simulink model "day11p2"  (R2026a)
settings: Solver=FixedStepAuto  StopTime=inf
InitFcn:
  | QueueLen = 200;
  | 
  | %{
  | fxp: udl vii hgb qmy
  | ixc: cje lra jhu
  | sgn: apv vbc
  | wua: knq
  | fnr: csd awl vvj fyx cvi xhb mvn guw wid vbp uvk krt oil izj zlh gwv
  | krt: grp cml vxt
  | hwj: laq jlg
  | rus: out
  | oag: wrc gpp
  | uos: zqg aiu gdx
  | xpu: qpb zqg gdx aiu
  | mdb: fnr mwu ozd
  | yrt: jlg ifs laq
  | eao: txi jmk xee sta knq
  | qcj: ivn mwb nrx lgx
  | wks: fyy lyd
  | xso: rqn flj fak
  | ucp: wpn mpy
  | zcf: knq sta xee jmk
  | sdr: vfy gsc wfb
  | ggn: brb ylm kdl rnk
  | tky: wcx ytk hbp xjh dne
  | kzl: sft sof utn
  | epc: uhn cqf xwv
  | srh: shh mei
  | uqe: sft
  | htw: hmf aia wsm
  | wid: qwo
  | daz: yvs
  | bdl: ipm kkp
  | xay: mpi
  | bsb: epc jpb cqs ixc cur ril ybr
  | mwb: out
  | cxr: yvs
  | ruf: jax uvl ctm
  | vtp: rbo
  | tqs: kdl pje ylm brb
  | thb: out
  | ljy: ael tqw
  | tkl: ssx yds
  | ozd: itv csd vvj fyx awl xhb mvn guw vbp hzn yft mfv izj oil uvk cui krt myo fqn gwv zlh
  | uhn: lzx dac iqf
  | zad: wvh tmc ece
  | qlf: gce sgn fni
  | kcf: dka pvw uzw
  | uat: bda mkd
  | aai: gtk gkf cuk qcj
  | mfv: cml
  | qlv: wdr sbi ihm nww jkx bud qxb
  | paz: kbq osk
  | rys: iwh
  | gdx: out
  | hco: cuk gkf
  | gte: wks fft
  | zrw: iur mei shh
  | izj: elj wrh vnz uss
  | lur: jpb zib zwl uzn epc nta cur cqs ybr tkl sle
  | hgu: jmk xee
  | okf: ypu gye qzd
  | mli: dir mzw
  | shh: rjp
  | nhj: ael tqw
  | pbm: fxp dfl
  | vnz: che
  | vim: bmu
  | puz: dcl ofd
  | zrg: ihy
  | scj: ysr knu
  | pjc: uvl jax bvs
  | tbn: uat lkd fdg
  | rcp: okf
  | min: out
  | poc: rta yvs rbo
  | kde: bcz
  | wct: bvs jax uvl
  | wvh: brg
  | wrh: frd kbe ihy
  | fak: jwl lzu dni
  | zaq: jlg ifs laq ppm
  | yun: kde kob qmz uxn
  | boa: yql brg fbt sgu
  | izk: czt
  | xyj: out
  | xhk: ril cur yun pmu nta epc uzn zwl rxn sle tkl puz ixc cqs nqo jpb zzk
  | yql: mjy cfo bpj vqp
  | dcl: nbq
  | ogv: utn sof pld
  | rtp: gpp gmb eka
  | nki: jmk xee knq
  | agn: jly alh ola zcf
  | vrp: hnw
  | lts: yql fbt sgu
  | myo: rhq kvi
  | jpb: dcl xuk
  | dju: vrt ozd fnr you mwu
  | hnw: hmf
  | rhq: ehc
  | dij: knq sta xee txi
  | awl: vxt
  | knu: bsb lur igu
  | dfo: pab
  | ewm: sgn fni gce
  | fed: osk
  | nwy: ppm laq qgn
  | wby: you mwu fnr ozd
  | dir: jmn gpu
  | mjy: wfb iyi vfy
  | fcj: zkn hgq szd
  | mzo: out
  | lzl: xhk
  | czt: xcu xvu
  | tyq: gsc wfb kjq iyi
  | tda: rbo
  | ltv: srf vim mli slg
  | iwh: qpo
  | hnn: bsb fpb lur
  | fan: sgu
  | vqp: zow rqn fak flj wke
  | ltm: pvm xmq
  | cyc: dfl fxp
  | kvi: gwp jnw
  | srd: ipm jrk
  | lkv: fnr vrt
  | shb: hxf thb rus
  | xuk: zxj
  | ifs: ryr gep wck lcp fwn gdh foj
  | ynz: uji
  | igh: sta jmk
  | fyx: krd
  | gkf: ivn mwb axi
  | bcz: ftm rdm wby lkv
  | qeg: jlg qgn ifs ppm
  | goq: icv
  | qmy: out
  | wxl: igh heh hvs
  | kbe: dzp ybw
  | hxf: out
  | tqw: rdn nac
  | bmu: jmn gkl xfg
  | cqf: lzx
  | phn: rbi fjm
  | ykt: sgu fbt brg
  | zqg: out
  | ain: mpj
  | esz: jmk txi
  | bpj: rqn zow flj wke fak
  | qaj: gtk gkf cuk qcj
  | kul: ckh
  | rss: dka nwy
  | gaq: ifs laq jlg
  | ehc: hco qaj qup
  | saf: mwu you fnr vrt
  | mub: bee
  | tns: lyd fyy bqw
  | ssx: utb nel thp hhu wbs
  | mwd: qeg gpo
  | lgx: out
  | lyr: ozd
  | knq: qlf tnt bhv aeo ljy dmr
  | php: sgu
  | qmz: fer bcz
  | oab: lup
  | sof: ikt
  | lte: ytk hbp xjh dne wcx
  | hvs: xee txi knq
  | bnw: yhu qhx
  | jnw: aai hco qup nxs
  | uge: bqw fyy
  | cml: sid txz qgh
  | sle: uwp jhu lra ltm
  | uoi: yql sgu
  | tcu: eao hgu
  | aaj: laq ppm
  | bqy: you
  | gye: qpo
  | csx: you mwu fnr vrt
  | uut: dne xjh wcx
  | tat: kul jxm dxd shb wtu
  | sbi: yvn mub
  | uss: suv ihy kbe
  | def: wrc eka gpp
  | rso: out
  | dmr: oab kbr jaa
  | jhu: xmq
  | qxb: mub sfu fhq yvn
  | nww: htw
  | szd: zfx
  | gpp: qvv min rso iey
  | sft: fzl hnn ikt
  | fwn: mei iur
  | giz: txi sta jmk
  | you: hzn izj oil krt wid awl vbp csd
  | yvs: fpb lur xhk bsb
  | mci: jrk ipm kkp
  | nqo: uwp jhu cje
  | alh: jmk xee sta txi
  | ejz: fjm rbi fim
  | jnd: wua esz
  | igu: nta pmu yun cur ril ybr rxn zwl uzn fnn cqs ixc puz sle zzk jpb nqo zib
  | yft: tky kcj
  | vxt: sid
  | dni: hvs heh mpi
  | jwy: wtu
  | ypu: yrt
  | rqn: lzu dni
  | yfw: bag puu yba
  | vgx: amv gte qwd hpw
  | hgb: out
  | gwp: nxs qaj
  | obo: fbt
  | yhu: xkn jai boa
  | phi: bqy ftm
  | cmi: xyj
  | mvn: ruf btp
  | utn: ikt
  | mkd: zcf giz alh
  | eff: zow rqn wke flj
  | dml: yql brg sgu fbt
  | ivn: out
  | fft: fyy lyd
  | vbp: vnz
  | cuk: ivn lgx axi nrx
  | brb: lts bcq xsx fan
  | ckh: out
  | cui: zrg elj wrh vnz uss
  | ybw: pxr
  | sfu: bee ynz
  | aov: gyl xyj
  | yxq: jsh smb qhx
  | hgq: xvu
  | yba: pab xbk bvq
  | ser: mzo vii hgb qmy
  | xfg: txi xee
  | iey: out
  | vhi: jaa kbr evt ndc
  | kcj: hbp
  | qmf: zfx
  | tum: sgu brg yql
  | sva: her yfw anr
  | ctm: cyc
  | sta: ewm izk bhv tnt vhi hkq ljy waa aeo ofz xhd fcj gwo qlf nhj
  | jai: fbt sgu
  | iyj: dka kez nwy
  | ofd: tlb
  | qff: rcp osk
  | wbs: fnr you mwu vrt ozd
  | ulj: hrd tcu uqb
  | uvk: vxt grp qgy
  | txz: irm jwy fmr
  | yco: out
  | hlo: fxp ser
  | gsc: ldf yqe ulj
  | vpo: zxj tlb
  | jgf: laq
  | hns: uoi tmc ece
  | cvi: gpt otp sva
  | cur: kob kde qmz
  | lre: ipm
  | ryr: wpn fdl
  | wrc: iey yco
  | ftq: fvb kbp scb oap cvl
  | qwd: tns wks uge
  | laq: ryr nhf srh zrw bvv xje gep phn ejz ucp vgx foj gdh tph
  | fyy: vin obo dml php tum
  | iyi: yqe ldf axk
  | wck: mei iur
  | lzu: mpi
  | btp: uvl ctm bvs jax
  | zib: jhu lra cje ltm uwp
  | dac: lyr csx saf rmg vns
  | pje: lts ykt bcq
  | awp: oap kbp
  | iqf: lyr vns
  | fac: qgn
  | iiu: lre
  | gmb: min rso
  | pxk: wsm
  | icv: jlg ifs laq
  | tnt: oab ndc kbr evt
  | guw: otp qwo
  | rjp: fbt sgu
  | iqh: srf vim mli slg
  | xje: mpy
  | cmt: amv gte
  | kob: bcz fer
  | fzl: igu fpb
  | bud: rss fxl
  | lup: fvb cvl
  | bpc: jsh smb yhu
  | jui: fnr mwu you vrt ozd
  | wmr: tmc uoi wvh
  | ulo: yql brg sgu
  | quz: hns avo euq zad
  | avo: wvh uoi tmc
  | wtu: rus thb hxf ckh
  | jsh: xkn ulo boa ahv
  | bbz: mwd imq
  | hpw: fft tns uge
  | nbq: gcg jui zqy
  | cel: fxp dfl
  | jrk: lsu nki wgx
  | qzd: acm yrt qpo
  | xcu: ain
  | qxl: lur igu bsb
  | pmu: xuk dcl ofd
  | ahv: fbt brg
  | gtk: lgx nrx
  | vrt: yft izj uvk cui mfv oil myo hzn gwv zlh fqn guw vbp wid xhb mvn csd itv cvi fyx awl
  | gcg: vrt
  | ppm: bvv zrw vis dcr wck ryr gdh tph ucp ejz uuh gep
  | nel: ozd fnr
  | udl: out
  | gkl: knq txi jmk xee
  | vvj: btp pjc wct
  | adp: cxr vtp daz poc
  | zxj: jui gcg zqy
  | dka: ifs laq qgn jlg
  | bhl: xpu uos
  | mzw: jmn xfg
  | ycr: qmf hgq szd czt
  | zfx: dbo ain scj
  | jax: pbm bxg cel cyc hlo
  | yqe: jnd uqb hrd
  | lyd: dml php vin obo
  | euq: uoi ece
  | hzn: wct
  | gwv: uut tky lte
  | wgx: sta xee knq
  | xhd: phh ael
  | axk: tcu uqb
  | ece: sgu fbt
  | waa: jaa
  | jaa: ftq lup awp
  | cje: xmq pvm
  | lln: bbz qff dkw paz htf fhv vrp jkx ihm bud jef eej
  | bvs: pbm cel
  | zow: xay wxl
  | pvm: fnr you vrt ozd
  | dbo: knu
  | vbc: pld
  | xpp: iwh qzd gye
  | gep: fdl
  | qqj: xhk bsb lur fpb
  | wpo: fdg
  | qgy: sid qgh
  | dne: oag def
  | oap: igu lur bsb xhk
  | bee: oxm uji tpb jgf
  | dxd: rus thb
  | mjp: jgf mkp
  | ytc: brg yql sgu fbt
  | zlh: krd kvi rhq
  | wcx: def oag rtp
  | svr: qlv lln qwc
  | ola: sta xee jmk txi
  | qwc: jkx ihm nww sbi bud fed jef eej bbz qff nfj paz fhv vrp wdr
  | gce: kzl ogv
  | uxn: phi bcz
  | vnd: fbt brg
  | xee: uni hkq ljy qlf aeo
  | zaz: cmi
  | gpt: yfw
  | dkm: gaq fac aaj zaq
  | kjq: sgy
  | oba: qgn jlg
  | slg: dir
  | fvb: xhk bsb igu lur
  | csd: gpt otp qwo
  | kkp: dij pbf
  | osk: xpp rys
  | hmf: pde luh dkm
  | uwn: lkd
  | crd: ikt hnn fzl
  | acm: jlg qgn laq
  | utb: fnr mwu you
  | lcp: rbi
  | mby: out
  | fbt: tbn iiu uxu sdr wyl uwn xao ltv wpo mjy xso
  | fhq: ynz mjp
  | qhx: ahv boa ulo jai
  | wpn: bpo
  | xbk: mby
  | axi: out
  | rbi: yxq bnw
  | dcr: fjm
  | nxs: gkf cuk qcj
  | rxn: uwp jhu lra ltm
  | kez: ifs
  | ikt: xhk bsb igu fpb
  | nhf: pje
  | lsu: xee sta jmk
  | ejp: oba aaj gaq
  | tph: rnk brb
  | bpo: wmr euq
  | ybr: uhn cqf
  | pde: gaq
  | kbp: xhk bsb
  | fhv: pxk htw
  | lkd: bda mkd agn bhh
  | fmr: shb wtu kul
  | ftm: ozd vrt
  | aeo: szd qmf hgq
  | dhu: ogv apv vbc kzl
  | irh: mpj ysr qxl
  | thp: you ozd vrt
  | bda: alh jly ola zcf giz
  | uzw: laq ifs qgn
  | scb: bsb
  | aeb: wbs hhu nel utb
  | vin: brg
  | rnk: fan
  | sid: jwy fmr irm
  | uxu: slg mli vim srf
  | anr: yba puu zaz
  | kbq: rys
  | jwl: igh
  | vis: amv hpw gte qwd
  | fer: lkv wby rdm bqy ftm
  | kwv: ola jly zcf
  | nac: lur
  | xvu: phc irh
  | luh: aaj zaq oba gaq
  | bcq: fbt sgu brg yql
  | puu: bvq xbk
  | mei: rjp ytc vnd
  | lyf: igu xhk bsb
  | tmc: fbt
  | suv: rzo dzp qig bhl
  | qwo: anr
  | uuh: iur
  | dfl: mzo vii
  | hrd: esz wua
  | eka: min rso qvv yco
  | qpb: out
  | zqy: you mwu
  | evt: lup
  | bxg: dfl fxp
  | uni: oab kbr evt jaa
  | uwp: xmq dju
  | rdm: ozd vrt you fnr
  | gwo: poc
  | dto: bsb xhk lur fpb
  | ofz: dhu fni sgn
  | fjm: bpc
  | wsm: pde luh ejp
  | tmb: amv qwd
  | kdl: bcq ykt lts
  | jxm: ckh hxf
  | dyl: euq avo wmr hns
  | pxr: zqg
  | xsx: yql brg
  | wdr: rss fxl kcf
  | frd: rzo qig dzp bhl
  | tlb: zqy mdb
  | yvn: ynz mjp
  | bvv: fim
  | xjh: oag def
  | jmk: vhi bhv tnt izk ewm adp nhj qlf gwo fcj xhd ofz aeo ycr ljy hkq
  | smb: ahv xkn ulo
  | hbp: def rtp
  | fdl: quz bpo
  | flj: xay wxl
  | mkp: qgn jlg
  | fdg: mkd agn bda kwv bhh
  | mpy: bpo quz dyl
  | fim: yxq bnw bpc
  | mwu: xhb yft myo cui gwv mvn fqn fyx vbp wid
  | yds: hhu nel
  | her: dfo yba puu bag
  | ipm: nki wgx lsu pbf
  | wfb: ulj axk ldf
  | bvq: xyj
  | hhu: ozd you fnr
  | vfy: ulj yqe ldf axk
  | pld: qqj fzl
  | zkn: xvu zfx xcu
  | rbo: fpb lur
  | zzk: yds aeb
  | rdn: bsb igu fpb
  | ril: qmz uxn kde kob
  | foj: fdl
  | xhb: krd kvi
  | htf: osk rcp
  | nrx: out
  | zwl: xwv uhn cqf
  | gyl: out
  | dkw: rcp osk
  | sgu: wyl iiu vqp bpj sdr tyq tbn cfo eff wpo xso xao ltv
  | pbf: sta
  | ytk: oag
  | irm: shb kul
  | brg: wpo iqh tyq tbn uwn
  | dzp: xpu uos
  | ufe: utb nel hhu
  | gpo: jlg
  | ihy: bhl rzo dzp qig
  | jlg: srh tqs bvv tmb dcr
  | qgh: jwy fmr tat irm
  | aiu: out
  | itv: grp qgy
  | cqs: yds ufe ssx
  | mpj: igu xhk
  | pvw: ppm laq
  | mpi: xee knq
  | pab: gyl
  | jef: rss kcf iyj
  | qig: pxr xpu
  | lra: pvm
  | che: rzo qig dzp ybw
  | xao: rqn fak wke
  | nta: vpo xuk
  | rta: lur igu bsb
  | qvv: out
  | fpb: puz cqs ixc fnn tkl nqo jpb zzk zib yun cur pmu nta ybr ril uzn zwl
  | imq: hwj qeg gpo
  | jkx: fhq mub sfu
  | ael: lzl dto
  | wyl: srd bdl mci
  | hkq: zkn czt
  | apv: utn crd sof pld
  | kbr: ftq
  | xwv: iqf lzx
  | cfo: lre bdl srd
  | ysr: fpb xhk bsb
  | aia: dkm ejp
  | ndc: awp lup ftq
  | bhh: ola
  | bhv: poc daz vtp tda cxr
  | uqb: hgu
  | xkn: yql
  | eej: imq
  | ihm: htw pxk
  | phh: rdn lyf nac
  | cvl: fpb igu lur xhk
  | rzo: uos
  | uzn: kde
  | jly: jmk sta xee knq
  | otp: her
  | vii: out
  | fni: ogv uqe kzl
  | phc: ysr
  | srf: bmu mzw
  | fnn: xwv
  | rmg: you
  | heh: knq jmk xee txi
  | elj: frd kbe che suv
  | fxl: dka kez pvw uzw
  | sgy: uqb
  | vns: vrt fnr
  | gdh: hpw
  | bag: pab aov xbk cmi
  | bqw: dml tum php
  | txi: aeo dmr adp waa nhj uni
  | krd: gwp
  | wke: dni wxl jwl
  | ldf: uqb tcu hrd
  | jmn: knq xee jmk
  | ylm: fan bcq lts
  | qpo: ppm laq qgn jlg
  | qgn: ucp ejz phn cmt lcp uuh xje tqs gep foj gdh tph nhf fwn dcr wck ryr bvv tmb zrw srh vis ggn
  | tpb: ifs laq
  | uvl: hlo cel bxg pbm
  | iur: rjp vnd ytc
  | oil: uut lte
  | oxm: ppm laq qgn jlg
  | grp: qgh sid
  | lzx: vns csx saf
  | uji: qgn jlg ppm laq
  | amv: wks uge tns
  | qup: qcj
  | xmq: mwu you
  | fqn: sva
  | gpu: sta xee jmk txi
  | nfj: mwd goq
  | %}
undefined symbols (not defined in the file): DiscIntNeverNeededParam
libraries: simulink x12
(part 1 of 4)
settings Model: PauseTimes=193  Creator=pete  LastModifiedBy=pete

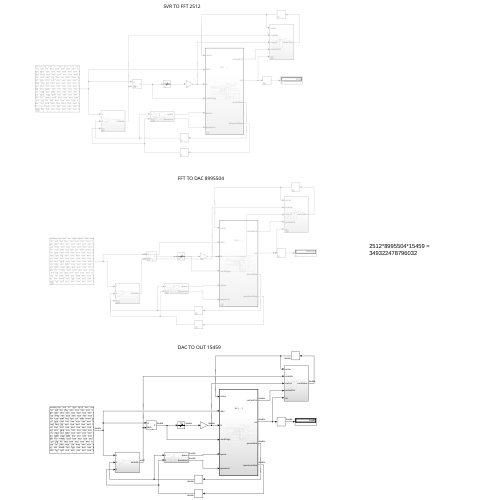
[thumbnail: Simulink's stored preview of the top-level diagram]
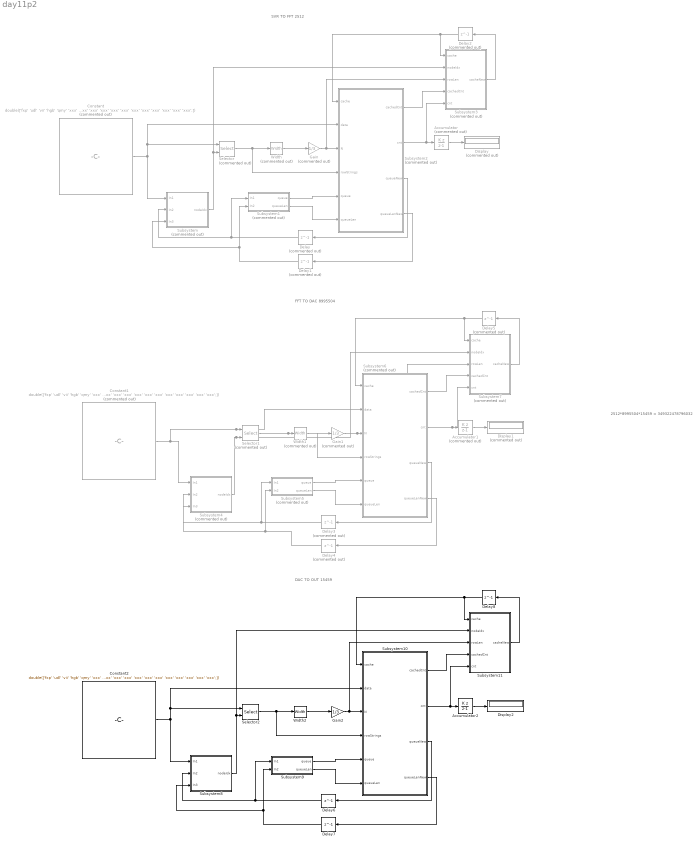
== system day11p2 ==
  note: 2512*8995504*15459 = 349322478796032
  note: SVR TO FFT 2512
  note: FFT TO DAC 8995504
  note: DAC TO OUT 15459
  Accumulator : DiscreteIntegrator  Commented=on  IntegratorMethod=Accumulation: Backward Euler  SampleTime=-1  OutDataTypeStr=double  ICPrevOutput=DiscIntNeverNeededParam  ICPrevScaledInput=DiscIntNeverNeededParam
  Accumulator1 : DiscreteIntegrator  Commented=on  IntegratorMethod=Accumulation: Backward Euler  SampleTime=-1  OutDataTypeStr=double  ICPrevOutput=DiscIntNeverNeededParam  ICPrevScaledInput=DiscIntNeverNeededParam
  Accumulator2 : DiscreteIntegrator  IntegratorMethod=Accumulation: Backward Euler  SampleTime=-1  OutDataTypeStr=double  ICPrevOutput=DiscIntNeverNeededParam  ICPrevScaledInput=DiscIntNeverNeededParam
  Constant : Constant  Commented=on  Value=|
      | double(['fxp' 'udl' 'vii' 'hgb' 'qmy' 'xxx' 'xxx' 'xxx' 'xxx' 'xxx' 'xxx' 'xxx' 'xxx' 'xxx' 'xxx' 'xxx' 'xxx' 'xxx' 'xxx' 'xxx' 'xxx' 'xxx' 'xxx' 'xxx';
      | 'ixc' 'cje' 'lra' 'jhu' 'xxx' 'xxx' 'xxx' 'xxx' 'xxx' 'xxx' 'xxx' 'xxx' 'xxx' 'xxx' 'xxx' 'xxx' 'xxx' 'xxx' 'xxx' 'xxx' 'xxx' 'xxx' 'xxx' 'xxx';
      | 'sgn' 'apv' 'vbc' 'xxx' 'xxx' 'xxx' 'xxx' 'xxx' 'xxx' 'xxx' 'xxx' 'xxx' 'xxx' 'xxx' 'xxx' 'xxx' 'xxx' 'xxx' 'xxx' 'xxx' 'xxx' 'xxx' 'xxx' 'xxx';
      | 'wua' 'knq' 'xxx' 'xxx' 'xxx' 'xxx' 'xxx' 'xxx' 'xxx' 'xxx' 'xxx' 'xxx' 'xxx' 'xxx' 'xxx' 'xxx' 'xxx' 'xxx' 'xxx' 'xxx' 'xxx' 'xxx' 'xxx' 'xxx';
      | 'fnr' 'csd' 'awl' 'vvj' 'fyx' 'cvi' 'xhb' 'mvn' 'guw' 'wid' 'vbp' 'uvk' 'krt' 'oil' 'izj' 'zlh' 'gwv' 'xxx' 'xxx' 'xxx' 'xxx' 'xxx' 'xxx' 'xxx';
      | 'krt' 'grp' 'cml' 'vxt' 'xxx' 'xxx' 'xxx' 'xxx' 'xxx' 'xxx' 'xxx' 'xxx' 'xxx' 'xxx' 'xxx' 'xxx' 'xxx' 'xxx' 'xxx' 'xxx' 'xxx' 'xxx' 'xxx' 'xxx';
      | 'hwj' 'laq' 'jlg' 'xxx' 'xxx' 'xxx' 'xxx' 'xxx' 'xxx' 'xxx' 'xxx' 'xxx' 'xxx' 'xxx' 'xxx' 'xxx' 'xxx' 'xxx' 'xxx' 'xxx' 'xxx' 'xxx' 'xxx' 'xxx';
      | 'rus' 'out' 'xxx' 'xxx' 'xxx' 'xxx' 'xxx' 'xxx' 'xxx' 'xxx' 'xxx' 'xxx' 'xxx' 'xxx' 'xxx' 'xxx' 'xxx' 'xxx' 'xxx' 'xxx' 'xxx' 'xxx' 'xxx' 'xxx';
      | 'oag' 'wrc' 'gpp' 'xxx' 'xxx' 'xxx' 'xxx' 'xxx' 'xxx' 'xxx' 'xxx' 'xxx' 'xxx' 'xxx' 'xxx' 'xxx' 'xxx' 'xxx' 'xxx' 'xxx' 'xxx' 'xxx' 'xxx' 'xxx';
      | 'uos' 'zqg' 'aiu' 'gdx' 'xxx' 'xxx' 'xxx' 'xxx' 'xxx' 'xxx' 'xxx' 'xxx' 'xxx' 'xxx' 'xxx' 'xxx' 'xxx' 'xxx' 'xxx' 'xxx' 'xxx' 'xxx' 'xxx' 'xxx';
      | 'xpu' 'qpb' 'zqg' 'gdx' 'aiu' 'xxx' 'xxx' 'xxx' 'xxx' 'xxx' 'xxx' 'xxx' 'xxx' 'xxx' 'xxx' 'xxx' 'xxx' 'xxx' 'xxx' 'xxx' 'xxx' 'xxx' 'xxx' 'xxx';
      | 'mdb' 'fnr' 'mwu' 'ozd' 'xxx' 'xxx' 'xxx' 'xxx' 'xxx' 'xxx' 'xxx' 'xxx' 'xxx' 'xxx' 'xxx' 'xxx' 'xxx' 'xxx' 'xxx' 'xxx' 'xxx' 'xxx' 'xxx' 'xxx';
      | 'yrt' 'jlg' 'ifs' 'laq' 'xxx' 'xxx' 'xxx' 'xxx' 'xxx' 'xxx' 'xxx' 'xxx' 'xxx' 'xxx' 'xxx' 'xxx' 'xxx' 'xxx' 'xxx' 'xxx' 'xxx' 'xxx' 'xxx' 'xxx';
      | 'eao' 'txi' 'jmk' 'xee' 'sta' 'knq' 'xxx' 'xxx' 'xxx' 'xxx' 'xxx' 'xxx' 'xxx' 'xxx' 'xxx' 'xxx' 'xxx' 'xxx' 'xxx' 'xxx' 'xxx' 'xxx' 'xxx' 'xxx';
      | 'qcj' 'ivn' 'mwb' 'nrx' 'lgx' 'xxx' 'xxx' 'xxx' 'xxx' 'xxx' 'xxx' 'xxx' 'xxx' 'xxx' 'xxx' 'xxx' 'xxx' 'xxx' 'xxx' 'xxx' 'xxx' 'xxx' 'xxx' 'xxx';
      | 'wks' 'fyy' 'lyd' 'xxx' 'xxx' 'xxx' 'xxx' 'xxx' 'xxx' 'xxx' 'xxx' 'xxx' 'xxx' 'xxx' 'xxx' 'xxx' 'xxx' 'xxx' 'xxx' 'xxx' 'xxx' 'xxx' 'xxx' 'xxx';
      | 'xso' 'rqn' 'flj' 'fak' 'xxx' 'xxx' 'xxx' 'xxx' 'xxx' 'xxx' 'xxx' 'xxx' 'xxx' 'xxx' 'xxx' 'xxx' 'xxx' 'xxx' 'xxx' 'xxx' 'xxx' 'xxx' 'xxx' 'xxx';
      | 'ucp' 'wpn' 'mpy' 'xxx' 'xxx' 'xxx' 'xxx' 'xxx' 'xxx' 'xxx' 'xxx' 'xxx' 'xxx' 'xxx' 'xxx' 'xxx' 'xxx' 'xxx' 'xxx' 'xxx' 'xxx' 'xxx' 'xxx' 'xxx';
      | 'zcf' 'knq' 'sta' 'xee' 'jmk' 'xxx' 'xxx' 'xxx' 'xxx' 'xxx' 'xxx' 'xxx' 'xxx' 'xxx' 'xxx' 'xxx' 'xxx' 'xxx' 'xxx' 'xxx' 'xxx' 'xxx' 'xxx' 'xxx';
      | 'sdr' 'vfy' 'gsc' 'wfb' 'xxx' 'xxx' 'xxx' 'xxx' 'xxx' 'xxx' 'xxx' 'xxx' 'xxx' 'xxx' 'xxx' 'xxx' 'xxx' 'xxx' 'xxx' 'xxx' 'xxx' 'xxx' 'xxx' 'xxx';
      | 'ggn' 'brb' 'ylm' 'kdl' 'rnk' 'xxx' 'xxx' 'xxx' 'xxx' 'xxx' 'xxx' 'xxx' 'xxx' 'xxx' 'xxx' 'xxx' 'xxx' 'xxx' 'xxx' 'xxx' 'xxx' 'xxx' 'xxx' 'xxx';
      | 'tky' 'wcx' 'ytk' 'hbp' 'xjh' 'dne' 'xxx' 'xxx' 'xxx' 'xxx' 'xxx' 'xxx' 'xxx' 'xxx' 'xxx' 'xxx' 'xxx' 'xxx' 'xxx' 'xxx' 'xxx' 'xxx' 'xxx' 'xxx';
      | 'kzl' 'sft' 'sof' 'utn' 'xxx' 'xxx' 'xxx' 'xxx' 'xxx' 'xxx' 'xxx' 'xxx' 'xxx' 'xxx' 'xxx' 'xxx' 'xxx' 'xxx' 'xxx' 'xxx' 'xxx' 'xxx' 'xxx' 'xxx';
      | 'epc' 'uhn' 'cqf' 'xwv' 'xxx' 'xxx' 'xxx' 'xxx' 'xxx' 'xxx' 'xxx' 'xxx' 'xxx' 'xxx' 'xxx' 'xxx' 'xxx' 'xxx' 'xxx' 'xxx' 'xxx' 'xxx' 'xxx' 'xxx';
      | 'srh' 'shh' 'mei' 'xxx' 'xxx' 'xxx' 'xxx' 'xxx' 'xxx' 'xxx' 'xxx' 'xxx' 'xxx' 'xxx' 'xxx' 'xxx' 'xxx' 'xxx' 'xxx' 'xxx' 'xxx' 'xxx' 'xxx' 'xxx';
      | 'uqe' 'sft' 'xxx' 'xxx' 'xxx' 'xxx' 'xxx' 'xxx' 'xxx' 'xxx' 'xxx' 'xxx' 'xxx' 'xxx' 'xxx' 'xxx' 'xxx' 'xxx' 'xxx' 'xxx' 'xxx' 'xxx' 'xxx' 'xxx';
      | 'htw' 'hmf' 'aia' 'wsm' 'xxx' 'xxx' 'xxx' 'xxx' 'xxx' 'xxx' 'xxx' 'xxx' 'xxx' 'xxx' 'xxx' 'xxx' 'xxx' 'xxx' 'xxx' 'xxx' 'xxx' 'xxx' 'xxx' 'xxx';
      | 'wid' 'qwo' 'xxx' 'xxx' 'xxx' 'xxx' 'xxx' 'xxx' 'xxx' 'xxx' 'xxx' 'xxx' 'xxx' 'xxx' 'xxx' 'xxx' 'xxx' 'xxx' 'xxx' 'xxx' 'xxx' 'xxx' 'xxx' 'xxx';
      | 'daz' 'yvs' 'xxx' 'xxx' 'xxx' 'xxx' 'xxx' 'xxx' 'xxx' 'xxx' 'xxx' 'xxx' 'xxx' 'xxx' 'xxx' 'xxx' 'xxx' 'xxx' 'xxx' 'xxx' 'xxx' 'xxx' 'xxx' 'xxx';
      | 'bdl' 'ipm' 'kkp' 'xxx' 'xxx' 'xxx' 'xxx' 'xxx' 'xxx' 'xxx' 'xxx' 'xxx' 'xxx' 'xxx' 'xxx' 'xxx' 'xxx' 'xxx' 'xxx' 'xxx' 'xxx' 'xxx' 'xxx' 'xxx';
      | 'xay' 'mpi' 'xxx' 'xxx' 'xxx' 'xxx' 'xxx' 'xxx' 'xxx' 'xxx' 'xxx' 'xxx' 'xxx' 'xxx' 'xxx' 'xxx' 'xxx' 'xxx' 'xxx' 'xxx' 'xxx' 'xxx' 'xxx' 'xxx';
      | 'bsb' 'epc' 'jpb' 'cqs' 'ixc' 'cur' 'ril' 'ybr' 'xxx' 'xxx' 'xxx' 'xxx' 'xxx' 'xxx' 'xxx' 'xxx' 'xxx' 'xxx' 'xxx' 'xxx' 'xxx' 'xxx' 'xxx' 'xxx';
      | 'mwb' 'out' 'xxx' 'xxx' 'xxx' 'xxx' 'xxx' 'xxx' 'xxx' 'xxx' 'xxx' 'xxx' 'xxx' 'xxx' 'xxx' 'xxx' 'xxx' 'xxx' 'xxx' 'xxx' 'xxx' 'xxx' 'xxx' 'xxx';
      | 'cxr' 'yvs' 'xxx' 'xxx' 'xxx' 'xxx' 'xxx' 'xxx' 'xxx' 'xxx' 'xxx' 'xxx' 'xxx' 'xxx' 'xxx' 'xxx' 'xxx' 'xxx' 'xxx' 'xxx' 'xxx' 'xxx' 'xxx' 'xxx';
      | 'ruf' 'jax' 'uvl' 'ctm' 'xxx' 'xxx' 'xxx' 'xxx' 'xxx' 'xxx' 'xxx' 'xxx' 'xxx' 'xxx' 'xxx' 'xxx' 'xxx' 'xxx' 'xxx' 'xxx' 'xxx' 'xxx' 'xxx' 'xxx';
      | 'vtp' 'rbo' 'xxx' 'xxx' 'xxx' 'xxx' 'xxx' 'xxx' 'xxx' 'xxx' 'xxx' 'xxx' 'xxx' 'xxx' 'xxx' 'xxx' 'xxx' 'xxx' 'xxx' 'xxx' 'xxx' 'xxx' 'xxx' 'xxx';
      | 'tqs' 'kdl' 'pje' 'ylm' 'brb' 'xxx' 'xxx' 'xxx' 'xxx' 'xxx' 'xxx' 'xxx' 'xxx' 'xxx' 'xxx' 'xxx' 'xxx' 'xxx' 'xxx' 'xxx' 'xxx' 'xxx' 'xxx' 'xxx';
      | 'thb' 'out' 'xxx' 'xxx' 'xxx' 'xxx' 'xxx' 'xxx' 'xxx' 'xxx' 'xxx' 'xxx' 'xxx' 'xxx' 'xxx' 'xxx' 'xxx' 'xxx' 'xxx' 'xxx' 'xxx' 'xxx' 'xxx' 'xxx';
      | 'ljy' 'ael' 'tqw' 'xxx' 'xxx' 'xxx' 'xxx' 'xxx' 'xxx' 'xxx' 'xxx' 'xxx' 'xxx' 'xxx' 'xxx' 'xxx' 'xxx' 'xxx' 'xxx' 'xxx' 'xxx' 'xxx' 'xxx' 'xxx';
      | 'tkl' 'ssx' 'yds' 'xxx' 'xxx' 'xxx' 'xxx' 'xxx' 'xxx' 'xxx' 'xxx' 'xxx' 'xxx' 'xxx' 'xxx' 'xxx' 'xxx' 'xxx' 'xxx' 'xxx' 'xxx' 'xxx' 'xxx' 'xxx';
      | 'ozd' 'itv' 'csd' 'vvj' 'fyx' 'awl' 'xhb' 'mvn' 'guw' 'vbp' 'hzn' 'yft' 'mfv' 'izj' 'oil' 'uvk' 'cui' 'krt' 'myo' 'fqn' 'gwv' 'zlh' 'xxx' 'xxx';
      | 'uhn' 'lzx' 'dac' 'iqf' 'xxx' 'xxx' 'xxx' 'xxx' 'xxx' 'xxx' 'xxx' 'xxx' 'xxx' 'xxx' 'xxx' 'xxx' 'xxx' 'xxx' 'xxx' 'xxx' 'xxx' 'xxx' 'xxx' 'xxx';
      | 'zad' 'wvh' 'tmc' 'ece' 'xxx' 'xxx' 'xxx' 'xxx' 'xxx' 'xxx' 'xxx' 'xxx' 'xxx' 'xxx' 'xxx' 'xxx' 'xxx' 'xxx' 'xxx' 'xxx' 'xxx' 'xxx' 'xxx' 'xxx';
      | 'qlf' 'gce' 'sgn' 'fni' 'xxx' 'xxx' 'xxx' 'xxx' 'xxx' 'xxx' 'xxx' 'xxx' 'xxx' 'xxx' 'xxx' 'xxx' 'xxx' 'xxx' 'xxx' 'xxx' 'xxx' 'xxx' 'xxx' 'xxx';
      | 'kcf' 'dka' 'pvw' 'uzw' 'xxx' 'xxx' 'xxx' 'xxx' 'xxx' 'xxx' 'xxx' 'xxx' 'xxx' 'xxx' 'xxx' 'xxx' 'xxx' 'xxx' 'xxx' 'xxx' 'xxx' 'xxx' 'xxx' 'xxx';
      | 'uat' 'bda' 'mkd' 'xxx' 'xxx' 'xxx' 'xxx' 'xxx' 'xxx' 'xxx' 'xxx' 'xxx' 'xxx' 'xxx' 'xxx' 'xxx' 'xxx' 'xxx' 'xxx' 'xxx' 'xxx' 'xxx' 'xxx' 'xxx';
      | 'aai' 'gtk' 'gkf' 'cuk' 'qcj' 'xxx' 'xxx' 'xxx' 'xxx' 'xxx' 'xxx' 'xxx' 'xxx' 'xxx' 'xxx' 'xxx' 'xxx' 'xxx' 'xxx' 'xxx' 'xxx' 'xxx' 'xxx' 'xxx';
      | 'mfv' 'cml' 'xxx' 'xxx' 'xxx' 'xxx' 'xxx' 'xxx' 'xxx' 'xxx' 'xxx' 'xxx' 'xxx' 'xxx' 'xxx' 'xxx' 'xxx' 'xxx' 'xxx' 'xxx' 'xxx' 'xxx' 'xxx' 'xxx';
      | 'qlv' 'wdr' 'sbi' 'ihm' 'nww' 'jkx' 'bud' 'qxb' 'xxx' 'xxx' 'xxx' 'xxx' 'xxx' 'xxx' 'xxx' 'xxx' 'xxx' 'xxx' 'xxx' 'xxx' 'xxx' 'xxx' 'xxx' 'xxx';
      | 'paz' 'kbq' 'osk' 'xxx' 'xxx' 'xxx' 'xxx' 'xxx' 'xxx' 'xxx' 'xxx' 'xxx' 'xxx' 'xxx' 'xxx' 'xxx' 'xxx' 'xxx' 'xxx' 'xxx' 'xxx' 'xxx' 'xxx' 'xxx';
      | 'rys' 'iwh' 'xxx' 'xxx' 'xxx' 'xxx' 'xxx' 'xxx' 'xxx' 'xxx' 'xxx' 'xxx' 'xxx' 'xxx' 'xxx' 'xxx' 'xxx' 'xxx' 'xxx' 'xxx' 'xxx' 'xxx' 'xxx' 'xxx';
      | 'gdx' 'out' 'xxx' 'xxx' 'xxx' 'xxx' 'xxx' 'xxx' 'xxx' 'xxx' 'xxx' 'xxx' 'xxx' 'xxx' 'xxx' 'xxx' 'xxx' 'xxx' 'xxx' 'xxx' 'xxx' 'xxx' 'xxx' 'xxx';
      | 'hco' 'cuk' 'gkf' 'xxx' 'xxx' 'xxx' 'xxx' 'xxx' 'xxx' 'xxx' 'xxx' 'xxx' 'xxx' 'xxx' 'xxx' 'xxx' 'xxx' 'xxx' 'xxx' 'xxx' 'xxx' 'xxx' 'xxx' 'xxx';
      | 'gte' 'wks' 'fft' 'xxx' 'xxx' 'xxx' 'xxx' 'xxx' 'xxx' 'xxx' 'xxx' 'xxx' 'xxx' 'xxx' 'xxx' 'xxx' 'xxx' 'xxx' 'xxx' 'xxx' 'xxx' 'xxx' 'xxx' 'xxx';
      | 'zrw' 'iur' 'mei' 'shh' 'xxx' 'xxx' 'xxx' 'xxx' 'xxx' 'xxx' 'xxx' 'xxx' 'xxx' 'xxx' 'xxx' 'xxx' 'xxx' 'xxx' 'xxx' 'xxx' 'xxx' 'xxx' 'xxx' 'xxx';
      | 'izj' 'elj' 'wrh' 'vnz' 'uss' 'xxx' 'xxx' 'xxx' 'xxx' 'xxx' 'xxx' 'xxx' 'xxx' 'xxx' 'xxx' 'xxx' 'xxx' 'xxx' 'xxx' 'xxx' 'xxx' 'xxx' 'xxx' 'xxx';
      | 'lur' 'jpb' 'zib' 'zwl' 'uzn' 'epc' 'nta' 'cur' 'cqs' 'ybr' 'tkl' 'sle' 'xxx' 'xxx' 'xxx' 'xxx' 'xxx' 'xxx' 'xxx' 'xxx' 'xxx' 'xxx' 'xxx' 'xxx';
      | 'hgu' 'jmk' 'xee' 'xxx' 'xxx' 'xxx' 'xxx' 'xxx' 'xxx' 'xxx' 'xxx' 'xxx' 'xxx' 'xxx' 'xxx' 'xxx' 'xxx' 'xxx' 'xxx' 'xxx' 'xxx' 'xxx' 'xxx' 'xxx';
      | 'okf' 'ypu' 'gye' 'qzd' 'xxx' 'xxx' 'xxx' 'xxx' 'xxx' 'xxx' 'xxx' 'xxx' 'xxx' 'xxx' 'xxx' 'xxx' 'xxx' 'xxx' 'xxx' 'xxx' 'xxx' 'xxx' 'xxx' 'xxx';
      | 'mli' 'dir' 'mzw' 'xxx' 'xxx' 'xxx' 'xxx' 'xxx' 'xxx' 'xxx' 'xxx' 'xxx' 'xxx' 'xxx' 'xxx' 'xxx' 'xxx' 'xxx' 'xxx' 'xxx' 'xxx' 'xxx' 'xxx' 'xxx';
      | 'shh' 'rjp' 'xxx' 'xxx' 'xxx' 'xxx' 'xxx' 'xxx' 'xxx' 'xxx' 'xxx' 'xxx' 'xxx' 'xxx' 'xxx' 'xxx' 'xxx' 'xxx' 'xxx' 'xxx' 'xxx' 'xxx' 'xxx' 'xxx';
      | 'nhj' 'ael' 'tqw' 'xxx' 'xxx' 'xxx' 'xxx' 'xxx' 'xxx' 'xxx' 'xxx' 'xxx' 'xxx' 'xxx' 'xxx' 'xxx' 'xxx' 'xxx' 'xxx' 'xxx' 'xxx' 'xxx' 'xxx' 'xxx';
      | 'pbm' 'fxp' 'dfl' 'xxx' 'xxx' 'xxx' 'xxx' 'xxx' 'xxx' 'xxx' 'xxx' 'xxx' 'xxx' 'xxx' 'xxx' 'xxx' 'xxx' 'xxx' 'xxx' 'xxx' 'xxx' 'xxx' 'xxx' 'xxx';
      | 'vnz' 'che' 'xxx' 'xxx' 'xxx' 'xxx' 'xxx' 'xxx' 'xxx' 'xxx' 'xxx' 'xxx' 'xxx' 'xxx' 'xxx' 'xxx' 'xxx' 'xxx' 'xxx' 'xxx' 'xxx' 'xxx' 'xxx' 'xxx';
      | 'vim' 'bmu' 'xxx' 'xxx' 'xxx' 'xxx' 'xxx' 'xxx' 'xxx' 'xxx' 'xxx' 'xxx' 'xxx' 'xxx' 'xxx' 'xxx' 'xxx' 'xxx' 'xxx' 'xxx' 'xxx' 'xxx' 'xxx' 'xxx';
      | 'puz' 'dcl' 'ofd' 'xxx' 'xxx' 'xxx' 'xxx' 'xxx' 'xxx' 'xxx' 'xxx' 'xxx' 'xxx' 'xxx' 'xxx' 'xxx' 'xxx' 'xxx' 'xxx' 'xxx' 'xxx' 'xxx' 'xxx' 'xxx';
      | 'zrg' 'ihy' 'xxx' 'xxx' 'xxx' 'xxx' 'xxx' 'xxx' 'xxx' 'xxx' 'xxx' 'xxx' 'xxx' 'xxx' 'xxx' 'xxx' 'xxx' 'xxx' 'xxx' 'xxx' 'xxx' 'xxx' 'xxx' 'xxx';
      | 'scj' 'ysr' 'knu' 'xxx' 'xxx' 'xxx' 'xxx' 'xxx' 'xxx' 'xxx' 'xxx' 'xxx' 'xxx' 'xxx' 'xxx' 'xxx' 'xxx' 'xxx' 'xxx' 'xxx' 'xxx' 'xxx' 'xxx' 'xxx';
      | 'pjc' 'uvl' 'jax' 'bvs' 'xxx' 'xxx' 'xxx' 'xxx' 'xxx' 'xxx' 'xxx' 'xxx' 'xxx' 'xxx' 'xxx' 'xxx' 'xxx' 'xxx' 'xxx' 'xxx' 'xxx' 'xxx' 'xxx' 'xxx';
      | 'tbn' 'uat' 'lkd' 'fdg' 'xxx' 'xxx' 'xxx' 'xxx' 'xxx' 'xxx' 'xxx' 'xxx' 'xxx' 'xxx' 'xxx' 'xxx' 'xxx' 'xxx' 'xxx' 'xxx' 'xxx' 'xxx' 'xxx' 'xxx';
      | 'rcp' 'okf' 'xxx' 'xxx' 'xxx' 'xxx' 'xxx' 'xxx' 'xxx' 'xxx' 'xxx' 'xxx' 'xxx' 'xxx' 'xxx' 'xxx' 'xxx' 'xxx' 'xxx' 'xxx' 'xxx' 'xxx' 'xxx' 'xxx';
      | 'min' 'out' 'xxx' 'xxx' 'xxx' 'xxx' 'xxx' 'xxx' 'xxx' 'xxx' 'xxx' 'xxx' 'xxx' 'xxx' 'xxx' 'xxx' 'xxx' 'xxx' 'xxx' 'xxx' 'xxx' 'xxx' 'xxx' 'xxx';
      | 'poc' 'rta' 'yvs' 'rbo' 'xxx' 'xxx' 'xxx' 'xxx' 'xxx' 'xxx' 'xxx' 'xxx' 'xxx' 'xxx' 'xxx' 'xxx' 'xxx' 'xxx' 'xxx' 'xxx' 'xxx' 'xxx' 'xxx' 'xxx';
      | 'kde' 'bcz' 'xxx' 'xxx' 'xxx' 'xxx' 'xxx' 'xxx' 'xxx' 'xxx' 'xxx' 'xxx' 'xxx' 'xxx' 'xxx' 'xxx' 'xxx' 'xxx' 'xxx' 'xxx' 'xxx' 'xxx' 'xxx' 'xxx';
      | 'wct' 'bvs' 'jax' 'uvl' 'xxx' 'xxx' 'xxx' 'xxx' 'xxx' 'xxx' 'xxx' 'xxx' 'xxx' 'xxx' 'xxx' 'xxx' 'xxx' 'xxx' 'xxx' 'xxx' 'xxx' 'xxx' 'xxx' 'xxx';
      | 'wvh' 'brg' 'xxx' 'xxx' 'xxx' 'xxx' 'xxx' 'xxx' 'xxx' 'xxx' 'xxx' 'xxx' 'xxx' 'xxx' 'xxx' 'xxx' 'xxx' 'xxx' 'xxx' 'xxx' 'xxx' 'xxx' 'xxx' 'xxx';
      | 'wrh' 'frd' 'kbe' 'ihy' 'xxx' 'xxx' 'xxx' 'xxx' 'xxx' 'xxx' 'xxx' 'xxx' 'xxx' 'xxx' 'xxx' 'xxx' 'xxx' 'xxx' 'xxx' 'xxx' 'xxx' 'xxx' 'xxx' 'xxx';
      | 'fak' 'jwl' 'lzu' 'dni' 'xxx' 'xxx' 'xxx' 'xxx' 'xxx' 'xxx' 'xxx' 'xxx' 'xxx' 'xxx' 'xxx' 'xxx' 'xxx' 'xxx' 'xxx' 'xxx' 'xxx' 'xxx' 'xxx' 'xxx';
      | 'zaq' 'jlg' 'ifs' 'laq' 'ppm' 'xxx' 'xxx' 'xxx' 'xxx' 'xxx' 'xxx' 'xxx' 'xxx' 'xxx' 'xxx' 'xxx' 'xxx' 'xxx' 'xxx' 'xxx' 'xxx' 'xxx' 'xxx' 'xxx';
      | 'yun' 'kde' 'kob' 'qmz' 'uxn' 'xxx' 'xxx' 'xxx' 'xxx' 'xxx' 'xxx' 'xxx' 'xxx' 'xxx' 'xxx' 'xxx' 'xxx' 'xxx' 'xxx' 'xxx' 'xxx' 'xxx' 'xxx' 'xxx';
      | 'boa' 'yql' 'brg' 'fbt' 'sgu' 'xxx' 'xxx' 'xxx' 'xxx' 'xxx' 'xxx' 'xxx' 'xxx' 'xxx' 'xxx' 'xxx' 'xxx' 'xxx' 'xxx' 'xxx' 'xxx' 'xxx' 'xxx' 'xxx';
      | 'izk' 'czt' 'xxx' 'xxx' 'xxx' 'xxx' 'xxx' 'xxx' 'xxx' 'xxx' 'xxx' 'xxx' 'xxx' 'xxx' 'xxx' 'xxx' 'xxx' 'xxx' 'xxx' 'xxx' 'xxx' 'xxx' 'xxx' 'xxx';
      | 'xyj' 'out' 'xxx' 'xxx' 'xxx' 'xxx' 'xxx' 'xxx' 'xxx' 'xxx' 'xxx' 'xxx' 'xxx' 'xxx' 'xxx' 'xxx' 'xxx' 'xxx' 'xxx' 'xxx' 'xxx' 'xxx' 'xxx' 'xxx';
      | 'xhk' 'ril' 'cur' 'yun' 'pmu' 'nta' 'epc' 'uzn' 'zwl' 'rxn' 'sle' 'tkl' 'puz' 'ixc' 'cqs' 'nqo' 'jpb' 'zzk' 'xxx' 'xxx' 'xxx' 'xxx' 'xxx' 'xxx';
      | 'yql' 'mjy' 'cfo' 'bpj' 'vqp' 'xxx' 'xxx' 'xxx' 'xxx' 'xxx' 'xxx' 'xxx' 'xxx' 'xxx' 'xxx' 'xxx' 'xxx' 'xxx' 'xxx' 'xxx' 'xxx' 'xxx' 'xxx' 'xxx';
      | 'dcl' 'nbq' 'xxx' 'xxx' 'xxx' 'xxx' 'xxx' 'xxx' 'xxx' 'xxx' 'xxx' 'xxx' 'xxx' 'xxx' 'xxx' 'xxx' 'xxx' 'xxx' 'xxx' 'xxx' 'xxx' 'xxx' 'xxx' 'xxx';
      | 'ogv' 'utn' 'sof' 'pld' 'xxx' 'xxx' 'xxx' 'xxx' 'xxx' 'xxx' 'xxx' 'xxx' 'xxx' 'xxx' 'xxx' 'xxx' 'xxx' 'xxx' 'xxx' 'xxx' 'xxx' 'xxx' 'xxx' 'xxx';
      | 'rtp' 'gpp' 'gmb' 'eka' 'xxx' 'xxx' 'xxx' 'xxx' 'xxx' 'xxx' 'xxx' 'xxx' 'xxx' 'xxx' 'xxx' 'xxx' 'xxx' 'xxx' 'xxx' 'xxx' 'xxx' 'xxx' 'xxx' 'xxx';
      | 'nki' 'jmk' 'xee' 'knq' 'xxx' 'xxx' 'xxx' 'xxx' 'xxx' 'xxx' 'xxx' 'xxx' 'xxx' 'xxx' 'xxx' 'xxx' 'xxx' 'xxx' 'xxx' 'xxx' 'xxx' 'xxx' 'xxx' 'xxx';
      | 'agn' 'jly' 'alh' 'ola' 'zcf' 'xxx' 'xxx' 'xxx' 'xxx' 'xxx' 'xxx' 'xxx' 'xxx' 'xxx' 'xxx' 'xxx' 'xxx' 'xxx' 'xxx' 'xxx' 'xxx' 'xxx' 'xxx' 'xxx';
      | 'vrp' 'hnw' 'xxx' 'xxx' 'xxx' 'xxx' 'xxx' 'xxx' 'xxx' 'xxx' 'xxx' 'xxx' 'xxx' 'xxx' 'xxx' 'xxx' 'xxx' 'xxx' 'xxx' 'xxx' 'xxx' 'xxx' 'xxx' 'xxx';
      | 'lts' 'yql' 'fbt' 'sgu' 'xxx' 'xxx' 'xxx' 'xxx' 'xxx' 'xxx' 'xxx' 'xxx' 'xxx' 'xxx' 'xxx' 'xxx' 'xxx' 'xxx' 'xxx' 'xxx' 'xxx' 'xxx' 'xxx' 'xxx';
      | 'myo' 'rhq' 'kvi' 'xxx' 'xxx' 'xxx' 'xxx' 'xxx' 'xxx' 'xxx' 'xxx' 'xxx' 'xxx' 'xxx' 'xxx' 'xxx' 'xxx' 'xxx' 'xxx' 'xxx' 'xxx' 'xxx' 'xxx' 'xxx';
      | 'jpb' 'dcl' 'xuk' 'xxx' 'xxx' 'xxx' 'xxx' 'xxx' 'xxx' 'xxx' 'xxx' 'xxx' 'xxx' 'xxx' 'xxx' 'xxx' 'xxx' 'xxx' 'xxx' 'xxx' 'xxx' 'xxx' 'xxx' 'xxx';
      | 'dju' 'vrt' 'ozd' 'fnr' 'you' 'mwu' 'xxx' 'xxx' 'xxx' 'xxx' 'xxx' 'xxx' 'xxx' 'xxx' 'xxx' 'xxx' 'xxx' 'xxx' 'xxx' 'xxx' 'xxx' 'xxx' 'xxx' 'xxx';
      | 'hnw' 'hmf' 'xxx' 'xxx' 'xxx' 'xxx' 'xxx' 'xxx' 'xxx' 'xxx' 'xxx' 'xxx' 'xxx' 'xxx' 'xxx' 'xxx' 'xxx' 'xxx' 'xxx' 'xxx' 'xxx' 'xxx' 'xxx' 'xxx';
      | 'rhq' 'ehc' 'xxx' 'xxx' 'xxx' 'xxx' 'xxx' 'xxx' 'xxx' 'xxx' 'xxx' 'xxx' 'xxx' 'xxx' 'xxx' 'xxx' 'xxx' 'xxx' 'xxx' 'xxx' 'xxx' 'xxx' 'xxx' 'xxx';
      | 'dij' 'knq' 'sta' 'xee' 'txi' 'xxx' 'xxx' 'xxx' 'xxx' 'xxx' 'xxx' 'xxx' 'xxx' 'xxx' 'xxx' 'xxx' 'xxx' 'xxx' 'xxx' 'xxx' 'xxx' 'xxx' 'xxx' 'xxx';
      | 'awl' 'vxt' 'xxx' 'xxx' 'xxx' 'xxx' 'xxx' 'xxx' 'xxx' 'xxx' 'xxx' 'xxx' 'xxx' 'xxx' 'xxx' 'xxx' 'xxx' 'xxx' 'xxx' 'xxx' 'xxx' 'xxx' 'xxx' 'xxx';
      | 'knu' 'bsb' 'lur' 'igu' 'xxx' 'xxx' 'xxx' 'xxx' 'xxx' 'xxx' 'xxx' 'xxx' 'xxx' 'xxx' 'xxx' 'xxx' 'xxx' 'xxx' 'xxx' 'xxx' 'xxx' 'xxx' 'xxx' 'xxx';
      | 'dfo' 'pab' 'xxx' 'xxx' 'xxx' 'xxx' 'xxx' 'xxx' 'xxx' 'xxx' 'xxx' 'xxx' 'xxx' 'xxx' 'xxx' 'xxx' 'xxx' 'xxx' 'xxx' 'xxx' 'xxx' 'xxx' 'xxx' 'xxx';
      | 'ewm' 'sgn' 'fni' 'gce' 'xxx' 'xxx' 'xxx' 'xxx' 'xxx' 'xxx' 'xxx' 'xxx' 'xxx' 'xxx' 'xxx' 'xxx' 'xxx' 'xxx' 'xxx' 'xxx' 'xxx' 'xxx' 'xxx' 'xxx';
      | 'fed' 'osk' 'xxx' 'xxx' 'xxx' 'xxx' 'xxx' 'xxx' 'xxx' 'xxx' 'xxx' 'xxx' 'xxx' 'xxx' 'xxx' 'xxx' 'xxx' 'xxx' 'xxx' 'xxx' 'xxx' 'xxx' 'xxx' 'xxx';
      | 'nwy' 'ppm' 'laq' 'qgn' 'xxx' 'xxx' 'xxx' 'xxx' 'xxx' 'xxx' 'xxx' 'xxx' 'xxx' 'xxx' 'xxx' 'xxx' 'xxx' 'xxx' 'xxx' 'xxx' 'xxx' 'xxx' 'xxx' 'xxx';
      | 'wby' 'you' 'mwu' 'fnr' 'ozd' 'xxx' 'xxx' 'xxx' 'xxx' 'xxx' 'xxx' 'xxx' 'xxx' 'xxx' 'xxx' 'xxx' 'xxx' 'xxx' 'xxx' 'xxx' 'xxx' 'xxx' 'xxx' 'xxx';
      | 'dir' 'jmn' 'gpu' 'xxx' 'xxx' 'xxx' 'xxx' 'xxx' 'xxx' 'xxx' 'xxx' 'xxx' 'xxx' 'xxx' 'xxx' 'xxx' 'xxx' 'xxx' 'xxx' 'xxx' 'xxx' 'xxx' 'xxx' 'xxx';
      | 'mjy' 'wfb' 'iyi' 'vfy' 'xxx' 'xxx' 'xxx' 'xxx' 'xxx' 'xxx' 'xxx' 'xxx' 'xxx' 'xxx' 'xxx' 'xxx' 'xxx' 'xxx' 'xxx' 'xxx' 'xxx' 'xxx' 'xxx' 'xxx';
      | 'fcj' 'zkn' 'hgq' 'szd' 'xxx' 'xxx' 'xxx' 'xxx' 'xxx' 'xxx' 'xxx' 'xxx' 'xxx' 'xxx' 'xxx' 'xxx' 'xxx' 'xxx' 'xxx' 'xxx' 'xxx' 'xxx' 'xxx' 'xxx';
      | 'mzo' 'out' 'xxx' 'xxx' 'xxx' 'xxx' 'xxx' 'xxx' 'xxx' 'xxx' 'xxx' 'xxx' 'xxx' 'xxx' 'xxx' 'xxx' 'xxx' 'xxx' 'xxx' 'xxx' 'xxx' 'xxx' 'xxx' 'xxx';
      | 'lzl' 'xhk' 'xxx' 'xxx' 'xxx' 'xxx' 'xxx' 'xxx' 'xxx' 'xxx' 'xxx' 'xxx' 'xxx' 'xxx' 'xxx' 'xxx' 'xxx' 'xxx' 'xxx' 'xxx' 'xxx' 'xxx' 'xxx' 'xxx';
      | 'czt' 'xcu' 'xvu' 'xxx' 'xxx' 'xxx' 'xxx' 'xxx' 'xxx' 'xxx' 'xxx' 'xxx' 'xxx' 'xxx' 'xxx' 'xxx' 'xxx' 'xxx' 'xxx' 'xxx' 'xxx' 'xxx' 'xxx' 'xxx';
      | 'tyq' 'gsc' 'wfb' 'kjq' 'iyi' 'xxx' 'xxx' 'xxx' 'xxx' 'xxx' 'xxx' 'xxx' 'xxx' 'xxx' 'xxx' 'xxx' 'xxx' 'xxx' 'xxx' 'xxx' 'xxx' 'xxx' 'xxx' 'xxx';
      | 'tda' 'rbo' 'xxx' 'xxx' 'xxx' 'xxx' 'xxx' 'xxx' 'xxx' 'xxx' 'xxx' 'xxx' 'xxx' 'xxx' 'xxx' 'xxx' 'xxx' 'xxx' 'xxx' 'xxx' 'xxx' 'xxx' 'xxx' 'xxx';
      | 'ltv' 'srf' 'vim' 'mli' 'slg' 'xxx' 'xxx' 'xxx' 'xxx' 'xxx' 'xxx' 'xxx' 'xxx' 'xxx' 'xxx' 'xxx' 'xxx' 'xxx' 'xxx' 'xxx' 'xxx' 'xxx' 'xxx' 'xxx';
      | 'iwh' 'qpo' 'xxx' 'xxx' 'xxx' 'xxx' 'xxx' 'xxx' 'xxx' 'xxx' 'xxx' 'xxx' 'xxx' 'xxx' 'xxx' 'xxx' 'xxx' 'xxx' 'xxx' 'xxx' 'xxx' 'xxx' 'xxx' 'xxx';
      | 'hnn' 'bsb' 'fpb' 'lur' 'xxx' 'xxx' 'xxx' 'xxx' 'xxx' 'xxx' 'xxx' 'xxx' 'xxx' 'xxx' 'xxx' 'xxx' 'xxx' 'xxx' 'xxx' 'xxx' 'xxx' 'xxx' 'xxx' 'xxx';
      | 'fan' 'sgu' 'xxx' 'xxx' 'xxx' 'xxx' 'xxx' 'xxx' 'xxx' 'xxx' 'xxx' 'xxx' 'xxx' 'xxx' 'xxx' 'xxx' 'xxx' 'xxx' 'xxx' 'xxx' 'xxx' 'xxx' 'xxx' 'xxx';
      | 'vqp' 'zow' 'rqn' 'fak' 'flj' 'wke' 'xxx' 'xxx' 'xxx' 'xxx' 'xxx' 'xxx' 'xxx' 'xxx' 'xxx' 'xxx' 'xxx' 'xxx' 'xxx' 'xxx' 'xxx' 'xxx' 'xxx' 'xxx';
      | 'ltm' 'pvm' 'xmq' 'xxx' 'xxx' 'xxx' 'xxx' 'xxx' 'xxx' 'xxx' 'xxx' 'xxx' 'xxx' 'xxx' 'xxx' 'xxx' 'xxx' 'xxx' 'xxx' 'xxx' 'xxx' 'xxx' 'xxx' 'xxx';
      | 'cyc' 'dfl' 'fxp' 'xxx' 'xxx' 'xxx' 'xxx' 'xxx' 'xxx' 'xxx' 'xxx' 'xxx' 'xxx' 'xxx' 'xxx' 'xxx' 'xxx' 'xxx' 'xxx' 'xxx' 'xxx' 'xxx' 'xxx' 'xxx';
      | 'kvi' 'gwp' 'jnw' 'xxx' 'xxx' 'xxx' 'xxx' 'xxx' 'xxx' 'xxx' 'xxx' 'xxx' 'xxx' 'xxx' 'xxx' 'xxx' 'xxx' 'xxx' 'xxx' 'xxx' 'xxx' 'xxx' 'xxx' 'xxx';
      | 'srd' 'ipm' 'jrk' 'xxx' 'xxx' 'xxx' 'xxx' 'xxx' 'xxx' 'xxx' 'xxx' 'xxx' 'xxx' 'xxx' 'xxx' 'xxx' 'xxx' 'xxx' 'xxx' 'xxx' 'xxx' 'xxx' 'xxx' 'xxx';
      | 'lkv' 'fnr' 'vrt' 'xxx' 'xxx' 'xxx' 'xxx' 'xxx' 'xxx' 'xxx' 'xxx' 'xxx' 'xxx' 'xxx' 'xxx' 'xxx' 'xxx' 'xxx' 'xxx' 'xxx' 'xxx' 'xxx' 'xxx' 'xxx';
      | 'shb' 'hxf' 'thb' 'rus' 'xxx' 'xxx' 'xxx' 'xxx' 'xxx' 'xxx' 'xxx' 'xxx' 'xxx' 'xxx' 'xxx' 'xxx' 'xxx' 'xxx' 'xxx' 'xxx' 'xxx' 'xxx' 'xxx' 'xxx';
      | 'xuk' 'zxj' 'xxx' 'xxx' 'xxx' 'xxx' 'xxx' 'xxx' 'xxx' 'xxx' 'xxx' 'xxx' 'xxx' 'xxx' 'xxx' 'xxx' 'xxx' 'xxx' 'xxx' 'xxx' 'xxx' 'xxx' 'xxx' 'xxx';
      | 'ifs' 'ryr' 'gep' 'wck' 'lcp' 'fwn' 'gdh' 'foj' 'xxx' 'xxx' 'xxx' 'xxx' 'xxx' 'xxx' 'xxx' 'xxx' 'xxx' 'xxx' 'xxx' 'xxx' 'xxx' 'xxx' 'xxx' 'xxx';
      | 'ynz' 'uji' 'xxx' 'xxx' 'xxx' 'xxx' 'xxx' 'xxx' 'xxx' 'xxx' 'xxx' 'xxx' 'xxx' 'xxx' 'xxx' 'xxx' 'xxx' 'xxx' 'xxx' 'xxx' 'xxx' 'xxx' 'xxx' 'xxx';
      | 'igh' 'sta' 'jmk' 'xxx' 'xxx' 'xxx' 'xxx' 'xxx' 'xxx' 'xxx' 'xxx' 'xxx' 'xxx' 'xxx' 'xxx' 'xxx' 'xxx' 'xxx' 'xxx' 'xxx' 'xxx' 'xxx' 'xxx' 'xxx';
      | 'fyx' 'krd' 'xxx' 'xxx' 'xxx' 'xxx' 'xxx' 'xxx' 'xxx' 'xxx' 'xxx' 'xxx' 'xxx' 'xxx' 'xxx' 'xxx' 'xxx' 'xxx' 'xxx' 'xxx' 'xxx' 'xxx' 'xxx' 'xxx';
      | 'gkf' 'ivn' 'mwb' 'axi' 'xxx' 'xxx' 'xxx' 'xxx' 'xxx' 'xxx' 'xxx' 'xxx' 'xxx' 'xxx' 'xxx' 'xxx' 'xxx' 'xxx' 'xxx' 'xxx' 'xxx' 'xxx' 'xxx' 'xxx';
      | 'bcz' 'ftm' 'rdm' 'wby' 'lkv' 'xxx' 'xxx' 'xxx' 'xxx' 'xxx' 'xxx' 'xxx' 'xxx' 'xxx' 'xxx' 'xxx' 'xxx' 'xxx' 'xxx' 'xxx' 'xxx' 'xxx' 'xxx' 'xxx';
      | 'qeg' 'jlg' 'qgn' 'ifs' 'ppm' 'xxx' 'xxx' 'xxx' 'xxx' 'xxx' 'xxx' 'xxx' 'xxx' 'xxx' 'xxx' 'xxx' 'xxx' 'xxx' 'xxx' 'xxx' 'xxx' 'xxx' 'xxx' 'xxx';
      | 'goq' 'icv' 'xxx' 'xxx' 'xxx' 'xxx' 'xxx' 'xxx' 'xxx' 'xxx' 'xxx' 'xxx' 'xxx' 'xxx' 'xxx' 'xxx' 'xxx' 'xxx' 'xxx' 'xxx' 'xxx' 'xxx' 'xxx' 'xxx';
      | 'qmy' 'out' 'xxx' 'xxx' 'xxx' 'xxx' 'xxx' 'xxx' 'xxx' 'xxx' 'xxx' 'xxx' 'xxx' 'xxx' 'xxx' 'xxx' 'xxx' 'xxx' 'xxx' 'xxx' 'xxx' 'xxx' 'xxx' 'xxx';
      | 'wxl' 'igh' 'heh' 'hvs' 'xxx' 'xxx' 'xxx' 'xxx' 'xxx' 'xxx' 'xxx' 'xxx' 'xxx' 'xxx' 'xxx' 'xxx' 'xxx' 'xxx' 'xxx' 'xxx' 'xxx' 'xxx' 'xxx' 'xxx';
      | 'kbe' 'dzp' 'ybw' 'xxx' 'xxx' 'xxx' 'xxx' 'xxx' 'xxx' 'xxx' 'xxx' 'xxx' 'xxx' 'xxx' 'xxx' 'xxx' 'xxx' 'xxx' 'xxx' 'xxx' 'xxx' 'xxx' 'xxx' 'xxx';
      | 'hxf' 'out' 'xxx' 'xxx' 'xxx' 'xxx' 'xxx' 'xxx' 'xxx' 'xxx' 'xxx' 'xxx' 'xxx' 'xxx' 'xxx' 'xxx' 'xxx' 'xxx' 'xxx' 'xxx' 'xxx' 'xxx' 'xxx' 'xxx';
      | 'tqw' 'rdn' 'nac' 'xxx' 'xxx' 'xxx' 'xxx' 'xxx' 'xxx' 'xxx' 'xxx' 'xxx' 'xxx' 'xxx' 'xxx' 'xxx' 'xxx' 'xxx' 'xxx' 'xxx' 'xxx' 'xxx' 'xxx' 'xxx';
      | 'bmu' 'jmn' 'gkl' 'xfg' 'xxx' 'xxx' 'xxx' 'xxx' 'xxx' 'xxx' 'xxx' 'xxx' 'xxx' 'xxx' 'xxx' 'xxx' 'xxx' 'xxx' 'xxx' 'xxx' 'xxx' 'xxx' 'xxx' 'xxx';
      | 'cqf' 'lzx' 'xxx' 'xxx' 'xxx' 'xxx' 'xxx' 'xxx' 'xxx' 'xxx' 'xxx' 'xxx' 'xxx' 'xxx' 'xxx' 'xxx' 'xxx' 'xxx' 'xxx' 'xxx' 'xxx' 'xxx' 'xxx' 'xxx';
      | 'phn' 'rbi' 'fjm' 'xxx' 'xxx' 'xxx' 'xxx' 'xxx' 'xxx' 'xxx' 'xxx' 'xxx' 'xxx' 'xxx' 'xxx' 'xxx' 'xxx' 'xxx' 'xxx' 'xxx' 'xxx' 'xxx' 'xxx' 'xxx';
      | 'ykt' 'sgu' 'fbt' 'brg' 'xxx' 'xxx' 'xxx' 'xxx' 'xxx' 'xxx' 'xxx' 'xxx' 'xxx' 'xxx' 'xxx' 'xxx' 'xxx' 'xxx' 'xxx' 'xxx' 'xxx' 'xxx' 'xxx' 'xxx';
      | 'zqg' 'out' 'xxx' 'xxx' 'xxx' 'xxx' 'xxx' 'xxx' 'xxx' 'xxx' 'xxx' 'xxx' 'xxx' 'xxx' 'xxx' 'xxx' 'xxx' 'xxx' 'xxx' 'xxx' 'xxx' 'xxx' 'xxx' 'xxx';
      | 'ain' 'mpj' 'xxx' 'xxx' 'xxx' 'xxx' 'xxx' 'xxx' 'xxx' 'xxx' 'xxx' 'xxx' 'xxx' 'xxx' 'xxx' 'xxx' 'xxx' 'xxx' 'xxx' 'xxx' 'xxx' 'xxx' 'xxx' 'xxx';
      | 'esz' 'jmk' 'txi' 'xxx' 'xxx' 'xxx' 'xxx' 'xxx' 'xxx' 'xxx' 'xxx' 'xxx' 'xxx' 'xxx' 'xxx' 'xxx' 'xxx' 'xxx' 'xxx' 'xxx' 'xxx' 'xxx' 'xxx' 'xxx';
      | 'bpj' 'rqn' 'zow' 'flj' 'wke' 'fak' 'xxx' 'xxx' 'xxx' 'xxx' 'xxx' 'xxx' 'xxx' 'xxx' 'xxx' 'xxx' 'xxx' 'xxx' 'xxx' 'xxx' 'xxx' 'xxx' 'xxx' 'xxx';
      | 'qaj' 'gtk' 'gkf' 'cuk' 'qcj' 'xxx' 'xxx' 'xxx' 'xxx' 'xxx' 'xxx' 'xxx' 'xxx' 'xxx' 'xxx' 'xxx' 'xxx' 'xxx' 'xxx' 'xxx' 'xxx' 'xxx' 'xxx' 'xxx';
      | 'kul' 'ckh' 'xxx' 'xxx' 'xxx' 'xxx' 'xxx' 'xxx' 'xxx' 'xxx' 'xxx' 'xxx' 'xxx' 'xxx' 'xxx' 'xxx' 'xxx' 'xxx' 'xxx' 'xxx' 'xxx' 'xxx' 'xxx' 'xxx';
      | 'rss' 'dka' 'nwy' 'xxx' 'xxx' 'xxx' 'xxx' 'xxx' 'xxx' 'xxx' 'xxx' 'xxx' 'xxx' 'xxx' 'xxx' 'xxx' 'xxx' 'xxx' 'xxx' 'xxx' 'xxx' 'xxx' 'xxx' 'xxx';
      | 'gaq' 'ifs' 'laq' 'jlg' 'xxx' 'xxx' 'xxx' 'xxx' 'xxx' 'xxx' 'xxx' 'xxx' 'xxx' 'xxx' 'xxx' 'xxx' 'xxx' 'xxx' 'xxx' 'xxx' 'xxx' 'xxx' 'xxx' 'xxx';
      | 'ehc' 'hco' 'qaj' 'qup' 'xxx' 'xxx' 'xxx' 'xxx' 'xxx' 'xxx' 'xxx' 'xxx' 'xxx' 'xxx' 'xxx' 'xxx' 'xxx' 'xxx' 'xxx' 'xxx' 'xxx' 'xxx' 'xxx' 'xxx';
      | 'saf' 'mwu' 'you' 'fnr' 'vrt' 'xxx' 'xxx' 'xxx' 'xxx' 'xxx' 'xxx' 'xxx' 'xxx' 'xxx' 'xxx' 'xxx' 'xxx' 'xxx' 'xxx' 'xxx' 'xxx' 'xxx' 'xxx' 'xxx';
      | 'mub' 'bee' 'xxx' 'xxx' 'xxx' 'xxx' 'xxx' 'xxx' 'xxx' 'xxx' 'xxx' 'xxx' 'xxx' 'xxx' 'xxx' 'xxx' 'xxx' 'xxx' 'xxx' 'xxx' 'xxx' 'xxx' 'xxx' 'xxx';
      | 'tns' 'lyd' 'fyy' 'bqw' 'xxx' 'xxx' 'xxx' 'xxx' 'xxx' 'xxx' 'xxx' 'xxx' 'xxx' 'xxx' 'xxx' 'xxx' 'xxx' 'xxx' 'xxx' 'xxx' 'xxx' 'xxx' 'xxx' 'xxx';
      | 'ssx' 'utb' 'nel' 'thp' 'hhu' 'wbs' 'xxx' 'xxx' 'xxx' 'xxx' 'xxx' 'xxx' 'xxx' 'xxx' 'xxx' 'xxx' 'xxx' 'xxx' 'xxx' 'xxx' 'xxx' 'xxx' 'xxx' 'xxx';
      | 'mwd' 'qeg' 'gpo' 'xxx' 'xxx' 'xxx' 'xxx' 'xxx' 'xxx' 'xxx' 'xxx' 'xxx' 'xxx' 'xxx' 'xxx' 'xxx' 'xxx' 'xxx' 'xxx' 'xxx' 'xxx' 'xxx' 'xxx' 'xxx';
      | 'lgx' 'out' 'xxx' 'xxx' 'xxx' 'xxx' 'xxx' 'xxx' 'xxx' 'xxx' 'xxx' 'xxx' 'xxx' 'xxx' 'xxx' 'xxx' 'xxx' 'xxx' 'xxx' 'xxx' 'xxx' 'xxx' 'xxx' 'xxx';
      | 'lyr' 'ozd' 'xxx' 'xxx' 'xxx' 'xxx' 'xxx' 'xxx' 'xxx' 'xxx' 'xxx' 'xxx' 'xxx' 'xxx' 'xxx' 'xxx' 'xxx' 'xxx' 'xxx' 'xxx' 'xxx' 'xxx' 'xxx' 'xxx';
      | 'knq' 'qlf' 'tnt' 'bhv' 'aeo' 'ljy' 'dmr' 'xxx' 'xxx' 'xxx' 'xxx' 'xxx' 'xxx' 'xxx' 'xxx' 'xxx' 'xxx' 'xxx' 'xxx' 'xxx' 'xxx' 'xxx' 'xxx' 'xxx';
      | 'php' 'sgu' 'xxx' 'xxx' 'xxx' 'xxx' 'xxx' 'xxx' 'xxx' 'xxx' 'xxx' 'xxx' 'xxx' 'xxx' 'xxx' 'xxx' 'xxx' 'xxx' 'xxx' 'xxx' 'xxx' 'xxx' 'xxx' 'xxx';
      | 'qmz' 'fer' 'bcz' 'xxx' 'xxx' 'xxx' 'xxx' 'xxx' 'xxx' 'xxx' 'xxx' 'xxx' 'xxx' 'xxx' 'xxx' 'xxx' 'xxx' 'xxx' 'xxx' 'xxx' 'xxx' 'xxx' 'xxx' 'xxx';
      | 'oab' 'lup' 'xxx' 'xxx' 'xxx' 'xxx' 'xxx' 'xxx' 'xxx' 'xxx' 'xxx' 'xxx' 'xxx' 'xxx' 'xxx' 'xxx' 'xxx' 'xxx' 'xxx' 'xxx' 'xxx' 'xxx' 'xxx' 'xxx';
      | 'sof' 'ikt' 'xxx' 'xxx' 'xxx' 'xxx' 'xxx' 'xxx' 'xxx' 'xxx' 'xxx' 'xxx' 'xxx' 'xxx' 'xxx' 'xxx' 'xxx' 'xxx' 'xxx' 'xxx' 'xxx' 'xxx' 'xxx' 'xxx';
      | 'lte' 'ytk' 'hbp' 'xjh' 'dne' 'wcx' 'xxx' 'xxx' 'xxx' 'xxx' 'xxx' 'xxx' 'xxx' 'xxx' 'xxx' 'xxx' 'xxx' 'xxx' 'xxx' 'xxx' 'xxx' 'xxx' 'xxx' 'xxx';
      | 'hvs' 'xee' 'txi' 'knq' 'xxx' 'xxx' 'xxx' 'xxx' 'xxx' 'xxx' 'xxx' 'xxx' 'xxx' 'xxx' 'xxx' 'xxx' 'xxx' 'xxx' 'xxx' 'xxx' 'xxx' 'xxx' 'xxx' 'xxx';
      | 'bnw' 'yhu' 'qhx' 'xxx' 'xxx' 'xxx' 'xxx' 'xxx' 'xxx' 'xxx' 'xxx' 'xxx' 'xxx' 'xxx' 'xxx' 'xxx' 'xxx' 'xxx' 'xxx' 'xxx' 'xxx' 'xxx' 'xxx' 'xxx';
      | 'jnw' 'aai' 'hco' 'qup' 'nxs' 'xxx' 'xxx' 'xxx' 'xxx' 'xxx' 'xxx' 'xxx' 'xxx' 'xxx' 'xxx' 'xxx' 'xxx' 'xxx' 'xxx' 'xxx' 'xxx' 'xxx' 'xxx' 'xxx';
      | 'uge' 'bqw' 'fyy' 'xxx' 'xxx' 'xxx' 'xxx' 'xxx' 'xxx' 'xxx' 'xxx' 'xxx' 'xxx' 'xxx' 'xxx' 'xxx' 'xxx' 'xxx' 'xxx' 'xxx' 'xxx' 'xxx' 'xxx' 'xxx';
      | 'cml' 'sid' 'txz' 'qgh' 'xxx' 'xxx' 'xxx' 'xxx' 'xxx' 'xxx' 'xxx' 'xxx' 'xxx' 'xxx' 'xxx' 'xxx' 'xxx' 'xxx' 'xxx' 'xxx' 'xxx' 'xxx' 'xxx' 'xxx';
      | 'sle' 'uwp' 'jhu' 'lra' 'ltm' 'xxx' 'xxx' 'xxx' 'xxx' 'xxx' 'xxx' 'xxx' 'xxx' 'xxx' 'xxx' 'xxx' 'xxx' 'xxx' 'xxx' 'xxx' 'xxx' 'xxx' 'xxx' 'xxx';
      | 'uoi' 'yql' 'sgu' 'xxx' 'xxx' 'xxx' 'xxx' 'xxx' 'xxx' 'xxx' 'xxx' 'xxx' 'xxx' 'xxx' 'xxx' 'xxx' 'xxx' 'xxx' 'xxx' 'xxx' 'xxx' 'xxx' 'xxx' 'xxx';
      | 'tcu' 'eao' 'hgu' 'xxx' 'xxx' 'xxx' 'xxx' 'xxx' 'xxx' 'xxx' 'xxx' 'xxx' 'xxx' 'xxx' 'xxx' 'xxx' 'xxx' 'xxx' 'xxx' 'xxx' 'xxx' 'xxx' 'xxx' 'xxx';
      | 'aaj' 'laq' 'ppm' 'xxx' 'xxx' 'xxx' 'xxx' 'xxx' 'xxx' 'xxx' 'xxx' 'xxx' 'xxx' 'xxx' 'xxx' 'xxx' 'xxx' 'xxx' 'xxx' 'xxx' 'xxx' 'xxx' 'xxx' 'xxx';
      | 'bqy' 'you' 'xxx' 'xxx' 'xxx' 'xxx' 'xxx' 'xxx' 'xxx' 'xxx' 'xxx' 'xxx' 'xxx' 'xxx' 'xxx' 'xxx' 'xxx' 'xxx' 'xxx' 'xxx' 'xxx' 'xxx' 'xxx' 'xxx';
      | 'gye' 'qpo' 'xxx' 'xxx' 'xxx' 'xxx' 'xxx' 'xxx' 'xxx' 'xxx' 'xxx' 'xxx' 'xxx' 'xxx' 'xxx' 'xxx' 'xxx' 'xxx' 'xxx' 'xxx' 'xxx' 'xxx' 'xxx' 'xxx';
      | 'csx' 'you' 'mwu' 'fnr' 'vrt' 'xxx' 'xxx' 'xxx' 'xxx' 'xxx' 'xxx' 'xxx' 'xxx' 'xxx' 'xxx' 'xxx' 'xxx' 'xxx' 'xxx' 'xxx' 'xxx' 'xxx' 'xxx' 'xxx';
      | 'uut' 'dne' 'xjh' 'wcx' 'xxx' 'xxx' 'xxx' 'xxx' 'xxx' 'xxx' 'xxx' 'xxx' 'xxx' 'xxx' 'xxx' 'xxx' 'xxx' 'xxx' 'xxx' 'xxx' 'xxx' 'xxx' 'xxx' 'xxx';
      | 'tat' 'kul' 'jxm' 'dxd' 'shb' 'wtu' 'xxx' 'xxx' 'xxx' 'xxx' 'xxx' 'xxx' 'xxx' 'xxx' 'xxx' 'xxx' 'xxx' 'xxx' 'xxx' 'xxx' 'xxx' 'xxx' 'xxx' 'xxx';
      | 'sbi' 'yvn' 'mub' 'xxx' 'xxx' 'xxx' 'xxx' 'xxx' 'xxx' 'xxx' 'xxx' 'xxx' 'xxx' 'xxx' 'xxx' 'xxx' 'xxx' 'xxx' 'xxx' 'xxx' 'xxx' 'xxx' 'xxx' 'xxx';
      | 'uss' 'suv' 'ihy' 'kbe' 'xxx' 'xxx' 'xxx' 'xxx' 'xxx' 'xxx' 'xxx' 'xxx' 'xxx' 'xxx' 'xxx' 'xxx' 'xxx' 'xxx' 'xxx' 'xxx' 'xxx' 'xxx' 'xxx' 'xxx';
      | 'def' 'wrc' 'eka' 'gpp' 'xxx' 'xxx' 'xxx' 'xxx' 'xxx' 'xxx' 'xxx' 'xxx' 'xxx' 'xxx' 'xxx' 'xxx' 'xxx' 'xxx' 'xxx' 'xxx' 'xxx' 'xxx' 'xxx' 'xxx';
      | 'rso' 'out' 'xxx' 'xxx' 'xxx' 'xxx' 'xxx' 'xxx' 'xxx' 'xxx' 'xxx' 'xxx' 'xxx' 'xxx' 'xxx' 'xxx' 'xxx' 'xxx' 'xxx' 'xxx' 'xxx' 'xxx' 'xxx' 'xxx';
      | 'dmr' 'oab' 'kbr' 'jaa' 'xxx' 'xxx' 'xxx' 'xxx' 'xxx' 'xxx' 'xxx' 'xxx' 'xxx' 'xxx' 'xxx' 'xxx' 'xxx' 'xxx' 'xxx' 'xxx' 'xxx' 'xxx' 'xxx' 'xxx';
      | 'jhu' 'xmq' 'xxx' 'xxx' 'xxx' 'xxx' 'xxx' 'xxx' 'xxx' 'xxx' 'xxx' 'xxx' 'xxx' 'xxx' 'xxx' 'xxx' 'xxx' 'xxx' 'xxx' 'xxx' 'xxx' 'xxx' 'xxx' 'xxx';
      | 'qxb' 'mub' 'sfu' 'fhq' 'yvn' 'xxx' 'xxx' 'xxx' 'xxx' 'xxx' 'xxx' 'xxx' 'xxx' 'xxx' 'xxx' 'xxx' 'xxx' 'xxx' 'xxx' 'xxx' 'xxx' 'xxx' 'xxx' 'xxx';
      | 'nww' 'htw' 'xxx' 'xxx' 'xxx' 'xxx' 'xxx' 'xxx' 'xxx' 'xxx' 'xxx' 'xxx' 'xxx' 'xxx' 'xxx' 'xxx' 'xxx' 'xxx' 'xxx' 'xxx' 'xxx' 'xxx' 'xxx' 'xxx';
      | 'szd' 'zfx' 'xxx' 'xxx' 'xxx' 'xxx' 'xxx' 'xxx' 'xxx' 'xxx' 'xxx' 'xxx' 'xxx' 'xxx' 'xxx' 'xxx' 'xxx' 'xxx' 'xxx' 'xxx' 'xxx' 'xxx' 'xxx' 'xxx';
      | 'gpp' 'qvv' 'min' 'rso' 'iey' 'xxx' 'xxx' 'xxx' 'xxx' 'xxx' 'xxx' 'xxx' 'xxx' 'xxx' 'xxx' 'xxx' 'xxx' 'xxx' 'xxx' 'xxx' 'xxx' 'xxx' 'xxx' 'xxx';
      | 'sft' 'fzl' 'hnn' 'ikt' 'xxx' 'xxx' 'xxx' 'xxx' 'xxx' 'xxx' 'xxx' 'xxx' 'xxx' 'xxx' 'xxx' 'xxx' 'xxx' 'xxx' 'xxx' 'xxx' 'xxx' 'xxx' 'xxx' 'xxx';
      | 'fwn' 'mei' 'iur' 'xxx' 'xxx' 'xxx' 'xxx' 'xxx' 'xxx' 'xxx' 'xxx' 'xxx' 'xxx' 'xxx' 'xxx' 'xxx' 'xxx' 'xxx' 'xxx' 'xxx' 'xxx' 'xxx' 'xxx' 'xxx';
      | 'giz' 'txi' 'sta' 'jmk' 'xxx' 'xxx' 'xxx' 'xxx' 'xxx' 'xxx' 'xxx' 'xxx' 'xxx' 'xxx' 'xxx' 'xxx' 'xxx' 'xxx' 'xxx' 'xxx' 'xxx' 'xxx' 'xxx' 'xxx';
      | 'you' 'hzn' 'izj' 'oil' 'krt' 'wid' 'awl' 'vbp' 'csd' 'xxx' 'xxx' 'xxx' 'xxx' 'xxx' 'xxx' 'xxx' 'xxx' 'xxx' 'xxx' 'xxx' 'xxx' 'xxx' 'xxx' 'xxx';
      | 'yvs' 'fpb' 'lur' 'xhk' 'bsb' 'xxx' 'xxx' 'xxx' 'xxx' 'xxx' 'xxx' 'xxx' 'xxx' 'xxx' 'xxx' 'xxx' 'xxx' 'xxx' 'xxx' 'xxx' 'xxx' 'xxx' 'xxx' 'xxx';
      | 'mci' 'jrk' 'ipm' 'kkp' 'xxx' 'xxx' 'xxx' 'xxx' 'xxx' 'xxx' 'xxx' 'xxx' 'xxx' 'xxx' 'xxx' 'xxx' 'xxx' 'xxx' 'xxx' 'xxx' 'xxx' 'xxx' 'xxx' 'xxx';
      | 'nqo' 'uwp' 'jhu' 'cje' 'xxx' 'xxx' 'xxx' 'xxx' 'xxx' 'xxx' 'xxx' 'xxx' 'xxx' 'xxx' 'xxx' 'xxx' 'xxx' 'xxx' 'xxx' 'xxx' 'xxx' 'xxx' 'xxx' 'xxx';
      | 'alh' 'jmk' 'xee' 'sta' 'txi' 'xxx' 'xxx' 'xxx' 'xxx' 'xxx' 'xxx' 'xxx' 'xxx' 'xxx' 'xxx' 'xxx' 'xxx' 'xxx' 'xxx' 'xxx' 'xxx' 'xxx' 'xxx' 'xxx';
      | 'ejz' 'fjm' 'rbi' 'fim' 'xxx' 'xxx' 'xxx' 'xxx' 'xxx' 'xxx' 'xxx' 'xxx' 'xxx' 'xxx' 'xxx' 'xxx' 'xxx' 'xxx' 'xxx' 'xxx' 'xxx' 'xxx' 'xxx' 'xxx';
      | 'jnd' 'wua' 'esz' 'xxx' 'xxx' 'xxx' 'xxx' 'xxx' 'xxx' 'xxx' 'xxx' 'xxx' 'xxx' 'xxx' 'xxx' 'xxx' 'xxx' 'xxx' 'xxx' 'xxx' 'xxx' 'xxx' 'xxx' 'xxx';
      | 'igu' 'nta' 'pmu' 'yun' 'cur' 'ril' 'ybr' 'rxn' 'zwl' 'uzn' 'fnn' 'cqs' 'ixc' 'puz' 'sle' 'zzk' 'jpb' 'nqo' 'zib' 'xxx' 'xxx' 'xxx' 'xxx' 'xxx';
      | 'yft' 'tky' 'kcj' 'xxx' 'xxx' 'xxx' 'xxx' 'xxx' 'xxx' 'xxx' 'xxx' 'xxx' 'xxx' 'xxx' 'xxx' 'xxx' 'xxx' 'xxx' 'xxx' 'xxx' 'xxx' 'xxx' 'xxx' 'xxx';
      | 'vxt' 'sid' 'xxx' 'xxx' 'xxx' 'xxx' 'xxx' 'xxx' 'xxx' 'xxx' 'xxx' 'xxx' 'xxx' 'xxx' 'xxx' 'xxx' 'xxx' 'xxx' 'xxx' 'xxx' 'xxx' 'xxx' 'xxx' 'xxx';
      | 'dni' 'hvs' 'heh' 'mpi' 'xxx' 'xxx' 'xxx' 'xxx' 'xxx' 'xxx' 'xxx' 'xxx' 'xxx' 'xxx' 'xxx' 'xxx' 'xxx' 'xxx' 'xxx' 'xxx' 'xxx' 'xxx' 'xxx' 'xxx';
      | 'jwy' 'wtu' 'xxx' 'xxx' 'xxx' 'xxx' 'xxx' 'xxx' 'xxx' 'xxx' 'xxx' 'xxx' 'xxx' 'xxx' 'xxx' 'xxx' 'xxx' 'xxx' 'xxx' 'xxx' 'xxx' 'xxx' 'xxx' 'xxx';
      | 'ypu' 'yrt' 'xxx' 'xxx' 'xxx' 'xxx' 'xxx' 'xxx' 'xxx' 'xxx' 'xxx' 'xxx' 'xxx' 'xxx' 'xxx' 'xxx' 'xxx' 'xxx' 'xxx' 'xxx' 'xxx' 'xxx' 'xxx' 'xxx';
      | 'rqn' 'lzu' 'dni' 'xxx' 'xxx' 'xxx' 'xxx' 'xxx' 'xxx' 'xxx' 'xxx' 'xxx' 'xxx' 'xxx' 'xxx' 'xxx' 'xxx' 'xxx' 'xxx' 'xxx' 'xxx' 'xxx' 'xxx' 'xxx';
      | 'yfw' 'bag' 'puu' 'yba' 'xxx' 'xxx' 'xxx' 'xxx' 'xxx' 'xxx' 'xxx' 'xxx' 'xxx' 'xxx' 'xxx' 'xxx' 'xxx' 'xxx' 'xxx' 'xxx' 'xxx' 'xxx' 'xxx' 'xxx';
      | 'vgx' 'amv' 'gte' 'qwd' 'hpw' 'xxx' 'xxx' 'xxx' 'xxx' 'xxx' 'xxx' 'xxx' 'xxx' 'xxx' 'xxx' 'xxx' 'xxx' 'xxx' 'xxx' 'xxx' 'xxx' 'xxx' 'xxx' 'xxx';
      | 'hgb' 'out' 'xxx' 'xxx' 'xxx' 'xxx' 'xxx' 'xxx' 'xxx' 'xxx' 'xxx' 'xxx' 'xxx' 'xxx' 'xxx' 'xxx' 'xxx' 'xxx' 'xxx' 'xxx' 'xxx' 'xxx' 'xxx' 'xxx';
      | 'gwp' 'nxs' 'qaj' 'xxx' 'xxx' 'xxx' 'xxx' 'xxx' 'xxx' 'xxx' 'xxx' 'xxx' 'xxx' 'xxx' 'xxx' 'xxx' 'xxx' 'xxx' 'xxx' 'xxx' 'xxx' 'xxx' 'xxx' 'xxx';
      | 'obo' 'fbt' 'xxx' 'xxx' 'xxx' 'xxx' 'xxx' 'xxx' 'xxx' 'xxx' 'xxx' 'xxx' 'xxx' 'xxx' 'xxx' 'xxx' 'xxx' 'xxx' 'xxx' 'xxx' 'xxx' 'xxx' 'xxx' 'xxx';
      | 'yhu' 'xkn' 'jai' 'boa' 'xxx' 'xxx' 'xxx' 'xxx' 'xxx' 'xxx' 'xxx' 'xxx' 'xxx' 'xxx' 'xxx' 'xxx' 'xxx' 'xxx' 'xxx' 'xxx' 'xxx' 'xxx' 'xxx' 'xxx';
      | 'phi' 'bqy' 'ftm' 'xxx' 'xxx' 'xxx' 'xxx' 'xxx' 'xxx' 'xxx' 'xxx' 'xxx' 'xxx' 'xxx' 'xxx' 'xxx' 'xxx' 'xxx' 'xxx' 'xxx' 'xxx' 'xxx' 'xxx' 'xxx';
      | 'cmi' 'xyj' 'xxx' 'xxx' 'xxx' 'xxx' 'xxx' 'xxx' 'xxx' 'xxx' 'xxx' 'xxx' 'xxx' 'xxx' 'xxx' 'xxx' 'xxx' 'xxx' 'xxx' 'xxx' 'xxx' 'xxx' 'xxx' 'xxx';
      | 'mvn' 'ruf' 'btp' 'xxx' 'xxx' 'xxx' 'xxx' 'xxx' 'xxx' 'xxx' 'xxx' 'xxx' 'xxx' 'xxx' 'xxx' 'xxx' 'xxx' 'xxx' 'xxx' 'xxx' 'xxx' 'xxx' 'xxx' 'xxx';
      | 'utn' 'ikt' 'xxx' 'xxx' 'xxx' 'xxx' 'xxx' 'xxx' 'xxx' 'xxx' 'xxx' 'xxx' 'xxx' 'xxx' 'xxx' 'xxx' 'xxx' 'xxx' 'xxx' 'xxx' 'xxx' 'xxx' 'xxx' 'xxx';
      | 'mkd' 'zcf' 'giz' 'alh' 'xxx' 'xxx' 'xxx' 'xxx' 'xxx' 'xxx' 'xxx' 'xxx' 'xxx' 'xxx' 'xxx' 'xxx' 'xxx' 'xxx' 'xxx' 'xxx' 'xxx' 'xxx' 'xxx' 'xxx';
      | 'eff' 'zow' 'rqn' 'wke' 'flj' 'xxx' 'xxx' 'xxx' 'xxx' 'xxx' 'xxx' 'xxx' 'xxx' 'xxx' 'xxx' 'xxx' 'xxx' 'xxx' 'xxx' 'xxx' 'xxx' 'xxx' 'xxx' 'xxx';
      | 'dml' 'yql' 'brg' 'sgu' 'fbt' 'xxx' 'xxx' 'xxx' 'xxx' 'xxx' 'xxx' 'xxx' 'xxx' 'xxx' 'xxx' 'xxx' 'xxx' 'xxx' 'xxx' 'xxx' 'xxx' 'xxx' 'xxx' 'xxx';
      | 'ivn' 'out' 'xxx' 'xxx' 'xxx' 'xxx' 'xxx' 'xxx' 'xxx' 'xxx' 'xxx' 'xxx' 'xxx' 'xxx' 'xxx' 'xxx' 'xxx' 'xxx' 'xxx' 'xxx' 'xxx' 'xxx' 'xxx' 'xxx';
      | 'fft' 'fyy' 'lyd' 'xxx' 'xxx' 'xxx' 'xxx' 'xxx' 'xxx' 'xxx' 'xxx' 'xxx' 'xxx' 'xxx' 'xxx' 'xxx' 'xxx' 'xxx' 'xxx' 'xxx' 'xxx' 'xxx' 'xxx' 'xxx';
      | 'vbp' 'vnz' 'xxx' 'xxx' 'xxx' 'xxx' 'xxx' 'xxx' 'xxx' 'xxx' 'xxx' 'xxx' 'xxx' 'xxx' 'xxx' 'xxx' 'xxx' 'xxx' 'xxx' 'xxx' 'xxx' 'xxx' 'xxx' 'xxx';
      | 'cuk' 'ivn' 'lgx' 'axi' 'nrx' 'xxx' 'xxx' 'xxx' 'xxx' 'xxx' 'xxx' 'xxx' 'xxx' 'xxx' 'xxx' 'xxx' 'xxx' 'xxx' 'xxx' 'xxx' 'xxx' 'xxx' 'xxx' 'xxx';
      | 'brb' 'lts' 'bcq' 'xsx' 'fan' 'xxx' 'xxx' 'xxx' 'xxx' 'xxx' 'xxx' 'xxx' 'xxx' 'xxx' 'xxx' 'xxx' 'xxx' 'xxx' 'xxx' 'xxx' 'xxx' 'xxx' 'xxx' 'xxx';
      | 'ckh' 'out' 'xxx' 'xxx' 'xxx' 'xxx' 'xxx' 'xxx' 'xxx' 'xxx' 'xxx' 'xxx' 'xxx' 'xxx' 'xxx' 'xxx' 'xxx' 'xxx' 'xxx' 'xxx' 'xxx' 'xxx' 'xxx' 'xxx';
      | 'cui' 'zrg' 'elj' 'wrh' 'vnz' 'uss' 'xxx' 'xxx' 'xxx' 'xxx' 'xxx' 'xxx' 'xxx' 'xxx' 'xxx' 'xxx' 'xxx' 'xxx' 'xxx' 'xxx' 'xxx' 'xxx' 'xxx' 'xxx';
      | 'ybw' 'pxr' 'xxx' 'xxx' 'xxx' 'xxx' 'xxx' 'xxx' 'xxx' 'xxx' 'xxx' 'xxx' 'xxx' 'xxx' 'xxx' 'xxx' 'xxx' 'xxx' 'xxx' 'xxx' 'xxx' 'xxx' 'xxx' 'xxx';
      | 'sfu' 'bee' 'ynz' 'xxx' 'xxx' 'xxx' 'xxx' 'xxx' 'xxx' 'xxx' 'xxx' 'xxx' 'xxx' 'xxx' 'xxx' 'xxx' 'xxx' 'xxx' 'xxx' 'xxx' 'xxx' 'xxx' 'xxx' 'xxx';
      | 'aov' 'gyl' 'xyj' 'xxx' 'xxx' 'xxx' 'xxx' 'xxx' 'xxx' 'xxx' 'xxx' 'xxx' 'xxx' 'xxx' 'xxx' 'xxx' 'xxx' 'xxx' 'xxx' 'xxx' 'xxx' 'xxx' 'xxx' 'xxx';
      | 'yxq' 'jsh' 'smb' 'qhx' 'xxx' 'xxx' 'xxx' 'xxx' 'xxx' 'xxx' 'xxx' 'xxx' 'xxx' 'xxx' 'xxx' 'xxx' 'xxx' 'xxx' 'xxx' 'xxx' 'xxx' 'xxx' 'xxx' 'xxx';
      | 'hgq' 'xvu' 'xxx' 'xxx' 'xxx' 'xxx' 'xxx' 'xxx' 'xxx' 'xxx' 'xxx' 'xxx' 'xxx' 'xxx' 'xxx' 'xxx' 'xxx' 'xxx' 'xxx' 'xxx' 'xxx' 'xxx' 'xxx' 'xxx';
      | 'yba' 'pab' 'xbk' 'bvq' 'xxx' 'xxx' 'xxx' 'xxx' 'xxx' 'xxx' 'xxx' 'xxx' 'xxx' 'xxx' 'xxx' 'xxx' 'xxx' 'xxx' 'xxx' 'xxx' 'xxx' 'xxx' 'xxx' 'xxx';
      | 'ser' 'mzo' 'vii' 'hgb' 'qmy' 'xxx' 'xxx' 'xxx' 'xxx' 'xxx' 'xxx' 'xxx' 'xxx' 'xxx' 'xxx' 'xxx' 'xxx' 'xxx' 'xxx' 'xxx' 'xxx' 'xxx' 'xxx' 'xxx';
      | 'xfg' 'txi' 'xee' 'xxx' 'xxx' 'xxx' 'xxx' 'xxx' 'xxx' 'xxx' 'xxx' 'xxx' 'xxx' 'xxx' 'xxx' 'xxx' 'xxx' 'xxx' 'xxx' 'xxx' 'xxx' 'xxx' 'xxx' 'xxx';
      | 'iey' 'out' 'xxx' 'xxx' 'xxx' 'xxx' 'xxx' 'xxx' 'xxx' 'xxx' 'xxx' 'xxx' 'xxx' 'xxx' 'xxx' 'xxx' 'xxx' 'xxx' 'xxx' 'xxx' 'xxx' 'xxx' 'xxx' 'xxx';
      | 'vhi' 'jaa' 'kbr' 'evt' 'ndc' 'xxx' 'xxx' 'xxx' 'xxx' 'xxx' 'xxx' 'xxx' 'xxx' 'xxx' 'xxx' 'xxx' 'xxx' 'xxx' 'xxx' 'xxx' 'xxx' 'xxx' 'xxx' 'xxx';
      | 'kcj' 'hbp' 'xxx' 'xxx' 'xxx' 'xxx' 'xxx' 'xxx' 'xxx' 'xxx' 'xxx' 'xxx' 'xxx' 'xxx' 'xxx' 'xxx' 'xxx' 'xxx' 'xxx' 'xxx' 'xxx' 'xxx' 'xxx' 'xxx';
      | 'qmf' 'zfx' 'xxx' 'xxx' 'xxx' 'xxx' 'xxx' 'xxx' 'xxx' 'xxx' 'xxx' 'xxx' 'xxx' 'xxx' 'xxx' 'xxx' 'xxx' 'xxx' 'xxx' 'xxx' 'xxx' 'xxx' 'xxx' 'xxx';
      | 'tum' 'sgu' 'brg' 'yql' 'xxx' 'xxx' 'xxx' 'xxx' 'xxx' 'xxx' 'xxx' 'xxx' 'xxx' 'xxx' 'xxx' 'xxx' 'xxx' 'xxx' 'xxx' 'xxx' 'xxx' 'xxx' 'xxx' 'xxx';
      | 'sva' 'her' 'yfw' 'anr' 'xxx' 'xxx' 'xxx' 'xxx' 'xxx' 'xxx' 'xxx' 'xxx' 'xxx' 'xxx' 'xxx' 'xxx' 'xxx' 'xxx' 'xxx' 'xxx' 'xxx' 'xxx' 'xxx' 'xxx';
      | 'ctm' 'cyc' 'xxx' 'xxx' 'xxx' 'xxx' 'xxx' 'xxx' 'xxx' 'xxx' 'xxx' 'xxx' 'xxx' 'xxx' 'xxx' 'xxx' 'xxx' 'xxx' 'xxx' 'xxx' 'xxx' 'xxx' 'xxx' 'xxx';
      | 'sta' 'ewm' 'izk' 'bhv' 'tnt' 'vhi' 'hkq' 'ljy' 'waa' 'aeo' 'ofz' 'xhd' 'fcj' 'gwo' 'qlf' 'nhj' 'xxx' 'xxx' 'xxx' 'xxx' 'xxx' 'xxx' 'xxx' 'xxx';
      | 'jai' 'fbt' 'sgu' 'xxx' 'xxx' 'xxx' 'xxx' 'xxx' 'xxx' 'xxx' 'xxx' 'xxx' 'xxx' 'xxx' 'xxx' 'xxx' 'xxx' 'xxx' 'xxx' 'xxx' 'xxx' 'xxx' 'xxx' 'xxx';
      | 'iyj' 'dka' 'kez' 'nwy' 'xxx' 'xxx' 'xxx' 'xxx' 'xxx' 'xxx' 'xxx' 'xxx' 'xxx' 'xxx' 'xxx' 'xxx' 'xxx' 'xxx' 'xxx' 'xxx' 'xxx' 'xxx' 'xxx' 'xxx';
      | 'ofd' 'tlb' 'xxx' 'xxx' 'xxx' 'xxx' 'xxx' 'xxx' 'xxx' 'xxx' 'xxx' 'xxx' 'xxx' 'xxx' 'xxx' 'xxx' 'xxx' 'xxx' 'xxx' 'xxx' 'xxx' 'xxx' 'xxx' 'xxx';
      | 'qff' 'rcp' 'osk' 'xxx' 'xxx' 'xxx' 'xxx' 'xxx' 'xxx' 'xxx' 'xxx' 'xxx' 'xxx' 'xxx' 'xxx' 'xxx' 'xxx' 'xxx' 'xxx' 'xxx' 'xxx' 'xxx' 'xxx' 'xxx';
      | 'wbs' 'fnr' 'you' 'mwu' 'vrt' 'ozd' 'xxx' 'xxx' 'xxx' 'xxx' 'xxx' 'xxx' 'xxx' 'xxx' 'xxx' 'xxx' 'xxx' 'xxx' 'xxx' 'xxx' 'xxx' 'xxx' 'xxx' 'xxx';
      | 'ulj' 'hrd' 'tcu' 'uqb' 'xxx' 'xxx' 'xxx' 'xxx' 'xxx' 'xxx' 'xxx' 'xxx' 'xxx' 'xxx' 'xxx' 'xxx' 'xxx' 'xxx' 'xxx' 'xxx' 'xxx' 'xxx' 'xxx' 'xxx';
      | 'uvk' 'vxt' 'grp' 'qgy' 'xxx' 'xxx' 'xxx' 'xxx' 'xxx' 'xxx' 'xxx' 'xxx' 'xxx' 'xxx' 'xxx' 'xxx' 'xxx' 'xxx' 'xxx' 'xxx' 'xxx' 'xxx' 'xxx' 'xxx';
      | 'txz' 'irm' 'jwy' 'fmr' 'xxx' 'xxx' 'xxx' 'xxx' 'xxx' 'xxx' 'xxx' 'xxx' 'xxx' 'xxx' 'xxx' 'xxx' 'xxx' 'xxx' 'xxx' 'xxx' 'xxx' 'xxx' 'xxx' 'xxx';
      | 'yco' 'out' 'xxx' 'xxx' 'xxx' 'xxx' 'xxx' 'xxx' 'xxx' 'xxx' 'xxx' 'xxx' 'xxx' 'xxx' 'xxx' 'xxx' 'xxx' 'xxx' 'xxx' 'xxx' 'xxx' 'xxx' 'xxx' 'xxx';
      | 'hlo' 'fxp' 'ser' 'xxx' 'xxx' 'xxx' 'xxx' 'xxx' 'xxx' 'xxx' 'xxx' 'xxx' 'xxx' 'xxx' 'xxx' 'xxx' 'xxx' 'xxx' 'xxx' 'xxx' 'xxx' 'xxx' 'xxx' 'xxx';
      | 'gsc' 'ldf' 'yqe' 'ulj' 'xxx' 'xxx' 'xxx' 'xxx' 'xxx' 'xxx' 'xxx' 'xxx' 'xxx' 'xxx' 'xxx' 'xxx' 'xxx' 'xxx' 'xxx' 'xxx' 'xxx' 'xxx' 'xxx' 'xxx';
      | 'vpo' 'zxj' 'tlb' 'xxx' 'xxx' 'xxx' 'xxx' 'xxx' 'xxx' 'xxx' 'xxx' 'xxx' 'xxx' 'xxx' 'xxx' 'xxx' 'xxx' 'xxx' 'xxx' 'xxx' 'xxx' 'xxx' 'xxx' 'xxx';
      | 'jgf' 'laq' 'xxx' 'xxx' 'xxx' 'xxx' 'xxx' 'xxx' 'xxx' 'xxx' 'xxx' 'xxx' 'xxx' 'xxx' 'xxx' 'xxx' 'xxx' 'xxx' 'xxx' 'xxx' 'xxx' 'xxx' 'xxx' 'xxx';
      | 'hns' 'uoi' 'tmc' 'ece' 'xxx' 'xxx' 'xxx' 'xxx' 'xxx' 'xxx' 'xxx' 'xxx' 'xxx' 'xxx' 'xxx' 'xxx' 'xxx' 'xxx' 'xxx' 'xxx' 'xxx' 'xxx' 'xxx' 'xxx';
      | 'cvi' 'gpt' 'otp' 'sva' 'xxx' 'xxx' 'xxx' 'xxx' 'xxx' 'xxx' 'xxx' 'xxx' 'xxx' 'xxx' 'xxx' 'xxx' 'xxx' 'xxx' 'xxx' 'xxx' 'xxx' 'xxx' 'xxx' 'xxx';
      | 'cur' 'kob' 'kde' 'qmz' 'xxx' 'xxx' 'xxx' 'xxx' 'xxx' 'xxx' 'xxx' 'xxx' 'xxx' 'xxx' 'xxx' 'xxx' 'xxx' 'xxx' 'xxx' 'xxx' 'xxx' 'xxx' 'xxx' 'xxx';
      | 'lre' 'ipm' 'xxx' 'xxx' 'xxx' 'xxx' 'xxx' 'xxx' 'xxx' 'xxx' 'xxx' 'xxx' 'xxx' 'xxx' 'xxx' 'xxx' 'xxx' 'xxx' 'xxx' 'xxx' 'xxx' 'xxx' 'xxx' 'xxx';
      | 'ryr' 'wpn' 'fdl' 'xxx' 'xxx' 'xxx' 'xxx' 'xxx' 'xxx' 'xxx' 'xxx' 'xxx' 'xxx' 'xxx' 'xxx' 'xxx' 'xxx' 'xxx' 'xxx' 'xxx' 'xxx' 'xxx' 'xxx' 'xxx';
      | 'wrc' 'iey' 'yco' 'xxx' 'xxx' 'xxx' 'xxx' 'xxx' 'xxx' 'xxx' 'xxx' 'xxx' 'xxx' 'xxx' 'xxx' 'xxx' 'xxx' 'xxx' 'xxx' 'xxx' 'xxx' 'xxx' 'xxx' 'xxx';
      | 'ftq' 'fvb' 'kbp' 'scb' 'oap' 'cvl' 'xxx' 'xxx' 'xxx' 'xxx' 'xxx' 'xxx' 'xxx' 'xxx' 'xxx' 'xxx' 'xxx' 'xxx' 'xxx' 'xxx' 'xxx' 'xxx' 'xxx' 'xxx';
      | 'qwd' 'tns' 'wks' 'uge' 'xxx' 'xxx' 'xxx' 'xxx' 'xxx' 'xxx' 'xxx' 'xxx' 'xxx' 'xxx' 'xxx' 'xxx' 'xxx' 'xxx' 'xxx' 'xxx' 'xxx' 'xxx' 'xxx' 'xxx';
      | 'laq' 'ryr' 'nhf' 'srh' 'zrw' 'bvv' 'xje' 'gep' 'phn' 'ejz' 'ucp' 'vgx' 'foj' 'gdh' 'tph' 'xxx' 'xxx' 'xxx' 'xxx' 'xxx' 'xxx' 'xxx' 'xxx' 'xxx';
      | 'fyy' 'vin' 'obo' 'dml' 'php' 'tum' 'xxx' 'xxx' 'xxx' 'xxx' 'xxx' 'xxx' 'xxx' 'xxx' 'xxx' 'xxx' 'xxx' 'xxx' 'xxx' 'xxx' 'xxx' 'xxx' 'xxx' 'xxx';
      | 'iyi' 'yqe' 'ldf' 'axk' 'xxx' 'xxx' 'xxx' 'xxx' 'xxx' 'xxx' 'xxx' 'xxx' 'xxx' 'xxx' 'xxx' 'xxx' 'xxx' 'xxx' 'xxx' 'xxx' 'xxx' 'xxx' 'xxx' 'xxx';
      | 'wck' 'mei' 'iur' 'xxx' 'xxx' 'xxx' 'xxx' 'xxx' 'xxx' 'xxx' 'xxx' 'xxx' 'xxx' 'xxx' 'xxx' 'xxx' 'xxx' 'xxx' 'xxx' 'xxx' 'xxx' 'xxx' 'xxx' 'xxx';
      | 'lzu' 'mpi' 'xxx' 'xxx' 'xxx' 'xxx' 'xxx' 'xxx' 'xxx' 'xxx' 'xxx' 'xxx' 'xxx' 'xxx' 'xxx' 'xxx' 'xxx' 'xxx' 'xxx' 'xxx' 'xxx' 'xxx' 'xxx' 'xxx';
      | 'btp' 'uvl' 'ctm' 'bvs' 'jax' 'xxx' 'xxx' 'xxx' 'xxx' 'xxx' 'xxx' 'xxx' 'xxx' 'xxx' 'xxx' 'xxx' 'xxx' 'xxx' 'xxx' 'xxx' 'xxx' 'xxx' 'xxx' 'xxx';
      | 'zib' 'jhu' 'lra' 'cje' 'ltm' 'uwp' 'xxx' 'xxx' 'xxx' 'xxx' 'xxx' 'xxx' 'xxx' 'xxx' 'xxx' 'xxx' 'xxx' 'xxx' 'xxx' 'xxx' 'xxx' 'xxx' 'xxx' 'xxx';
      | 'dac' 'lyr' 'csx' 'saf' 'rmg' 'vns' 'xxx' 'xxx' 'xxx' 'xxx' 'xxx' 'xxx' 'xxx' 'xxx' 'xxx' 'xxx' 'xxx' 'xxx' 'xxx' 'xxx' 'xxx' 'xxx' 'xxx' 'xxx';
      | 'pje' 'lts' 'ykt' 'bcq' 'xxx' 'xxx' 'xxx' 'xxx' 'xxx' 'xxx' 'xxx' 'xxx' 'xxx' 'xxx' 'xxx' 'xxx' 'xxx' 'xxx' 'xxx' 'xxx' 'xxx' 'xxx' 'xxx' 'xxx';
      | 'awp' 'oap' 'kbp' 'xxx' 'xxx' 'xxx' 'xxx' 'xxx' 'xxx' 'xxx' 'xxx' 'xxx' 'xxx' 'xxx' 'xxx' 'xxx' 'xxx' 'xxx' 'xxx' 'xxx' 'xxx' 'xxx' 'xxx' 'xxx';
      | 'iqf' 'lyr' 'vns' 'xxx' 'xxx' 'xxx' 'xxx' 'xxx' 'xxx' 'xxx' 'xxx' 'xxx' 'xxx' 'xxx' 'xxx' 'xxx' 'xxx' 'xxx' 'xxx' 'xxx' 'xxx' 'xxx' 'xxx' 'xxx';
      | 'fac' 'qgn' 'xxx' 'xxx' 'xxx' 'xxx' 'xxx' 'xxx' 'xxx' 'xxx' 'xxx' 'xxx' 'xxx' 'xxx' 'xxx' 'xxx' 'xxx' 'xxx' 'xxx' 'xxx' 'xxx' 'xxx' 'xxx' 'xxx';
      | 'iiu' 'lre' 'xxx' 'xxx' 'xxx' 'xxx' 'xxx' 'xxx' 'xxx' 'xxx' 'xxx' 'xxx' 'xxx' 'xxx' 'xxx' 'xxx' 'xxx' 'xxx' 'xxx' 'xxx' 'xxx' 'xxx' 'xxx' 'xxx';
      | 'gmb' 'min' 'rso' 'xxx' 'xxx' 'xxx' 'xxx' 'xxx' 'xxx' 'xxx' 'xxx' 'xxx' 'xxx' 'xxx' 'xxx' 'xxx' 'xxx' 'xxx' 'xxx' 'xxx' 'xxx' 'xxx' 'xxx' 'xxx';
      | 'pxk' 'wsm' 'xxx' 'xxx' 'xxx' 'xxx' 'xxx' 'xxx' 'xxx' 'xxx' 'xxx' 'xxx' 'xxx' 'xxx' 'xxx' 'xxx' 'xxx' 'xxx' 'xxx' 'xxx' 'xxx' 'xxx' 'xxx' 'xxx';
      | 'icv' 'jlg' 'ifs' 'laq' 'xxx' 'xxx' 'xxx' 'xxx' 'xxx' 'xxx' 'xxx' 'xxx' 'xxx' 'xxx' 'xxx' 'xxx' 'xxx' 'xxx' 'xxx' 'xxx' 'xxx' 'xxx' 'xxx' 'xxx';
      | 'tnt' 'oab' 'ndc' 'kbr' 'evt' 'xxx' 'xxx' 'xxx' 'xxx' 'xxx' 'xxx' 'xxx' 'xxx' 'xxx' 'xxx' 'xxx' 'xxx' 'xxx' 'xxx' 'xxx' 'xxx' 'xxx' 'xxx' 'xxx';
      | 'guw' 'otp' 'qwo' 'xxx' 'xxx' 'xxx' 'xxx' 'xxx' 'xxx' 'xxx' 'xxx' 'xxx' 'xxx' 'xxx' 'xxx' 'xxx' 'xxx' 'xxx' 'xxx' 'xxx' 'xxx' 'xxx' 'xxx' 'xxx';
      | 'rjp' 'fbt' 'sgu' 'xxx' 'xxx' 'xxx' 'xxx' 'xxx' 'xxx' 'xxx' 'xxx' 'xxx' 'xxx' 'xxx' 'xxx' 'xxx' 'xxx' 'xxx' 'xxx' 'xxx' 'xxx' 'xxx' 'xxx' 'xxx';
      | 'iqh' 'srf' 'vim' 'mli' 'slg' 'xxx' 'xxx' 'xxx' 'xxx' 'xxx' 'xxx' 'xxx' 'xxx' 'xxx' 'xxx' 'xxx' 'xxx' 'xxx' 'xxx' 'xxx' 'xxx' 'xxx' 'xxx' 'xxx';
      | 'xje' 'mpy' 'xxx' 'xxx' 'xxx' 'xxx' 'xxx' 'xxx' 'xxx' 'xxx' 'xxx' 'xxx' 'xxx' 'xxx' 'xxx' 'xxx' 'xxx' 'xxx' 'xxx' 'xxx' 'xxx' 'xxx' 'xxx' 'xxx';
      | 'cmt' 'amv' 'gte' 'xxx' 'xxx' 'xxx' 'xxx' 'xxx' 'xxx' 'xxx' 'xxx' 'xxx' 'xxx' 'xxx' 'xxx' 'xxx' 'xxx' 'xxx' 'xxx' 'xxx' 'xxx' 'xxx' 'xxx' 'xxx';
      | 'kob' 'bcz' 'fer' 'xxx' 'xxx' 'xxx' 'xxx' 'xxx' 'xxx' 'xxx' 'xxx' 'xxx' 'xxx' 'xxx' 'xxx' 'xxx' 'xxx' 'xxx' 'xxx' 'xxx' 'xxx' 'xxx' 'xxx' 'xxx';
      | 'fzl' 'igu' 'fpb' 'xxx' 'xxx' 'xxx' 'xxx' 'xxx' 'xxx' 'xxx' 'xxx' 'xxx' 'xxx' 'xxx' 'xxx' 'xxx' 'xxx' 'xxx' 'xxx' 'xxx' 'xxx' 'xxx' 'xxx' 'xxx';
      | 'bud' 'rss' 'fxl' 'xxx' 'xxx' 'xxx' 'xxx' 'xxx' 'xxx' 'xxx' 'xxx' 'xxx' 'xxx' 'xxx' 'xxx' 'xxx' 'xxx' 'xxx' 'xxx' 'xxx' 'xxx' 'xxx' 'xxx' 'xxx';
      | 'lup' 'fvb' 'cvl' 'xxx' 'xxx' 'xxx' 'xxx' 'xxx' 'xxx' 'xxx' 'xxx' 'xxx' 'xxx' 'xxx' 'xxx' 'xxx' 'xxx' 'xxx' 'xxx' 'xxx' 'xxx' 'xxx' 'xxx' 'xxx';
      | 'bpc' 'jsh' 'smb' 'yhu' 'xxx' 'xxx' 'xxx' 'xxx' 'xxx' 'xxx' 'xxx' 'xxx' 'xxx' 'xxx' 'xxx' 'xxx' 'xxx' 'xxx' 'xxx' 'xxx' 'xxx' 'xxx' 'xxx' 'xxx';
      | 'jui' 'fnr' 'mwu' 'you' 'vrt' 'ozd' 'xxx' 'xxx' 'xxx' 'xxx' 'xxx' 'xxx' 'xxx' 'xxx' 'xxx' 'xxx' 'xxx' 'xxx' 'xxx' 'xxx' 'xxx' 'xxx' 'xxx' 'xxx';
      | 'wmr' 'tmc' 'uoi' 'wvh' 'xxx' 'xxx' 'xxx' 'xxx' 'xxx' 'xxx' 'xxx' 'xxx' 'xxx' 'xxx' 'xxx' 'xxx' 'xxx' 'xxx' 'xxx' 'xxx' 'xxx' 'xxx' 'xxx' 'xxx';
      | 'ulo' 'yql' 'brg' 'sgu' 'xxx' 'xxx' 'xxx' 'xxx' 'xxx' 'xxx' 'xxx' 'xxx' 'xxx' 'xxx' 'xxx' 'xxx' 'xxx' 'xxx' 'xxx' 'xxx' 'xxx' 'xxx' 'xxx' 'xxx';
      | 'quz' 'hns' 'avo' 'euq' 'zad' 'xxx' 'xxx' 'xxx' 'xxx' 'xxx' 'xxx' 'xxx' 'xxx' 'xxx' 'xxx' 'xxx' 'xxx' 'xxx' 'xxx' 'xxx' 'xxx' 'xxx' 'xxx' 'xxx';
      | 'avo' 'wvh' 'uoi' 'tmc' 'xxx' 'xxx' 'xxx' 'xxx' 'xxx' 'xxx' 'xxx' 'xxx' 'xxx' 'xxx' 'xxx' 'xxx' 'xxx' 'xxx' 'xxx' 'xxx' 'xxx' 'xxx' 'xxx' 'xxx';
      | 'wtu' 'rus' 'thb' 'hxf' 'ckh' 'xxx' 'xxx' 'xxx' 'xxx' 'xxx' 'xxx' 'xxx' 'xxx' 'xxx' 'xxx' 'xxx' 'xxx' 'xxx' 'xxx' 'xxx' 'xxx' 'xxx' 'xxx' 'xxx';
      | 'jsh' 'xkn' 'ulo' 'boa' 'ahv' 'xxx' 'xxx' 'xxx' 'xxx' 'xxx' 'xxx' 'xxx' 'xxx' 'xxx' 'xxx' 'xxx' 'xxx' 'xxx' 'xxx' 'xxx' 'xxx' 'xxx' 'xxx' 'xxx';
      | 'bbz' 'mwd' 'imq' 'xxx' 'xxx' 'xxx' 'xxx' 'xxx' 'xxx' 'xxx' 'xxx' 'xxx' 'xxx' 'xxx' 'xxx' 'xxx' 'xxx' 'xxx' 'xxx' 'xxx' 'xxx' 'xxx' 'xxx' 'xxx';
      | 'hpw' 'fft' 'tns' 'uge' 'xxx' 'xxx' 'xxx' 'xxx' 'xxx' 'xxx' 'xxx' 'xxx' 'xxx' 'xxx' 'xxx' 'xxx' 'xxx' 'xxx' 'xxx' 'xxx' 'xxx' 'xxx' 'xxx' 'xxx';
      | 'nbq' 'gcg' 'jui' 'zqy' 'xxx' 'xxx' 'xxx' 'xxx' 'xxx' 'xxx' 'xxx' 'xxx' 'xxx' 'xxx' 'xxx' 'xxx' 'xxx' 'xxx' 'xxx' 'xxx' 'xxx' 'xxx' 'xxx' 'xxx';
      | 'cel' 'fxp' 'dfl' 'xxx' 'xxx' 'xxx' 'xxx' 'xxx' 'xxx' 'xxx' 'xxx' 'xxx' 'xxx' 'xxx' 'xxx' 'xxx' 'xxx' 'xxx' 'xxx' 'xxx' 'xxx' 'xxx' 'xxx' 'xxx';
      | 'jrk' 'lsu' 'nki' 'wgx' 'xxx' 'xxx' 'xxx' 'xxx' 'xxx' 'xxx' 'xxx' 'xxx' 'xxx' 'xxx' 'xxx' 'xxx' 'xxx' 'xxx' 'xxx' 'xxx' 'xxx' 'xxx' 'xxx' 'xxx';
      | 'qzd' 'acm' 'yrt' 'qpo' 'xxx' 'xxx' 'xxx' 'xxx' 'xxx' 'xxx' 'xxx' 'xxx' 'xxx' 'xxx' 'xxx' 'xxx' 'xxx' 'xxx' 'xxx' 'xxx' 'xxx' 'xxx' 'xxx' 'xxx';
      | 'xcu' 'ain' 'xxx' 'xxx' 'xxx' 'xxx' 'xxx' 'xxx' 'xxx' 'xxx' 'xxx' 'xxx' 'xxx' 'xxx' 'xxx' 'xxx' 'xxx' 'xxx' 'xxx' 'xxx' 'xxx' 'xxx' 'xxx' 'xxx';
      | 'qxl' 'lur' 'igu' 'bsb' 'xxx' 'xxx' 'xxx' 'xxx' 'xxx' 'xxx' 'xxx' 'xxx' 'xxx' 'xxx' 'xxx' 'xxx' 'xxx' 'xxx' 'xxx' 'xxx' 'xxx' 'xxx' 'xxx' 'xxx';
      | 'pmu' 'xuk' 'dcl' 'ofd' 'xxx' 'xxx' 'xxx' 'xxx' 'xxx' 'xxx' 'xxx' 'xxx' 'xxx' 'xxx' 'xxx' 'xxx' 'xxx' 'xxx' 'xxx' 'xxx' 'xxx' 'xxx' 'xxx' 'xxx';
      | 'ahv' 'fbt' 'brg' 'xxx' 'xxx' 'xxx' 'xxx' 'xxx' 'xxx' 'xxx' 'xxx' 'xxx' 'xxx' 'xxx' 'xxx' 'xxx' 'xxx' 'xxx' 'xxx' 'xxx' 'xxx' 'xxx' 'xxx' 'xxx';
      | 'gtk' 'lgx' 'nrx' 'xxx' 'xxx' 'xxx' 'xxx' 'xxx' 'xxx' 'xxx' 'xxx' 'xxx' 'xxx' 'xxx' 'xxx' 'xxx' 'xxx' 'xxx' 'xxx' 'xxx' 'xxx' 'xxx' 'xxx' 'xxx';
      | 'vrt' 'yft' 'izj' 'uvk' 'cui' 'mfv' 'oil' 'myo' 'hzn' 'gwv' 'zlh' 'fqn' 'guw' 'vbp' 'wid' 'xhb' 'mvn' 'csd' 'itv' 'cvi' 'fyx' 'awl' 'xxx' 'xxx';
      | 'gcg' 'vrt' 'xxx' 'xxx' 'xxx' 'xxx' 'xxx' 'xxx' 'xxx' 'xxx' 'xxx' 'xxx' 'xxx' 'xxx' 'xxx' 'xxx' 'xxx' 'xxx' 'xxx' 'xxx' 'xxx' 'xxx' 'xxx' 'xxx';
      | 'ppm' 'bvv' 'zrw' 'vis' 'dcr' 'wck' 'ryr' 'gdh' 'tph' 'ucp' 'ejz' 'uuh' 'gep' 'xxx' 'xxx' 'xxx' 'xxx' 'xxx' 'xxx' 'xxx' 'xxx' 'xxx' 'xxx' 'xxx';
      | 'nel' 'ozd' 'fnr' 'xxx' 'xxx' 'xxx' 'xxx' 'xxx' 'xxx' 'xxx' 'xxx' 'xxx' 'xxx' 'xxx' 'xxx' 'xxx' 'xxx' 'xxx' 'xxx' 'xxx' 'xxx' 'xxx' 'xxx' 'xxx';
      | 'udl' 'out' 'xxx' 'xxx' 'xxx' 'xxx' 'xxx' 'xxx' 'xxx' 'xxx' 'xxx' 'xxx' 'xxx' 'xxx' 'xxx' 'xxx' 'xxx' 'xxx' 'xxx' 'xxx' 'xxx' 'xxx' 'xxx' 'xxx';
      | 'gkl' 'knq' 'txi' 'jmk' 'xee' 'xxx' 'xxx' 'xxx' 'xxx' 'xxx' 'xxx' 'xxx' 'xxx' 'xxx' 'xxx' 'xxx' 'xxx' 'xxx' 'xxx' 'xxx' 'xxx' 'xxx' 'xxx' 'xxx';
      | 'vvj' 'btp' 'pjc' 'wct' 'xxx' 'xxx' 'xxx' 'xxx' 'xxx' 'xxx' 'xxx' 'xxx' 'xxx' 'xxx' 'xxx' 'xxx' 'xxx' 'xxx' 'xxx' 'xxx' 'xxx' 'xxx' 'xxx' 'xxx';
      | 'adp' 'cxr' 'vtp' 'daz' 'poc' 'xxx' 'xxx' 'xxx' 'xxx' 'xxx' 'xxx' 'xxx' 'xxx' 'xxx' 'xxx' 'xxx' 'xxx' 'xxx' 'xxx' 'xxx' 'xxx' 'xxx' 'xxx' 'xxx';
      | 'zxj' 'jui' 'gcg' 'zqy' 'xxx' 'xxx' 'xxx' 'xxx' 'xxx' 'xxx' 'xxx' 'xxx' 'xxx' 'xxx' 'xxx' 'xxx' 'xxx' 'xxx' 'xxx' 'xxx' 'xxx' 'xxx' 'xxx' 'xxx';
      | 'dka' 'ifs' 'laq' 'qgn' 'jlg' 'xxx' 'xxx' 'xxx' 'xxx' 'xxx' 'xxx' 'xxx' 'xxx' 'xxx' 'xxx' 'xxx' 'xxx' 'xxx' 'xxx' 'xxx' 'xxx' 'xxx' 'xxx' 'xxx';
      | 'bhl' 'xpu' 'uos' 'xxx' 'xxx' 'xxx' 'xxx' 'xxx' 'xxx' 'xxx' 'xxx' 'xxx' 'xxx' 'xxx' 'xxx' 'xxx' 'xxx' 'xxx' 'xxx' 'xxx' 'xxx' 'xxx' 'xxx' 'xxx';
      | 'mzw' 'jmn' 'xfg' 'xxx' 'xxx' 'xxx' 'xxx' 'xxx' 'xxx' 'xxx' 'xxx' 'xxx' 'xxx' 'xxx' 'xxx' 'xxx' 'xxx' 'xxx' 'xxx' 'xxx' 'xxx' 'xxx' 'xxx' 'xxx';
      | 'ycr' 'qmf' 'hgq' 'szd' 'czt' 'xxx' 'xxx' 'xxx' 'xxx' 'xxx' 'xxx' 'xxx' 'xxx' 'xxx' 'xxx' 'xxx' 'xxx' 'xxx' 'xxx' 'xxx' 'xxx' 'xxx' 'xxx' 'xxx';
      | 'zfx' 'dbo' 'ain' 'scj' 'xxx' 'xxx' 'xxx' 'xxx' 'xxx' 'xxx' 'xxx' 'xxx' 'xxx' 'xxx' 'xxx' 'xxx' 'xxx' 'xxx' 'xxx' 'xxx' 'xxx' 'xxx' 'xxx' 'xxx';
      | 'jax' 'pbm' 'bxg' 'cel' 'cyc' 'hlo' 'xxx' 'xxx' 'xxx' 'xxx' 'xxx' 'xxx' 'xxx' 'xxx' 'xxx' 'xxx' 'xxx' 'xxx' 'xxx' 'xxx' 'xxx' 'xxx' 'xxx' 'xxx';
      | 'yqe' 'jnd' 'uqb' 'hrd' 'xxx' 'xxx' 'xxx' 'xxx' 'xxx' 'xxx' 'xxx' 'xxx' 'xxx' 'xxx' 'xxx' 'xxx' 'xxx' 'xxx' 'xxx' 'xxx' 'xxx' 'xxx' 'xxx' 'xxx';
      | 'lyd' 'dml' 'php' 'vin' 'obo' 'xxx' 'xxx' 'xxx' 'xxx' 'xxx' 'xxx' 'xxx' 'xxx' 'xxx' 'xxx' 'xxx' 'xxx' 'xxx' 'xxx' 'xxx' 'xxx' 'xxx' 'xxx' 'xxx';
      | 'euq' 'uoi' 'ece' 'xxx' 'xxx' 'xxx' 'xxx' 'xxx' 'xxx' 'xxx' 'xxx' 'xxx' 'xxx' 'xxx' 'xxx' 'xxx' 'xxx' 'xxx' 'xxx' 'xxx' 'xxx' 'xxx' 'xxx' 'xxx';
      | 'hzn' 'wct' 'xxx' 'xxx' 'xxx' 'xxx' 'xxx' 'xxx' 'xxx' 'xxx' 'xxx' 'xxx' 'xxx' 'xxx' 'xxx' 'xxx' 'xxx' 'xxx' 'xxx' 'xxx' 'xxx' 'xxx' 'xxx' 'xxx';
      | 'gwv' 'uut' 'tky' 'lte' 'xxx' 'xxx' 'xxx' 'xxx' 'xxx' 'xxx' 'xxx' 'xxx' 'xxx' 'xxx' 'xxx' 'xxx' 'xxx' 'xxx' 'xxx' 'xxx' 'xxx' 'xxx' 'xxx' 'xxx';
      | 'wgx' 'sta' 'xee' 'knq' 'xxx' 'xxx' 'xxx' 'xxx' 'xxx' 'xxx' 'xxx' 'xxx' 'xxx' 'xxx' 'xxx' 'xxx' 'xxx' 'xxx' 'xxx' 'xxx' 'xxx' 'xxx' 'xxx' 'xxx';
      | 'xhd' 'phh' 'ael' 'xxx' 'xxx' 'xxx' 'xxx' 'xxx' 'xxx' 'xxx' 'xxx' 'xxx' 'xxx' 'xxx' 'xxx' 'xxx' 'xxx' 'xxx' 'xxx' 'xxx' 'xxx' 'xxx' 'xxx' 'xxx';
      | 'axk' 'tcu' 'uqb' 'xxx' 'xxx' 'xxx' 'xxx' 'xxx' 'xxx' 'xxx' 'xxx' 'xxx' 'xxx' 'xxx' 'xxx' 'xxx' 'xxx' 'xxx' 'xxx' 'xxx' 'xxx' 'xxx' 'xxx' 'xxx';
      | 'ece' 'sgu' 'fbt' 'xxx' 'xxx' 'xxx' 'xxx' 'xxx' 'xxx' 'xxx' 'xxx' 'xxx' 'xxx' 'xxx' 'xxx' 'xxx' 'xxx' 'xxx' 'xxx' 'xxx' 'xxx' 'xxx' 'xxx' 'xxx';
      | 'waa' 'jaa' 'xxx' 'xxx' 'xxx' 'xxx' 'xxx' 'xxx' 'xxx' 'xxx' 'xxx' 'xxx' 'xxx' 'xxx' 'xxx' 'xxx' 'xxx' 'xxx' 'xxx' 'xxx' 'xxx' 'xxx' 'xxx' 'xxx';
      | 'jaa' 'ftq' 'lup' 'awp' 'xxx' 'xxx' 'xxx' 'xxx' 'xxx' 'xxx' 'xxx' 'xxx' 'xxx' 'xxx' 'xxx' 'xxx' 'xxx' 'xxx' 'xxx' 'xxx' 'xxx' 'xxx' 'xxx' 'xxx';
      | 'cje' 'xmq' 'pvm' 'xxx' 'xxx' 'xxx' 'xxx' 'xxx' 'xxx' 'xxx' 'xxx' 'xxx' 'xxx' 'xxx' 'xxx' 'xxx' 'xxx' 'xxx' 'xxx' 'xxx' 'xxx' 'xxx' 'xxx' 'xxx';
      | 'lln' 'bbz' 'qff' 'dkw' 'paz' 'htf' 'fhv' 'vrp' 'jkx' 'ihm' 'bud' 'jef' 'eej' 'xxx' 'xxx' 'xxx' 'xxx' 'xxx' 'xxx' 'xxx' 'xxx' 'xxx' 'xxx' 'xxx';
      | 'bvs' 'pbm' 'cel' 'xxx' 'xxx' 'xxx' 'xxx' 'xxx' 'xxx' 'xxx' 'xxx' 'xxx' 'xxx' 'xxx' 'xxx' 'xxx' 'xxx' 'xxx' 'xxx' 'xxx' 'xxx' 'xxx' 'xxx' 'xxx';
      | 'zow' 'xay' 'wxl' 'xxx' 'xxx' 'xxx' 'xxx' 'xxx' 'xxx' 'xxx' 'xxx' 'xxx' 'xxx' 'xxx' 'xxx' 'xxx' 'xxx' 'xxx' 'xxx' 'xxx' 'xxx' 'xxx' 'xxx' 'xxx';
      | 'pvm' 'fnr' 'you' 'vrt' 'ozd' 'xxx' 'xxx' 'xxx' 'xxx' 'xxx' 'xxx' 'xxx' 'xxx' 'xxx' 'xxx' 'xxx' 'xxx' 'xxx' 'xxx' 'xxx' 'xxx' 'xxx' 'xxx' 'xxx';
      | 'dbo' 'knu' 'xxx' 'xxx' 'xxx' 'xxx' 'xxx' 'xxx' 'xxx' 'xxx' 'xxx' 'xxx' 'xxx' 'xxx' 'xxx' 'xxx' 'xxx' 'xxx' 'xxx' 'xxx' 'xxx' 'xxx' 'xxx' 'xxx';
      | 'vbc' 'pld' 'xxx' 'xxx' 'xxx' 'xxx' 'xxx' 'xxx' 'xxx' 'xxx' 'xxx' 'xxx' 'xxx' 'xxx' 'xxx' 'xxx' 'xxx' 'xxx' 'xxx' 'xxx' 'xxx' 'xxx' 'xxx' 'xxx';
      | 'xpp' 'iwh' 'qzd' 'gye' 'xxx' 'xxx' 'xxx' 'xxx' 'xxx' 'xxx' 'xxx' 'xxx' 'xxx' 'xxx' 'xxx' 'xxx' 'xxx' 'xxx' 'xxx' 'xxx' 'xxx' 'xxx' 'xxx' 'xxx';
      | 'gep' 'fdl' 'xxx' 'xxx' 'xxx' 'xxx' 'xxx' 'xxx' 'xxx' 'xxx' 'xxx' 'xxx' 'xxx' 'xxx' 'xxx' 'xxx' 'xxx' 'xxx' 'xxx' 'xxx' 'xxx' 'xxx' 'xxx' 'xxx';
      | 'qqj' 'xhk' 'bsb' 'lur' 'fpb' 'xxx' 'xxx' 'xxx' 'xxx' 'xxx' 'xxx' 'xxx' 'xxx' 'xxx' 'xxx' 'xxx' 'xxx' 'xxx' 'xxx' 'xxx' 'xxx' 'xxx' 'xxx' 'xxx';
      | 'wpo' 'fdg' 'xxx' 'xxx' 'xxx' 'xxx' 'xxx' 'xxx' 'xxx' 'xxx' 'xxx' 'xxx' 'xxx' 'xxx' 'xxx' 'xxx' 'xxx' 'xxx' 'xxx' 'xxx' 'xxx' 'xxx' 'xxx' 'xxx';
      | 'qgy' 'sid' 'qgh' 'xxx' 'xxx' 'xxx' 'xxx' 'xxx' 'xxx' 'xxx' 'xxx' 'xxx' 'xxx' 'xxx' 'xxx' 'xxx' 'xxx' 'xxx' 'xxx' 'xxx' 'xxx' 'xxx' 'xxx' 'xxx';
      | 'dne' 'oag' 'def' 'xxx' 'xxx' 'xxx' 'xxx' 'xxx' 'xxx' 'xxx' 'xxx' 'xxx' 'xxx' 'xxx' 'xxx' 'xxx' 'xxx' 'xxx' 'xxx' 'xxx' 'xxx' 'xxx' 'xxx' 'xxx';
      | 'oap' 'igu' 'lur' 'bsb' 'xhk' 'xxx' 'xxx' 'xxx' 'xxx' 'xxx' 'xxx' 'xxx' 'xxx' 'xxx' 'xxx' 'xxx' 'xxx' 'xxx' 'xxx' 'xxx' 'xxx' 'xxx' 'xxx' 'xxx';
      | 'bee' 'oxm' 'uji' 'tpb' 'jgf' 'xxx' 'xxx' 'xxx' 'xxx' 'xxx' 'xxx' 'xxx' 'xxx' 'xxx' 'xxx' 'xxx' 'xxx' 'xxx' 'xxx' 'xxx' 'xxx' 'xxx' 'xxx' 'xxx';
      | 'dxd' 'rus' 'thb' 'xxx' 'xxx' 'xxx' 'xxx' 'xxx' 'xxx' 'xxx' 'xxx' 'xxx' 'xxx' 'xxx' 'xxx' 'xxx' 'xxx' 'xxx' 'xxx' 'xxx' 'xxx' 'xxx' 'xxx' 'xxx';
      | 'mjp' 'jgf' 'mkp' 'xxx' 'xxx' 'xxx' 'xxx' 'xxx' 'xxx' 'xxx' 'xxx' 'xxx' 'xxx' 'xxx' 'xxx' 'xxx' 'xxx' 'xxx' 'xxx' 'xxx' 'xxx' 'xxx' 'xxx' 'xxx';
      | 'ytc' 'brg' 'yql' 'sgu' 'fbt' 'xxx' 'xxx' 'xxx' 'xxx' 'xxx' 'xxx' 'xxx' 'xxx' 'xxx' 'xxx' 'xxx' 'xxx' 'xxx' 'xxx' 'xxx' 'xxx' 'xxx' 'xxx' 'xxx';
      | 'zlh' 'krd' 'kvi' 'rhq' 'xxx' 'xxx' 'xxx' 'xxx' 'xxx' 'xxx' 'xxx' 'xxx' 'xxx' 'xxx' 'xxx' 'xxx' 'xxx' 'xxx' 'xxx' 'xxx' 'xxx' 'xxx' 'xxx' 'xxx';
      | 'wcx' 'def' 'oag' 'rtp' 'xxx' 'xxx' 'xxx' 'xxx' 'xxx' 'xxx' 'xxx' 'xxx' 'xxx' 'xxx' 'xxx' 'xxx' 'xxx' 'xxx' 'xxx' 'xxx' 'xxx' 'xxx' 'xxx' 'xxx';
      | 'svr' 'qlv' 'lln' 'qwc' 'xxx' 'xxx' 'xxx' 'xxx' 'xxx' 'xxx' 'xxx' 'xxx' 'xxx' 'xxx' 'xxx' 'xxx' 'xxx' 'xxx' 'xxx' 'xxx' 'xxx' 'xxx' 'xxx' 'xxx';
      | 'ola' 'sta' 'xee' 'jmk' 'txi' 'xxx' 'xxx' 'xxx' 'xxx' 'xxx' 'xxx' 'xxx' 'xxx' 'xxx' 'xxx' 'xxx' 'xxx' 'xxx' 'xxx' 'xxx' 'xxx' 'xxx' 'xxx' 'xxx';
      | 'qwc' 'jkx' 'ihm' 'nww' 'sbi' 'bud' 'fed' 'jef' 'eej' 'bbz' 'qff' 'nfj' 'paz' 'fhv' 'vrp' 'wdr' 'xxx' 'xxx' 'xxx' 'xxx' 'xxx' 'xxx' 'xxx' 'xxx';
      | 'gce' 'kzl' 'ogv' 'xxx' 'xxx' 'xxx' 'xxx' 'xxx' 'xxx' 'xxx' 'xxx' 'xxx' 'xxx' 'xxx' 'xxx' 'xxx' 'xxx' 'xxx' 'xxx' 'xxx' 'xxx' 'xxx' 'xxx' 'xxx';
      | 'uxn' 'phi' 'bcz' 'xxx' 'xxx' 'xxx' 'xxx' 'xxx' 'xxx' 'xxx' 'xxx' 'xxx' 'xxx' 'xxx' 'xxx' 'xxx' 'xxx' 'xxx' 'xxx' 'xxx' 'xxx' 'xxx' 'xxx' 'xxx';
      | 'vnd' 'fbt' 'brg' 'xxx' 'xxx' 'xxx' 'xxx' 'xxx' 'xxx' 'xxx' 'xxx' 'xxx' 'xxx' 'xxx' 'xxx' 'xxx' 'xxx' 'xxx' 'xxx' 'xxx' 'xxx' 'xxx' 'xxx' 'xxx';
      | 'xee' 'uni' 'hkq' 'ljy' 'qlf' 'aeo' 'xxx' 'xxx' 'xxx' 'xxx' 'xxx' 'xxx' 'xxx' 'xxx' 'xxx' 'xxx' 'xxx' 'xxx' 'xxx' 'xxx' 'xxx' 'xxx' 'xxx' 'xxx';
      | 'zaz' 'cmi' 'xxx' 'xxx' 'xxx' 'xxx' 'xxx' 'xxx' 'xxx' 'xxx' 'xxx' 'xxx' 'xxx' 'xxx' 'xxx' 'xxx' 'xxx' 'xxx' 'xxx' 'xxx' 'xxx' 'xxx' 'xxx' 'xxx';
      | 'gpt' 'yfw' 'xxx' 'xxx' 'xxx' 'xxx' 'xxx' 'xxx' 'xxx' 'xxx' 'xxx' 'xxx' 'xxx' 'xxx' 'xxx' 'xxx' 'xxx' 'xxx' 'xxx' 'xxx' 'xxx' 'xxx' 'xxx' 'xxx';
      | 'dkm' 'gaq' 'fac' 'aaj' 'zaq' 'xxx' 'xxx' 'xxx' 'xxx' 'xxx' 'xxx' 'xxx' 'xxx' 'xxx' 'xxx' 'xxx' 'xxx' 'xxx' 'xxx' 'xxx' 'xxx' 'xxx' 'xxx' 'xxx';
      | 'kjq' 'sgy' 'xxx' 'xxx' 'xxx' 'xxx' 'xxx' 'xxx' 'xxx' 'xxx' 'xxx' 'xxx' 'xxx' 'xxx' 'xxx' 'xxx' 'xxx' 'xxx' 'xxx' 'xxx' 'xxx' 'xxx' 'xxx' 'xxx';
      | 'oba' 'qgn' 'jlg' 'xxx' 'xxx' 'xxx' 'xxx' 'xxx' 'xxx' 'xxx' 'xxx' 'xxx' 'xxx' 'xxx' 'xxx' 'xxx' 'xxx' 'xxx' 'xxx' 'xxx' 'xxx' 'xxx' 'xxx' 'xxx';
      | 'slg' 'dir' 'xxx' 'xxx' 'xxx' 'xxx' 'xxx' 'xxx' 'xxx' 'xxx' 'xxx' 'xxx' 'xxx' 'xxx' 'xxx' 'xxx' 'xxx' 'xxx' 'xxx' 'xxx' 'xxx' 'xxx' 'xxx' 'xxx';
      | 'fvb' 'xhk' 'bsb' 'igu' 'lur' 'xxx' 'xxx' 'xxx' 'xxx' 'xxx' 'xxx' 'xxx' 'xxx' 'xxx' 'xxx' 'xxx' 'xxx' 'xxx' 'xxx' 'xxx' 'xxx' 'xxx' 'xxx' 'xxx';
      | 'csd' 'gpt' 'otp' 'qwo' 'xxx' 'xxx' 'xxx' 'xxx' 'xxx' 'xxx' 'xxx' 'xxx' 'xxx' 'xxx' 'xxx' 'xxx' 'xxx' 'xxx' 'xxx' 'xxx' 'xxx' 'xxx' 'xxx' 'xxx';
      | 'kkp' 'dij' 'pbf' 'xxx' 'xxx' 'xxx' 'xxx' 'xxx' 'xxx' 'xxx' 'xxx' 'xxx' 'xxx' 'xxx' 'xxx' 'xxx' 'xxx' 'xxx' 'xxx' 'xxx' 'xxx' 'xxx' 'xxx' 'xxx';
      | 'osk' 'xpp' 'rys' 'xxx' 'xxx' 'xxx' 'xxx' 'xxx' 'xxx' 'xxx' 'xxx' 'xxx' 'xxx' 'xxx' 'xxx' 'xxx' 'xxx' 'xxx' 'xxx' 'xxx' 'xxx' 'xxx' 'xxx' 'xxx';
      | 'hmf' 'pde' 'luh' 'dkm' 'xxx' 'xxx' 'xxx' 'xxx' 'xxx' 'xxx' 'xxx' 'xxx' 'xxx' 'xxx' 'xxx' 'xxx' 'xxx' 'xxx' 'xxx' 'xxx' 'xxx' 'xxx' 'xxx' 'xxx';
      | 'uwn' 'lkd' 'xxx' 'xxx' 'xxx' 'xxx' 'xxx' 'xxx' 'xxx' 'xxx' 'xxx' 'xxx' 'xxx' 'xxx' 'xxx' 'xxx' 'xxx' 'xxx' 'xxx' 'xxx' 'xxx' 'xxx' 'xxx' 'xxx';
      | 'crd' 'ikt' 'hnn' 'fzl' 'xxx' 'xxx' 'xxx' 'xxx' 'xxx' 'xxx' 'xxx' 'xxx' 'xxx' 'xxx' 'xxx' 'xxx' 'xxx' 'xxx' 'xxx' 'xxx' 'xxx' 'xxx' 'xxx' 'xxx';
      | 'acm' 'jlg' 'qgn' 'laq' 'xxx' 'xxx' 'xxx' 'xxx' 'xxx' 'xxx' 'xxx' 'xxx' 'xxx' 'xxx' 'xxx' 'xxx' 'xxx' 'xxx' 'xxx' 'xxx' 'xxx' 'xxx' 'xxx' 'xxx';
      | 'utb' 'fnr' 'mwu' 'you' 'xxx' 'xxx' 'xxx' 'xxx' 'xxx' 'xxx' 'xxx' 'xxx' 'xxx' 'xxx' 'xxx' 'xxx' 'xxx' 'xxx' 'xxx' 'xxx' 'xxx' 'xxx' 'xxx' 'xxx';
      | 'lcp' 'rbi' 'xxx' 'xxx' 'xxx' 'xxx' 'xxx' 'xxx' 'xxx' 'xxx' 'xxx' 'xxx' 'xxx' 'xxx' 'xxx' 'xxx' 'xxx' 'xxx' 'xxx' 'xxx' 'xxx' 'xxx' 'xxx' 'xxx';
      | 'mby' 'out' 'xxx' 'xxx' 'xxx' 'xxx' 'xxx' 'xxx' 'xxx' 'xxx' 'xxx' 'xxx' 'xxx' 'xxx' 'xxx' 'xxx' 'xxx' 'xxx' 'xxx' 'xxx' 'xxx' 'xxx' 'xxx' 'xxx';
      | 'fbt' 'tbn' 'iiu' 'uxu' 'sdr' 'wyl' 'uwn' 'xao' 'ltv' 'wpo' 'mjy' 'xso' 'xxx' 'xxx' 'xxx' 'xxx' 'xxx' 'xxx' 'xxx' 'xxx' 'xxx' 'xxx' 'xxx' 'xxx';
      | 'fhq' 'ynz' 'mjp' 'xxx' 'xxx' 'xxx' 'xxx' 'xxx' 'xxx' 'xxx' 'xxx' 'xxx' 'xxx' 'xxx' 'xxx' 'xxx' 'xxx' 'xxx' 'xxx' 'xxx' 'xxx' 'xxx' 'xxx' 'xxx';
      | 'qhx' 'ahv' 'boa' 'ulo' 'jai' 'xxx' 'xxx' 'xxx' 'xxx' 'xxx' 'xxx' 'xxx' 'xxx' 'xxx' 'xxx' 'xxx' 'xxx' 'xxx' 'xxx' 'xxx' 'xxx' 'xxx' 'xxx' 'xxx';
      | 'wpn' 'bpo' 'xxx' 'xxx' 'xxx' 'xxx' 'xxx' 'xxx' 'xxx' 'xxx' 'xxx' 'xxx' 'xxx' 'xxx' 'xxx' 'xxx' 'xxx' 'xxx' 'xxx' 'xxx' 'xxx' 'xxx' 'xxx' 'xxx';
      | 'xbk' 'mby' 'xxx' 'xxx' 'xxx' 'xxx' 'xxx' 'xxx' 'xxx' 'xxx' 'xxx' 'xxx' 'xxx' 'xxx' 'xxx' 'xxx' 'xxx' 'xxx' 'xxx' 'xxx' 'xxx' 'xxx' 'xxx' 'xxx';
      | 'axi' 'out' 'xxx' 'xxx' 'xxx' 'xxx' 'xxx' 'xxx' 'xxx' 'xxx' 'xxx' 'xxx' 'xxx' 'xxx' 'xxx' 'xxx' 'xxx' 'xxx' 'xxx' 'xxx' 'xxx' 'xxx' 'xxx' 'xxx';
      | 'rbi' 'yxq' 'bnw' 'xxx' 'xxx' 'xxx' 'xxx' 'xxx' 'xxx' 'xxx' 'xxx' 'xxx' 'xxx' 'xxx' 'xxx' 'xxx' 'xxx' 'xxx' 'xxx' 'xxx' 'xxx' 'xxx' 'xxx' 'xxx';
      | 'dcr' 'fjm' 'xxx' 'xxx' 'xxx' 'xxx' 'xxx' 'xxx' 'xxx' 'xxx' 'xxx' 'xxx' 'xxx' 'xxx' 'xxx' 'xxx' 'xxx' 'xxx' 'xxx' 'xxx' 'xxx' 'xxx' 'xxx' 'xxx';
      | 'nxs' 'gkf' 'cuk' 'qcj' 'xxx' 'xxx' 'xxx' 'xxx' 'xxx' 'xxx' 'xxx' 'xxx' 'xxx' 'xxx' 'xxx' 'xxx' 'xxx' 'xxx' 'xxx' 'xxx' 'xxx' 'xxx' 'xxx' 'xxx';
      | 'rxn' 'uwp' 'jhu' 'lra' 'ltm' 'xxx' 'xxx' 'xxx' 'xxx' 'xxx' 'xxx' 'xxx' 'xxx' 'xxx' 'xxx' 'xxx' 'xxx' 'xxx' 'xxx' 'xxx' 'xxx' 'xxx' 'xxx' 'xxx';
      | 'kez' 'ifs' 'xxx' 'xxx' 'xxx' 'xxx' 'xxx' 'xxx' 'xxx' 'xxx' 'xxx' 'xxx' 'xxx' 'xxx' 'xxx' 'xxx' 'xxx' 'xxx' 'xxx' 'xxx' 'xxx' 'xxx' 'xxx' 'xxx';
      | 'ikt' 'xhk' 'bsb' 'igu' 'fpb' 'xxx' 'xxx' 'xxx' 'xxx' 'xxx' 'xxx' 'xxx' 'xxx' 'xxx' 'xxx' 'xxx' 'xxx' 'xxx' 'xxx' 'xxx' 'xxx' 'xxx' 'xxx' 'xxx';
      | 'nhf' 'pje' 'xxx' 'xxx' 'xxx' 'xxx' 'xxx' 'xxx' 'xxx' 'xxx' 'xxx' 'xxx' 'xxx' 'xxx' 'xxx' 'xxx' 'xxx' 'xxx' 'xxx' 'xxx' 'xxx' 'xxx' 'xxx' 'xxx';
      | 'lsu' 'xee' 'sta' 'jmk' 'xxx' 'xxx' 'xxx' 'xxx' 'xxx' 'xxx' 'xxx' 'xxx' 'xxx' 'xxx' 'xxx' 'xxx' 'xxx' 'xxx' 'xxx' 'xxx' 'xxx' 'xxx' 'xxx' 'xxx';
      | 'ejp' 'oba' 'aaj' 'gaq' 'xxx' 'xxx' 'xxx' 'xxx' 'xxx' 'xxx' 'xxx' 'xxx' 'xxx' 'xxx' 'xxx' 'xxx' 'xxx' 'xxx' 'xxx' 'xxx' 'xxx' 'xxx' 'xxx' 'xxx';
      | 'tph' 'rnk' 'brb' 'xxx' 'xxx' 'xxx' 'xxx' 'xxx' 'xxx' 'xxx' 'xxx' 'xxx' 'xxx' 'xxx' 'xxx' 'xxx' 'xxx' 'xxx' 'xxx' 'xxx' 'xxx' 'xxx' 'xxx' 'xxx';
      | 'bpo' 'wmr' 'euq' 'xxx' 'xxx' 'xxx' 'xxx' 'xxx' 'xxx' 'xxx' 'xxx' 'xxx' 'xxx' 'xxx' 'xxx' 'xxx' 'xxx' 'xxx' 'xxx' 'xxx' 'xxx' 'xxx' 'xxx' 'xxx';
      | 'ybr' 'uhn' 'cqf' 'xxx' 'xxx' 'xxx' 'xxx' 'xxx' 'xxx' 'xxx' 'xxx' 'xxx' 'xxx' 'xxx' 'xxx' 'xxx' 'xxx' 'xxx' 'xxx' 'xxx' 'xxx' 'xxx' 'xxx' 'xxx';
      | 'pde' 'gaq' 'xxx' 'xxx' 'xxx' 'xxx' 'xxx' 'xxx' 'xxx' 'xxx' 'xxx' 'xxx' 'xxx' 'xxx' 'xxx' 'xxx' 'xxx' 'xxx' 'xxx' 'xxx' 'xxx' 'xxx' 'xxx' 'xxx';
      | 'kbp' 'xhk' 'bsb' 'xxx' 'xxx' 'xxx' 'xxx' 'xxx' 'xxx' 'xxx' 'xxx' 'xxx' 'xxx' 'xxx' 'xxx' 'xxx' 'xxx' 'xxx' 'xxx' 'xxx' 'xxx' 'xxx' 'xxx' 'xxx';
      | 'fhv' 'pxk' 'htw' 'xxx' 'xxx' 'xxx' 'xxx' 'xxx' 'xxx' 'xxx' 'xxx' 'xxx' 'xxx' 'xxx' 'xxx' 'xxx' 'xxx' 'xxx' 'xxx' 'xxx' 'xxx' 'xxx' 'xxx' 'xxx';
      | 'lkd' 'bda' 'mkd' 'agn' 'bhh' 'xxx' 'xxx' 'xxx' 'xxx' 'xxx' 'xxx' 'xxx' 'xxx' 'xxx' 'xxx' 'xxx' 'xxx' 'xxx' 'xxx' 'xxx' 'xxx' 'xxx' 'xxx' 'xxx';
      | 'fmr' 'shb' 'wtu' 'kul' 'xxx' 'xxx' 'xxx' 'xxx' 'xxx' 'xxx' 'xxx' 'xxx' 'xxx' 'xxx' 'xxx' 'xxx' 'xxx' 'xxx' 'xxx' 'xxx' 'xxx' 'xxx' 'xxx' 'xxx';
      | 'ftm' 'ozd' 'vrt' 'xxx' 'xxx' 'xxx' 'xxx' 'xxx' 'xxx' 'xxx' 'xxx' 'xxx' 'xxx' 'xxx' 'xxx' 'xxx' 'xxx' 'xxx' 'xxx' 'xxx' 'xxx' 'xxx' 'xxx' 'xxx';
      | 'aeo' 'szd' 'qmf' 'hgq' 'xxx' 'xxx' 'xxx' 'xxx' 'xxx' 'xxx' 'xxx' 'xxx' 'xxx' 'xxx' 'xxx' 'xxx' 'xxx' 'xxx' 'xxx' 'xxx' 'xxx' 'xxx' 'xxx' 'xxx';
      | 'dhu' 'ogv' 'apv' 'vbc' 'kzl' 'xxx' 'xxx' 'xxx' 'xxx' 'xxx' 'xxx' 'xxx' 'xxx' 'xxx' 'xxx' 'xxx' 'xxx' 'xxx' 'xxx' 'xxx' 'xxx' 'xxx' 'xxx' 'xxx';
      | 'irh' 'mpj' 'ysr' 'qxl' 'xxx' 'xxx' 'xxx' 'xxx' 'xxx' 'xxx' 'xxx' 'xxx' 'xxx' 'xxx' 'xxx' 'xxx' 'xxx' 'xxx' 'xxx' 'xxx' 'xxx' 'xxx' 'xxx' 'xxx';
      | 'thp' 'you' 'ozd' 'vrt' 'xxx' 'xxx' 'xxx' 'xxx' 'xxx' 'xxx' 'xxx' 'xxx' 'xxx' 'xxx' 'xxx' 'xxx' 'xxx' 'xxx' 'xxx' 'xxx' 'xxx' 'xxx' 'xxx' 'xxx';
      | 'bda' 'alh' 'jly' 'ola' 'zcf' 'giz' 'xxx' 'xxx' 'xxx' 'xxx' 'xxx' 'xxx' 'xxx' 'xxx' 'xxx' 'xxx' 'xxx' 'xxx' 'xxx' 'xxx' 'xxx' 'xxx' 'xxx' 'xxx';
      | 'uzw' 'laq' 'ifs' 'qgn' 'xxx' 'xxx' 'xxx' 'xxx' 'xxx' 'xxx' 'xxx' 'xxx' 'xxx' 'xxx' 'xxx' 'xxx' 'xxx' 'xxx' 'xxx' 'xxx' 'xxx' 'xxx' 'xxx' 'xxx';
      | 'scb' 'bsb' 'xxx' 'xxx' 'xxx' 'xxx' 'xxx' 'xxx' 'xxx' 'xxx' 'xxx' 'xxx' 'xxx' 'xxx' 'xxx' 'xxx' 'xxx' 'xxx' 'xxx' 'xxx' 'xxx' 'xxx' 'xxx' 'xxx';
      | 'aeb' 'wbs' 'hhu' 'nel' 'utb' 'xxx' 'xxx' 'xxx' 'xxx' 'xxx' 'xxx' 'xxx' 'xxx' 'xxx' 'xxx' 'xxx' 'xxx' 'xxx' 'xxx' 'xxx' 'xxx' 'xxx' 'xxx' 'xxx';
      | 'vin' 'brg' 'xxx' 'xxx' 'xxx' 'xxx' 'xxx' 'xxx' 'xxx' 'xxx' 'xxx' 'xxx' 'xxx' 'xxx' 'xxx' 'xxx' 'xxx' 'xxx' 'xxx' 'xxx' 'xxx' 'xxx' 'xxx' 'xxx';
      | 'rnk' 'fan' 'xxx' 'xxx' 'xxx' 'xxx' 'xxx' 'xxx' 'xxx' 'xxx' 'xxx' 'xxx' 'xxx' 'xxx' 'xxx' 'xxx' 'xxx' 'xxx' 'xxx' 'xxx' 'xxx' 'xxx' 'xxx' 'xxx';
      | 'sid' 'jwy' 'fmr' 'irm' 'xxx' 'xxx' 'xxx' 'xxx' 'xxx' 'xxx' 'xxx' 'xxx' 'xxx' 'xxx' 'xxx' 'xxx' 'xxx' 'xxx' 'xxx' 'xxx' 'xxx' 'xxx' 'xxx' 'xxx';
      | 'uxu' 'slg' 'mli' 'vim' 'srf' 'xxx' 'xxx' 'xxx' 'xxx' 'xxx' 'xxx' 'xxx' 'xxx' 'xxx' 'xxx' 'xxx' 'xxx' 'xxx' 'xxx' 'xxx' 'xxx' 'xxx' 'xxx' 'xxx';
      | 'anr' 'yba' 'puu' 'zaz' 'xxx' 'xxx' 'xxx' 'xxx' 'xxx' 'xxx' 'xxx' 'xxx' 'xxx' 'xxx' 'xxx' 'xxx' 'xxx' 'xxx' 'xxx' 'xxx' 'xxx' 'xxx' 'xxx' 'xxx';
      | 'kbq' 'rys' 'xxx' 'xxx' 'xxx' 'xxx' 'xxx' 'xxx' 'xxx' 'xxx' 'xxx' 'xxx' 'xxx' 'xxx' 'xxx' 'xxx' 'xxx' 'xxx' 'xxx' 'xxx' 'xxx' 'xxx' 'xxx' 'xxx';
      | 'jwl' 'igh' 'xxx' 'xxx' 'xxx' 'xxx' 'xxx' 'xxx' 'xxx' 'xxx' 'xxx' 'xxx' 'xxx' 'xxx' 'xxx' 'xxx' 'xxx' 'xxx' 'xxx' 'xxx' 'xxx' 'xxx' 'xxx' 'xxx';
      | 'vis' 'amv' 'hpw' 'gte' 'qwd' 'xxx' 'xxx' 'xxx' 'xxx' 'xxx' 'xxx' 'xxx' 'xxx' 'xxx' 'xxx' 'xxx' 'xxx' 'xxx' 'xxx' 'xxx' 'xxx' 'xxx' 'xxx' 'xxx';
      | 'fer' 'lkv' 'wby' 'rdm' 'bqy' 'ftm' 'xxx' 'xxx' 'xxx' 'xxx' 'xxx' 'xxx' 'xxx' 'xxx' 'xxx' 'xxx' 'xxx' 'xxx' 'xxx' 'xxx' 'xxx' 'xxx' 'xxx' 'xxx';
      | 'kwv' 'ola' 'jly' 'zcf' 'xxx' 'xxx' 'xxx' 'xxx' 'xxx' 'xxx' 'xxx' 'xxx' 'xxx' 'xxx' 'xxx' 'xxx' 'xxx' 'xxx' 'xxx' 'xxx' 'xxx' 'xxx' 'xxx' 'xxx';
      | 'nac' 'lur' 'xxx' 'xxx' 'xxx' 'xxx' 'xxx' 'xxx' 'xxx' 'xxx' 'xxx' 'xxx' 'xxx' 'xxx' 'xxx' 'xxx' 'xxx' 'xxx' 'xxx' 'xxx' 'xxx' 'xxx' 'xxx' 'xxx';
      | 'xvu' 'phc' 'irh' 'xxx' 'xxx' 'xxx' 'xxx' 'xxx' 'xxx' 'xxx' 'xxx' 'xxx' 'xxx' 'xxx' 'xxx' 'xxx' 'xxx' 'xxx' 'xxx' 'xxx' 'xxx' 'xxx' 'xxx' 'xxx';
      | 'luh' 'aaj' 'zaq' 'oba' 'gaq' 'xxx' 'xxx' 'xxx' 'xxx' 'xxx' 'xxx' 'xxx' 'xxx' 'xxx' 'xxx' 'xxx' 'xxx' 'xxx' 'xxx' 'xxx' 'xxx' 'xxx' 'xxx' 'xxx';
      | 'bcq' 'fbt' 'sgu' 'brg' 'yql' 'xxx' 'xxx' 'xxx' 'xxx' 'xxx' 'xxx' 'xxx' 'xxx' 'xxx' 'xxx' 'xxx' 'xxx' 'xxx' 'xxx' 'xxx' 'xxx' 'xxx' 'xxx' 'xxx';
      | 'puu' 'bvq' 'xbk' 'xxx' 'xxx' 'xxx' 'xxx' 'xxx' 'xxx' 'xxx' 'xxx' 'xxx' 'xxx' 'xxx' 'xxx' 'xxx' 'xxx' 'xxx' 'xxx' 'xxx' 'xxx' 'xxx' 'xxx' 'xxx';
      | 'mei' 'rjp' 'ytc' 'vnd' 'xxx' 'xxx' 'xxx' 'xxx' 'xxx' 'xxx' 'xxx' 'xxx' 'xxx' 'xxx' 'xxx' 'xxx' 'xxx' 'xxx' 'xxx' 'xxx' 'xxx' 'xxx' 'xxx' 'xxx';
      | 'lyf' 'igu' 'xhk' 'bsb' 'xxx' 'xxx' 'xxx' 'xxx' 'xxx' 'xxx' 'xxx' 'xxx' 'xxx' 'xxx' 'xxx' 'xxx' 'xxx' 'xxx' 'xxx' 'xxx' 'xxx' 'xxx' 'xxx' 'xxx';
      | 'tmc' 'fbt' 'xxx' 'xxx' 'xxx' 'xxx' 'xxx' 'xxx' 'xxx' 'xxx' 'xxx' 'xxx' 'xxx' 'xxx' 'xxx' 'xxx' 'xxx' 'xxx' 'xxx' 'xxx' 'xxx' 'xxx' 'xxx' 'xxx';
      | 'suv' 'rzo' 'dzp' 'qig' 'bhl' 'xxx' 'xxx' 'xxx' 'xxx' 'xxx' 'xxx' 'xxx' 'xxx' 'xxx' 'xxx' 'xxx' 'xxx' 'xxx' 'xxx' 'xxx' 'xxx' 'xxx' 'xxx' 'xxx';
      | 'qwo' 'anr' 'xxx' 'xxx' 'xxx' 'xxx' 'xxx' 'xxx' 'xxx' 'xxx' 'xxx' 'xxx' 'xxx' 'xxx' 'xxx' 'xxx' 'xxx' 'xxx' 'xxx' 'xxx' 'xxx' 'xxx' 'xxx' 'xxx';
      | 'uuh' 'iur' 'xxx' 'xxx' 'xxx' 'xxx' 'xxx' 'xxx' 'xxx' 'xxx' 'xxx' 'xxx' 'xxx' 'xxx' 'xxx' 'xxx' 'xxx' 'xxx' 'xxx' 'xxx' 'xxx' 'xxx' 'xxx' 'xxx';
      | 'dfl' 'mzo' 'vii' 'xxx' 'xxx' 'xxx' 'xxx' 'xxx' 'xxx' 'xxx' 'xxx' 'xxx' 'xxx' 'xxx' 'xxx' 'xxx' 'xxx' 'xxx' 'xxx' 'xxx' 'xxx' 'xxx' 'xxx' 'xxx';
      | 'hrd' 'esz' 'wua' 'xxx' 'xxx' 'xxx' 'xxx' 'xxx' 'xxx' 'xxx' 'xxx' 'xxx' 'xxx' 'xxx' 'xxx' 'xxx' 'xxx' 'xxx' 'xxx' 'xxx' 'xxx' 'xxx' 'xxx' 'xxx';
      | 'eka' 'min' 'rso' 'qvv' 'yco' 'xxx' 'xxx' 'xxx' 'xxx' 'xxx' 'xxx' 'xxx' 'xxx' 'xxx' 'xxx' 'xxx' 'xxx' 'xxx' 'xxx' 'xxx' 'xxx' 'xxx' 'xxx' 'xxx';
      | 'qpb' 'out' 'xxx' 'xxx' 'xxx' 'xxx' 'xxx' 'xxx' 'xxx' 'xxx' 'xxx' 'xxx' 'xxx' 'xxx' 'xxx' 'xxx' 'xxx' 'xxx' 'xxx' 'xxx' 'xxx' 'xxx' 'xxx' 'xxx';
      | 'zqy' 'you' 'mwu' 'xxx' 'xxx' 'xxx' 'xxx' 'xxx' 'xxx' 'xxx' 'xxx' 'xxx' 'xxx' 'xxx' 'xxx' 'xxx' 'xxx' 'xxx' 'xxx' 'xxx' 'xxx' 'xxx' 'xxx' 'xxx';
      | 'evt' 'lup' 'xxx' 'xxx' 'xxx' 'xxx' 'xxx' 'xxx' 'xxx' 'xxx' 'xxx' 'xxx' 'xxx' 'xxx' 'xxx' 'xxx' 'xxx' 'xxx' 'xxx' 'xxx' 'xxx' 'xxx' 'xxx' 'xxx';
      | 'bxg' 'dfl' 'fxp' 'xxx' 'xxx' 'xxx' 'xxx' 'xxx' 'xxx' 'xxx' 'xxx' 'xxx' 'xxx' 'xxx' 'xxx' 'xxx' 'xxx' 'xxx' 'xxx' 'xxx' 'xxx' 'xxx' 'xxx' 'xxx';
      | 'uni' 'oab' 'kbr' 'evt' 'jaa' 'xxx' 'xxx' 'xxx' 'xxx' 'xxx' 'xxx' 'xxx' 'xxx' 'xxx' 'xxx' 'xxx' 'xxx' 'xxx' 'xxx' 'xxx' 'xxx' 'xxx' 'xxx' 'xxx';
      | 'uwp' 'xmq' 'dju' 'xxx' 'xxx' 'xxx' 'xxx' 'xxx' 'xxx' 'xxx' 'xxx' 'xxx' 'xxx' 'xxx' 'xxx' 'xxx' 'xxx' 'xxx' 'xxx' 'xxx' 'xxx' 'xxx' 'xxx' 'xxx';
      | 'rdm' 'ozd' 'vrt' 'you' 'fnr' 'xxx' 'xxx' 'xxx' 'xxx' 'xxx' 'xxx' 'xxx' 'xxx' 'xxx' 'xxx' 'xxx' 'xxx' 'xxx' 'xxx' 'xxx' 'xxx' 'xxx' 'xxx' 'xxx';
      | 'gwo' 'poc' 'xxx' 'xxx' 'xxx' 'xxx' 'xxx' 'xxx' 'xxx' 'xxx' 'xxx' 'xxx' 'xxx' 'xxx' 'xxx' 'xxx' 'xxx' 'xxx' 'xxx' 'xxx' 'xxx' 'xxx' 'xxx' 'xxx';
      | 'dto' 'bsb' 'xhk' 'lur' 'fpb' 'xxx' 'xxx' 'xxx' 'xxx' 'xxx' 'xxx' 'xxx' 'xxx' 'xxx' 'xxx' 'xxx' 'xxx' 'xxx' 'xxx' 'xxx' 'xxx' 'xxx' 'xxx' 'xxx';
      | 'ofz' 'dhu' 'fni' 'sgn' 'xxx' 'xxx' 'xxx' 'xxx' 'xxx' 'xxx' 'xxx' 'xxx' 'xxx' 'xxx' 'xxx' 'xxx' 'xxx' 'xxx' 'xxx' 'xxx' 'xxx' 'xxx' 'xxx' 'xxx';
      | 'fjm' 'bpc' 'xxx' 'xxx' 'xxx' 'xxx' 'xxx' 'xxx' 'xxx' 'xxx' 'xxx' 'xxx' 'xxx' 'xxx' 'xxx' 'xxx' 'xxx' 'xxx' 'xxx' 'xxx' 'xxx' 'xxx' 'xxx' 'xxx';
      | 'wsm' 'pde' 'luh' 'ejp' 'xxx' 'xxx' 'xxx' 'xxx' 'xxx' 'xxx' 'xxx' 'xxx' 'xxx' 'xxx' 'xxx' 'xxx' 'xxx' 'xxx' 'xxx' 'xxx' 'xxx' 'xxx' 'xxx' 'xxx';
      | 'tmb' 'amv' 'qwd' 'xxx' 'xxx' 'xxx' 'xxx' 'xxx' 'xxx' 'xxx' 'xxx' 'xxx' 'xxx' 'xxx' 'xxx' 'xxx' 'xxx' 'xxx' 'xxx' 'xxx' 'xxx' 'xxx' 'xxx' 'xxx';
      | 'kdl' 'bcq' 'ykt' 'lts' 'xxx' 'xxx' 'xxx' 'xxx' 'xxx' 'xxx' 'xxx' 'xxx' 'xxx' 'xxx' 'xxx' 'xxx' 'xxx' 'xxx' 'xxx' 'xxx' 'xxx' 'xxx' 'xxx' 'xxx';
      | 'jxm' 'ckh' 'hxf' 'xxx' 'xxx' 'xxx' 'xxx' 'xxx' 'xxx' 'xxx' 'xxx' 'xxx' 'xxx' 'xxx' 'xxx' 'xxx' 'xxx' 'xxx' 'xxx' 'xxx' 'xxx' 'xxx' 'xxx' 'xxx';
      | 'dyl' 'euq' 'avo' 'wmr' 'hns' 'xxx' 'xxx' 'xxx' 'xxx' 'xxx' 'xxx' 'xxx' 'xxx' 'xxx' 'xxx' 'xxx' 'xxx' 'xxx' 'xxx' 'xxx' 'xxx' 'xxx' 'xxx' 'xxx';
      | 'pxr' 'zqg' 'xxx' 'xxx' 'xxx' 'xxx' 'xxx' 'xxx' 'xxx' 'xxx' 'xxx' 'xxx' 'xxx' 'xxx' 'xxx' 'xxx' 'xxx' 'xxx' 'xxx' 'xxx' 'xxx' 'xxx' 'xxx' 'xxx';
      | 'xsx' 'yql' 'brg' 'xxx' 'xxx' 'xxx' 'xxx' 'xxx' 'xxx' 'xxx' 'xxx' 'xxx' 'xxx' 'xxx' 'xxx' 'xxx' 'xxx' 'xxx' 'xxx' 'xxx' 'xxx' 'xxx' 'xxx' 'xxx';
      | 'wdr' 'rss' 'fxl' 'kcf' 'xxx' 'xxx' 'xxx' 'xxx' 'xxx' 'xxx' 'xxx' 'xxx' 'xxx' 'xxx' 'xxx' 'xxx' 'xxx' 'xxx' 'xxx' 'xxx' 'xxx' 'xxx' 'xxx' 'xxx';
      | 'frd' 'rzo' 'qig' 'dzp' 'bhl' 'xxx' 'xxx' 'xxx' 'xxx' 'xxx' 'xxx' 'xxx' 'xxx' 'xxx' 'xxx' 'xxx' 'xxx' 'xxx' 'xxx' 'xxx' 'xxx' 'xxx' 'xxx' 'xxx';
      | 'tlb' 'zqy' 'mdb' 'xxx' 'xxx' 'xxx' 'xxx' 'xxx' 'xxx' 'xxx' 'xxx' 'xxx' 'xxx' 'xxx' 'xxx' 'xxx' 'xxx' 'xxx' 'xxx' 'xxx' 'xxx' 'xxx' 'xxx' 'xxx';
      | 'yvn' 'ynz' 'mjp' 'xxx' 'xxx' 'xxx' 'xxx' 'xxx' 'xxx' 'xxx' 'xxx' 'xxx' 'xxx' 'xxx' 'xxx' 'xxx' 'xxx' 'xxx' 'xxx' 'xxx' 'xxx' 'xxx' 'xxx' 'xxx';
      | 'bvv' 'fim' 'xxx' 'xxx' 'xxx' 'xxx' 'xxx' 'xxx' 'xxx' 'xxx' 'xxx' 'xxx' 'xxx' 'xxx' 'xxx' 'xxx' 'xxx' 'xxx' 'xxx' 'xxx' 'xxx' 'xxx' 'xxx' 'xxx';
      | 'xjh' 'oag' 'def' 'xxx' 'xxx' 'xxx' 'xxx' 'xxx' 'xxx' 'xxx' 'xxx' 'xxx' 'xxx' 'xxx' 'xxx' 'xxx' 'xxx' 'xxx' 'xxx' 'xxx' 'xxx' 'xxx' 'xxx' 'xxx';
      | 'jmk' 'vhi' 'bhv' 'tnt' 'izk' 'ewm' 'adp' 'nhj' 'qlf' 'gwo' 'fcj' 'xhd' 'ofz' 'aeo' 'ycr' 'ljy' 'hkq' 'xxx' 'xxx' 'xxx' 'xxx' 'xxx' 'xxx' 'xxx';
      | 'smb' 'ahv' 'xkn' 'ulo' 'xxx' 'xxx' 'xxx' 'xxx' 'xxx' 'xxx' 'xxx' 'xxx' 'xxx' 'xxx' 'xxx' 'xxx' 'xxx' 'xxx' 'xxx' 'xxx' 'xxx' 'xxx' 'xxx' 'xxx';
      | 'hbp' 'def' 'rtp' 'xxx' 'xxx' 'xxx' 'xxx' 'xxx' 'xxx' 'xxx' 'xxx' 'xxx' 'xxx' 'xxx' 'xxx' 'xxx' 'xxx' 'xxx' 'xxx' 'xxx' 'xxx' 'xxx' 'xxx' 'xxx';
      | 'fdl' 'quz' 'bpo' 'xxx' 'xxx' 'xxx' 'xxx' 'xxx' 'xxx' 'xxx' 'xxx' 'xxx' 'xxx' 'xxx' 'xxx' 'xxx' 'xxx' 'xxx' 'xxx' 'xxx' 'xxx' 'xxx' 'xxx' 'xxx';
      | 'flj' 'xay' 'wxl' 'xxx' 'xxx' 'xxx' 'xxx' 'xxx' 'xxx' 'xxx' 'xxx' 'xxx' 'xxx' 'xxx' 'xxx' 'xxx' 'xxx' 'xxx' 'xxx' 'xxx' 'xxx' 'xxx' 'xxx' 'xxx';
      | 'mkp' 'qgn' 'jlg' 'xxx' 'xxx' 'xxx' 'xxx' 'xxx' 'xxx' 'xxx' 'xxx' 'xxx' 'xxx' 'xxx' 'xxx' 'xxx' 'xxx' 'xxx' 'xxx' 'xxx' 'xxx' 'xxx' 'xxx' 'xxx';
      | 'fdg' 'mkd' 'agn' 'bda' 'kwv' 'bhh' 'xxx' 'xxx' 'xxx' 'xxx' 'xxx' 'xxx' 'xxx' 'xxx' 'xxx' 'xxx' 'xxx' 'xxx' 'xxx' 'xxx' 'xxx' 'xxx' 'xxx' 'xxx';
      | 'mpy' 'bpo' 'quz' 'dyl' 'xxx' 'xxx' 'xxx' 'xxx' 'xxx' 'xxx' 'xxx' 'xxx' 'xxx' 'xxx' 'xxx' 'xxx' 'xxx' 'xxx' 'xxx' 'xxx' 'xxx' 'xxx' 'xxx' 'xxx';
      | 'fim' 'yxq' 'bnw' 'bpc' 'xxx' 'xxx' 'xxx' 'xxx' 'xxx' 'xxx' 'xxx' 'xxx' 'xxx' 'xxx' 'xxx' 'xxx' 'xxx' 'xxx' 'xxx' 'xxx' 'xxx' 'xxx' 'xxx' 'xxx';
      | 'mwu' 'xhb' 'yft' 'myo' 'cui' 'gwv' 'mvn' 'fqn' 'fyx' 'vbp' 'wid' 'xxx' 'xxx' 'xxx' 'xxx' 'xxx' 'xxx' 'xxx' 'xxx' 'xxx' 'xxx' 'xxx' 'xxx' 'xxx';
      | 'yds' 'hhu' 'nel' 'xxx' 'xxx' 'xxx' 'xxx' 'xxx' 'xxx' 'xxx' 'xxx' 'xxx' 'xxx' 'xxx' 'xxx' 'xxx' 'xxx' 'xxx' 'xxx' 'xxx' 'xxx' 'xxx' 'xxx' 'xxx';
      | 'her' 'dfo' 'yba' 'puu' 'bag' 'xxx' 'xxx' 'xxx' 'xxx' 'xxx' 'xxx' 'xxx' 'xxx' 'xxx' 'xxx' 'xxx' 'xxx' 'xxx' 'xxx' 'xxx' 'xxx' 'xxx' 'xxx' 'xxx';
      | 'ipm' 'nki' 'wgx' 'lsu' 'pbf' 'xxx' 'xxx' 'xxx' 'xxx' 'xxx' 'xxx' 'xxx' 'xxx' 'xxx' 'xxx' 'xxx' 'xxx' 'xxx' 'xxx' 'xxx' 'xxx' 'xxx' 'xxx' 'xxx';
      | 'wfb' 'ulj' 'axk' 'ldf' 'xxx' 'xxx' 'xxx' 'xxx' 'xxx' 'xxx' 'xxx' 'xxx' 'xxx' 'xxx' 'xxx' 'xxx' 'xxx' 'xxx' 'xxx' 'xxx' 'xxx' 'xxx' 'xxx' 'xxx';
      | 'bvq' 'xyj' 'xxx' 'xxx' 'xxx' 'xxx' 'xxx' 'xxx' 'xxx' 'xxx' 'xxx' 'xxx' 'xxx' 'xxx' 'xxx' 'xxx' 'xxx' 'xxx' 'xxx' 'xxx' 'xxx' 'xxx' 'xxx' 'xxx';
      | 'hhu' 'ozd' 'you' 'fnr' 'xxx' 'xxx' 'xxx' 'xxx' 'xxx' 'xxx' 'xxx' 'xxx' 'xxx' 'xxx' 'xxx' 'xxx' 'xxx' 'xxx' 'xxx' 'xxx' 'xxx' 'xxx' 'xxx' 'xxx';
      | 'vfy' 'ulj' 'yqe' 'ldf' 'axk' 'xxx' 'xxx' 'xxx' 'xxx' 'xxx' 'xxx' 'xxx' 'xxx' 'xxx' 'xxx' 'xxx' 'xxx' 'xxx' 'xxx' 'xxx' 'xxx' 'xxx' 'xxx' 'xxx';
      | 'pld' 'qqj' 'fzl' 'xxx' 'xxx' 'xxx' 'xxx' 'xxx' 'xxx' 'xxx' 'xxx' 'xxx' 'xxx' 'xxx' 'xxx' 'xxx' 'xxx' 'xxx' 'xxx' 'xxx' 'xxx' 'xxx' 'xxx' 'xxx';
      | 'zkn' 'xvu' 'zfx' 'xcu' 'xxx' 'xxx' 'xxx' 'xxx' 'xxx' 'xxx' 'xxx' 'xxx' 'xxx' 'xxx' 'xxx' 'xxx' 'xxx' 'xxx' 'xxx' 'xxx' 'xxx' 'xxx' 'xxx' 'xxx';
      | 'rbo' 'fpb' 'lur' 'xxx' 'xxx' 'xxx' 'xxx' 'xxx' 'xxx' 'xxx' 'xxx' 'xxx' 'xxx' 'xxx' 'xxx' 'xxx' 'xxx' 'xxx' 'xxx' 'xxx' 'xxx' 'xxx' 'xxx' 'xxx';
      | 'zzk' 'yds' 'aeb' 'xxx' 'xxx' 'xxx' 'xxx' 'xxx' 'xxx' 'xxx' 'xxx' 'xxx' 'xxx' 'xxx' 'xxx' 'xxx' 'xxx' 'xxx' 'xxx' 'xxx' 'xxx' 'xxx' 'xxx' 'xxx';
      | 'rdn' 'bsb' 'igu' 'fpb' 'xxx' 'xxx' 'xxx' 'xxx' 'xxx' 'xxx' 'xxx' 'xxx' 'xxx' 'xxx' 'xxx' 'xxx' 'xxx' 'xxx' 'xxx' 'xxx' 'xxx' 'xxx' 'xxx' 'xxx';
      | 'ril' 'qmz' 'uxn' 'kde' 'kob' 'xxx' 'xxx' 'xxx' 'xxx' 'xxx' 'xxx' 'xxx' 'xxx' 'xxx' 'xxx' 'xxx' 'xxx' 'xxx' 'xxx' 'xxx' 'xxx' 'xxx' 'xxx' 'xxx';
      | 'foj' 'fdl' 'xxx' 'xxx' 'xxx' 'xxx' 'xxx' 'xxx' 'xxx' 'xxx' 'xxx' 'xxx' 'xxx' 'xxx' 'xxx' 'xxx' 'xxx' 'xxx' 'xxx' 'xxx' 'xxx' 'xxx' 'xxx' 'xxx';
      | 'xhb' 'krd' 'kvi' 'xxx' 'xxx' 'xxx' 'xxx' 'xxx' 'xxx' 'xxx' 'xxx' 'xxx' 'xxx' 'xxx' 'xxx' 'xxx' 'xxx' 'xxx' 'xxx' 'xxx' 'xxx' 'xxx' 'xxx' 'xxx';
      | 'htf' 'osk' 'rcp' 'xxx' 'xxx' 'xxx' 'xxx' 'xxx' 'xxx' 'xxx' 'xxx' 'xxx' 'xxx' 'xxx' 'xxx' 'xxx' 'xxx' 'xxx' 'xxx' 'xxx' 'xxx' 'xxx' 'xxx' 'xxx';
      | 'nrx' 'out' 'xxx' 'xxx' 'xxx' 'xxx' 'xxx' 'xxx' 'xxx' 'xxx' 'xxx' 'xxx' 'xxx' 'xxx' 'xxx' 'xxx' 'xxx' 'xxx' 'xxx' 'xxx' 'xxx' 'xxx' 'xxx' 'xxx';
      | 'zwl' 'xwv' 'uhn' 'cqf' 'xxx' 'xxx' 'xxx' 'xxx' 'xxx' 'xxx' 'xxx' 'xxx' 'xxx' 'xxx' 'xxx' 'xxx' 'xxx' 'xxx' 'xxx' 'xxx' 'xxx' 'xxx' 'xxx' 'xxx';
      | 'gyl' 'out' 'xxx' 'xxx' 'xxx' 'xxx' 'xxx' 'xxx' 'xxx' 'xxx' 'xxx' 'xxx' 'xxx' 'xxx' 'xxx' 'xxx' 'xxx' 'xxx' 'xxx' 'xxx' 'xxx' 'xxx' 'xxx' 'xxx';
      | 'dkw' 'rcp' 'osk' 'xxx' 'xxx' 'xxx' 'xxx' 'xxx' 'xxx' 'xxx' 'xxx' 'xxx' 'xxx' 'xxx' 'xxx' 'xxx' 'xxx' 'xxx' 'xxx' 'xxx' 'xxx' 'xxx' 'xxx' 'xxx';
      | 'sgu' 'wyl' 'iiu' 'vqp' 'bpj' 'sdr' 'tyq' 'tbn' 'cfo' 'eff' 'wpo' 'xso' 'xao' 'ltv' 'xxx' 'xxx' 'xxx' 'xxx' 'xxx' 'xxx' 'xxx' 'xxx' 'xxx' 'xxx';
      | 'pbf' 'sta' 'xxx' 'xxx' 'xxx' 'xxx' 'xxx' 'xxx' 'xxx' 'xxx' 'xxx' 'xxx' 'xxx' 'xxx' 'xxx' 'xxx' 'xxx' 'xxx' 'xxx' 'xxx' 'xxx' 'xxx' 'xxx' 'xxx';
      | 'ytk' 'oag' 'xxx' 'xxx' 'xxx' 'xxx' 'xxx' 'xxx' 'xxx' 'xxx' 'xxx' 'xxx' 'xxx' 'xxx' 'xxx' 'xxx' 'xxx' 'xxx' 'xxx' 'xxx' 'xxx' 'xxx' 'xxx' 'xxx';
      | 'irm' 'shb' 'kul' 'xxx' 'xxx' 'xxx' 'xxx' 'xxx' 'xxx' 'xxx' 'xxx' 'xxx' 'xxx' 'xxx' 'xxx' 'xxx' 'xxx' 'xxx' 'xxx' 'xxx' 'xxx' 'xxx' 'xxx' 'xxx';
      | 'brg' 'wpo' 'iqh' 'tyq' 'tbn' 'uwn' 'xxx' 'xxx' 'xxx' 'xxx' 'xxx' 'xxx' 'xxx' 'xxx' 'xxx' 'xxx' 'xxx' 'xxx' 'xxx' 'xxx' 'xxx' 'xxx' 'xxx' 'xxx';
      | 'dzp' 'xpu' 'uos' 'xxx' 'xxx' 'xxx' 'xxx' 'xxx' 'xxx' 'xxx' 'xxx' 'xxx' 'xxx' 'xxx' 'xxx' 'xxx' 'xxx' 'xxx' 'xxx' 'xxx' 'xxx' 'xxx' 'xxx' 'xxx';
      | 'ufe' 'utb' 'nel' 'hhu' 'xxx' 'xxx' 'xxx' 'xxx' 'xxx' 'xxx' 'xxx' 'xxx' 'xxx' 'xxx' 'xxx' 'xxx' 'xxx' 'xxx' 'xxx' 'xxx' 'xxx' 'xxx' 'xxx' 'xxx';
      | 'gpo' 'jlg' 'xxx' 'xxx' 'xxx' 'xxx' 'xxx' 'xxx' 'xxx' 'xxx' 'xxx' 'xxx' 'xxx' 'xxx' 'xxx' 'xxx' 'xxx' 'xxx' 'xxx' 'xxx' 'xxx' 'xxx' 'xxx' 'xxx';
      | 'ihy' 'bhl' 'rzo' 'dzp' 'qig' 'xxx' 'xxx' 'xxx' 'xxx' 'xxx' 'xxx' 'xxx' 'xxx' 'xxx' 'xxx' 'xxx' 'xxx' 'xxx' 'xxx' 'xxx' 'xxx' 'xxx' 'xxx' 'xxx';
      | 'jlg' 'srh' 'tqs' 'bvv' 'tmb' 'dcr' 'xxx' 'xxx' 'xxx' 'xxx' 'xxx' 'xxx' 'xxx' 'xxx' 'xxx' 'xxx' 'xxx' 'xxx' 'xxx' 'xxx' 'xxx' 'xxx' 'xxx' 'xxx';
      | 'qgh' 'jwy' 'fmr' 'tat' 'irm' 'xxx' 'xxx' 'xxx' 'xxx' 'xxx' 'xxx' 'xxx' 'xxx' 'xxx' 'xxx' 'xxx' 'xxx' 'xxx' 'xxx' 'xxx' 'xxx' 'xxx' 'xxx' 'xxx';
      | 'aiu' 'out' 'xxx' 'xxx' 'xxx' 'xxx' 'xxx' 'xxx' 'xxx' 'xxx' 'xxx' 'xxx' 'xxx' 'xxx' 'xxx' 'xxx' 'xxx' 'xxx' 'xxx' 'xxx' 'xxx' 'xxx' 'xxx' 'xxx';
      | 'itv' 'grp' 'qgy' 'xxx' 'xxx' 'xxx' 'xxx' 'xxx' 'xxx' 'xxx' 'xxx' 'xxx' 'xxx' 'xxx' 'xxx' 'xxx' 'xxx' 'xxx' 'xxx' 'xxx' 'xxx' 'xxx' 'xxx' 'xxx';
      | 'cqs' 'yds' 'ufe' 'ssx' 'xxx' 'xxx' 'xxx' 'xxx' 'xxx' 'xxx' 'xxx' 'xxx' 'xxx' 'xxx' 'xxx' 'xxx' 'xxx' 'xxx' 'xxx' 'xxx' 'xxx' 'xxx' 'xxx' 'xxx';
      | 'mpj' 'igu' 'xhk' 'xxx' 'xxx' 'xxx' 'xxx' 'xxx' 'xxx' 'xxx' 'xxx' 'xxx' 'xxx' 'xxx' 'xxx' 'xxx' 'xxx' 'xxx' 'xxx' 'xxx' 'xxx' 'xxx' 'xxx' 'xxx';
      | 'pvw' 'ppm' 'laq' 'xxx' 'xxx' 'xxx' 'xxx' 'xxx' 'xxx' 'xxx' 'xxx' 'xxx' 'xxx' 'xxx' 'xxx' 'xxx' 'xxx' 'xxx' 'xxx' 'xxx' 'xxx' 'xxx' 'xxx' 'xxx';
      | 'mpi' 'xee' 'knq' 'xxx' 'xxx' 'xxx' 'xxx' 'xxx' 'xxx' 'xxx' 'xxx' 'xxx' 'xxx' 'xxx' 'xxx' 'xxx' 'xxx' 'xxx' 'xxx' 'xxx' 'xxx' 'xxx' 'xxx' 'xxx';
      | 'pab' 'gyl' 'xxx' 'xxx' 'xxx' 'xxx' 'xxx' 'xxx' 'xxx' 'xxx' 'xxx' 'xxx' 'xxx' 'xxx' 'xxx' 'xxx' 'xxx' 'xxx' 'xxx' 'xxx' 'xxx' 'xxx' 'xxx' 'xxx';
      | 'jef' 'rss' 'kcf' 'iyj' 'xxx' 'xxx' 'xxx' 'xxx' 'xxx' 'xxx' 'xxx' 'xxx' 'xxx' 'xxx' 'xxx' 'xxx' 'xxx' 'xxx' 'xxx' 'xxx' 'xxx' 'xxx' 'xxx' 'xxx';
      | 'qig' 'pxr' 'xpu' 'xxx' 'xxx' 'xxx' 'xxx' 'xxx' 'xxx' 'xxx' 'xxx' 'xxx' 'xxx' 'xxx' 'xxx' 'xxx' 'xxx' 'xxx' 'xxx' 'xxx' 'xxx' 'xxx' 'xxx' 'xxx';
      | 'lra' 'pvm' 'xxx' 'xxx' 'xxx' 'xxx' 'xxx' 'xxx' 'xxx' 'xxx' 'xxx' 'xxx' 'xxx' 'xxx' 'xxx' 'xxx' 'xxx' 'xxx' 'xxx' 'xxx' 'xxx' 'xxx' 'xxx' 'xxx';
      | 'che' 'rzo' 'qig' 'dzp' 'ybw' 'xxx' 'xxx' 'xxx' 'xxx' 'xxx' 'xxx' 'xxx' 'xxx' 'xxx' 'xxx' 'xxx' 'xxx' 'xxx' 'xxx' 'xxx' 'xxx' 'xxx' 'xxx' 'xxx';
      | 'xao' 'rqn' 'fak' 'wke' 'xxx' 'xxx' 'xxx' 'xxx' 'xxx' 'xxx' 'xxx' 'xxx' 'xxx' 'xxx' 'xxx' 'xxx' 'xxx' 'xxx' 'xxx' 'xxx' 'xxx' 'xxx' 'xxx' 'xxx';
      | 'nta' 'vpo' 'xuk' 'xxx' 'xxx' 'xxx' 'xxx' 'xxx' 'xxx' 'xxx' 'xxx' 'xxx' 'xxx' 'xxx' 'xxx' 'xxx' 'xxx' 'xxx' 'xxx' 'xxx' 'xxx' 'xxx' 'xxx' 'xxx';
      | 'rta' 'lur' 'igu' 'bsb' 'xxx' 'xxx' 'xxx' 'xxx' 'xxx' 'xxx' 'xxx' 'xxx' 'xxx' 'xxx' 'xxx' 'xxx' 'xxx' 'xxx' 'xxx' 'xxx' 'xxx' 'xxx' 'xxx' 'xxx';
      | 'qvv' 'out' 'xxx' 'xxx' 'xxx' 'xxx' 'xxx' 'xxx' 'xxx' 'xxx' 'xxx' 'xxx' 'xxx' 'xxx' 'xxx' 'xxx' 'xxx' 'xxx' 'xxx' 'xxx' 'xxx' 'xxx' 'xxx' 'xxx';
      | 'fpb' 'puz' 'cqs' 'ixc' 'fnn' 'tkl' 'nqo' 'jpb' 'zzk' 'zib' 'yun' 'cur' 'pmu' 'nta' 'ybr' 'ril' 'uzn' 'zwl' 'xxx' 'xxx' 'xxx' 'xxx' 'xxx' 'xxx';
      | 'imq' 'hwj' 'qeg' 'gpo' 'xxx' 'xxx' 'xxx' 'xxx' 'xxx' 'xxx' 'xxx' 'xxx' 'xxx' 'xxx' 'xxx' 'xxx' 'xxx' 'xxx' 'xxx' 'xxx' 'xxx' 'xxx' 'xxx' 'xxx';
      | 'jkx' 'fhq' 'mub' 'sfu' 'xxx' 'xxx' 'xxx' 'xxx' 'xxx' 'xxx' 'xxx' 'xxx' 'xxx' 'xxx' 'xxx' 'xxx' 'xxx' 'xxx' 'xxx' 'xxx' 'xxx' 'xxx' 'xxx' 'xxx';
      | 'ael' 'lzl' 'dto' 'xxx' 'xxx' 'xxx' 'xxx' 'xxx' 'xxx' 'xxx' 'xxx' 'xxx' 'xxx' 'xxx' 'xxx' 'xxx' 'xxx' 'xxx' 'xxx' 'xxx' 'xxx' 'xxx' 'xxx' 'xxx';
      | 'wyl' 'srd' 'bdl' 'mci' 'xxx' 'xxx' 'xxx' 'xxx' 'xxx' 'xxx' 'xxx' 'xxx' 'xxx' 'xxx' 'xxx' 'xxx' 'xxx' 'xxx' 'xxx' 'xxx' 'xxx' 'xxx' 'xxx' 'xxx';
      | 'hkq' 'zkn' 'czt' 'xxx' 'xxx' 'xxx' 'xxx' 'xxx' 'xxx' 'xxx' 'xxx' 'xxx' 'xxx' 'xxx' 'xxx' 'xxx' 'xxx' 'xxx' 'xxx' 'xxx' 'xxx' 'xxx' 'xxx' 'xxx';
      | 'apv' 'utn' 'crd' 'sof' 'pld' 'xxx' 'xxx' 'xxx' 'xxx' 'xxx' 'xxx' 'xxx' 'xxx' 'xxx' 'xxx' 'xxx' 'xxx' 'xxx' 'xxx' 'xxx' 'xxx' 'xxx' 'xxx' 'xxx';
      | 'kbr' 'ftq' 'xxx' 'xxx' 'xxx' 'xxx' 'xxx' 'xxx' 'xxx' 'xxx' 'xxx' 'xxx' 'xxx' 'xxx' 'xxx' 'xxx' 'xxx' 'xxx' 'xxx' 'xxx' 'xxx' 'xxx' 'xxx' 'xxx';
      | 'xwv' 'iqf' 'lzx' 'xxx' 'xxx' 'xxx' 'xxx' 'xxx' 'xxx' 'xxx' 'xxx' 'xxx' 'xxx' 'xxx' 'xxx' 'xxx' 'xxx' 'xxx' 'xxx' 'xxx' 'xxx' 'xxx' 'xxx' 'xxx';
      | 'cfo' 'lre' 'bdl' 'srd' 'xxx' 'xxx' 'xxx' 'xxx' 'xxx' 'xxx' 'xxx' 'xxx' 'xxx' 'xxx' 'xxx' 'xxx' 'xxx' 'xxx' 'xxx' 'xxx' 'xxx' 'xxx' 'xxx' 'xxx';
      | 'ysr' 'fpb' 'xhk' 'bsb' 'xxx' 'xxx' 'xxx' 'xxx' 'xxx' 'xxx' 'xxx' 'xxx' 'xxx' 'xxx' 'xxx' 'xxx' 'xxx' 'xxx' 'xxx' 'xxx' 'xxx' 'xxx' 'xxx' 'xxx';
      | 'aia' 'dkm' 'ejp' 'xxx' 'xxx' 'xxx' 'xxx' 'xxx' 'xxx' 'xxx' 'xxx' 'xxx' 'xxx' 'xxx' 'xxx' 'xxx' 'xxx' 'xxx' 'xxx' 'xxx' 'xxx' 'xxx' 'xxx' 'xxx';
      | 'ndc' 'awp' 'lup' 'ftq' 'xxx' 'xxx' 'xxx' 'xxx' 'xxx' 'xxx' 'xxx' 'xxx' 'xxx' 'xxx' 'xxx' 'xxx' 'xxx' 'xxx' 'xxx' 'xxx' 'xxx' 'xxx' 'xxx' 'xxx';
      | 'bhh' 'ola' 'xxx' 'xxx' 'xxx' 'xxx' 'xxx' 'xxx' 'xxx' 'xxx' 'xxx' 'xxx' 'xxx' 'xxx' 'xxx' 'xxx' 'xxx' 'xxx' 'xxx' 'xxx' 'xxx' 'xxx' 'xxx' 'xxx';
      | 'bhv' 'poc' 'daz' 'vtp' 'tda' 'cxr' 'xxx' 'xxx' 'xxx' 'xxx' 'xxx' 'xxx' 'xxx' 'xxx' 'xxx' 'xxx' 'xxx' 'xxx' 'xxx' 'xxx' 'xxx' 'xxx' 'xxx' 'xxx';
      | 'uqb' 'hgu' 'xxx' 'xxx' 'xxx' 'xxx' 'xxx' 'xxx' 'xxx' 'xxx' 'xxx' 'xxx' 'xxx' 'xxx' 'xxx' 'xxx' 'xxx' 'xxx' 'xxx' 'xxx' 'xxx' 'xxx' 'xxx' 'xxx';
      | 'xkn' 'yql' 'xxx' 'xxx' 'xxx' 'xxx' 'xxx' 'xxx' 'xxx' 'xxx' 'xxx' 'xxx' 'xxx' 'xxx' 'xxx' 'xxx' 'xxx' 'xxx' 'xxx' 'xxx' 'xxx' 'xxx' 'xxx' 'xxx';
      | 'eej' 'imq' 'xxx' 'xxx' 'xxx' 'xxx' 'xxx' 'xxx' 'xxx' 'xxx' 'xxx' 'xxx' 'xxx' 'xxx' 'xxx' 'xxx' 'xxx' 'xxx' 'xxx' 'xxx' 'xxx' 'xxx' 'xxx' 'xxx';
      | 'ihm' 'htw' 'pxk' 'xxx' 'xxx' 'xxx' 'xxx' 'xxx' 'xxx' 'xxx' 'xxx' 'xxx' 'xxx' 'xxx' 'xxx' 'xxx' 'xxx' 'xxx' 'xxx' 'xxx' 'xxx' 'xxx' 'xxx' 'xxx';
      | 'phh' 'rdn' 'lyf' 'nac' 'xxx' 'xxx' 'xxx' 'xxx' 'xxx' 'xxx' 'xxx' 'xxx' 'xxx' 'xxx' 'xxx' 'xxx' 'xxx' 'xxx' 'xxx' 'xxx' 'xxx' 'xxx' 'xxx' 'xxx';
      | 'cvl' 'fpb' 'igu' 'lur' 'xhk' 'xxx' 'xxx' 'xxx' 'xxx' 'xxx' 'xxx' 'xxx' 'xxx' 'xxx' 'xxx' 'xxx' 'xxx' 'xxx' 'xxx' 'xxx' 'xxx' 'xxx' 'xxx' 'xxx';
      | 'rzo' 'uos' 'xxx' 'xxx' 'xxx' 'xxx' 'xxx' 'xxx' 'xxx' 'xxx' 'xxx' 'xxx' 'xxx' 'xxx' 'xxx' 'xxx' 'xxx' 'xxx' 'xxx' 'xxx' 'xxx' 'xxx' 'xxx' 'xxx';
      | 'uzn' 'kde' 'xxx' 'xxx' 'xxx' 'xxx' 'xxx' 'xxx' 'xxx' 'xxx' 'xxx' 'xxx' 'xxx' 'xxx' 'xxx' 'xxx' 'xxx' 'xxx' 'xxx' 'xxx' 'xxx' 'xxx' 'xxx' 'xxx';
      | 'jly' 'jmk' 'sta' 'xee' 'knq' 'xxx' 'xxx' 'xxx' 'xxx' 'xxx' 'xxx' 'xxx' 'xxx' 'xxx' 'xxx' 'xxx' 'xxx' 'xxx' 'xxx' 'xxx' 'xxx' 'xxx' 'xxx' 'xxx';
      | 'otp' 'her' 'xxx' 'xxx' 'xxx' 'xxx' 'xxx' 'xxx' 'xxx' 'xxx' 'xxx' 'xxx' 'xxx' 'xxx' 'xxx' 'xxx' 'xxx' 'xxx' 'xxx' 'xxx' 'xxx' 'xxx' 'xxx' 'xxx';
      | 'vii' 'out' 'xxx' 'xxx' 'xxx' 'xxx' 'xxx' 'xxx' 'xxx' 'xxx' 'xxx' 'xxx' 'xxx' 'xxx' 'xxx' 'xxx' 'xxx' 'xxx' 'xxx' 'xxx' 'xxx' 'xxx' 'xxx' 'xxx';
      | 'fni' 'ogv' 'uqe' 'kzl' 'xxx' 'xxx' 'xxx' 'xxx' 'xxx' 'xxx' 'xxx' 'xxx' 'xxx' 'xxx' 'xxx' 'xxx' 'xxx' 'xxx' 'xxx' 'xxx' 'xxx' 'xxx' 'xxx' 'xxx';
      | 'phc' 'ysr' 'xxx' 'xxx' 'xxx' 'xxx' 'xxx' 'xxx' 'xxx' 'xxx' 'xxx' 'xxx' 'xxx' 'xxx' 'xxx' 'xxx' 'xxx' 'xxx' 'xxx' 'xxx' 'xxx' 'xxx' 'xxx' 'xxx';
      | 'srf' 'bmu' 'mzw' 'xxx' 'xxx' 'xxx' 'xxx' 'xxx' 'xxx' 'xxx' 'xxx' 'xxx' 'xxx' 'xxx' 'xxx' 'xxx' 'xxx' 'xxx' 'xxx' 'xxx' 'xxx' 'xxx' 'xxx' 'xxx';
      | 'fnn' 'xwv' 'xxx' 'xxx' 'xxx' 'xxx' 'xxx' 'xxx' 'xxx' 'xxx' 'xxx' 'xxx' 'xxx' 'xxx' 'xxx' 'xxx' 'xxx' 'xxx' 'xxx' 'xxx' 'xxx' 'xxx' 'xxx' 'xxx';
      | 'rmg' 'you' 'xxx' 'xxx' 'xxx' 'xxx' 'xxx' 'xxx' 'xxx' 'xxx' 'xxx' 'xxx' 'xxx' 'xxx' 'xxx' 'xxx' 'xxx' 'xxx' 'xxx' 'xxx' 'xxx' 'xxx' 'xxx' 'xxx';
      | 'heh' 'knq' 'jmk' 'xee' 'txi' 'xxx' 'xxx' 'xxx' 'xxx' 'xxx' 'xxx' 'xxx' 'xxx' 'xxx' 'xxx' 'xxx' 'xxx' 'xxx' 'xxx' 'xxx' 'xxx' 'xxx' 'xxx' 'xxx';
      | 'elj' 'frd' 'kbe' 'che' 'suv' 'xxx' 'xxx' 'xxx' 'xxx' 'xxx' 'xxx' 'xxx' 'xxx' 'xxx' 'xxx' 'xxx' 'xxx' 'xxx' 'xxx' 'xxx' 'xxx' 'xxx' 'xxx' 'xxx';
      | 'fxl' 'dka' 'kez' 'pvw' 'uzw' 'xxx' 'xxx' 'xxx' 'xxx' 'xxx' 'xxx' 'xxx' 'xxx' 'xxx' 'xxx' 'xxx' 'xxx' 'xxx' 'xxx' 'xxx' 'xxx' 'xxx' 'xxx' 'xxx';
      | 'sgy' 'uqb' 'xxx' 'xxx' 'xxx' 'xxx' 'xxx' 'xxx' 'xxx' 'xxx' 'xxx' 'xxx' 'xxx' 'xxx' 'xxx' 'xxx' 'xxx' 'xxx' 'xxx' 'xxx' 'xxx' 'xxx' 'xxx' 'xxx';
      | 'vns' 'vrt' 'fnr' 'xxx' 'xxx' 'xxx' 'xxx' 'xxx' 'xxx' 'xxx' 'xxx' 'xxx' 'xxx' 'xxx' 'xxx' 'xxx' 'xxx' 'xxx' 'xxx' 'xxx' 'xxx' 'xxx' 'xxx' 'xxx';
      | 'gdh' 'hpw' 'xxx' 'xxx' 'xxx' 'xxx' 'xxx' 'xxx' 'xxx' 'xxx' 'xxx' 'xxx' 'xxx' 'xxx' 'xxx' 'xxx' 'xxx' 'xxx' 'xxx' 'xxx' 'xxx' 'xxx' 'xxx' 'xxx';
      | 'bag' 'pab' 'aov' 'xbk' 'cmi' 'xxx' 'xxx' 'xxx' 'xxx' 'xxx' 'xxx' 'xxx' 'xxx' 'xxx' 'xxx' 'xxx' 'xxx' 'xxx' 'xxx' 'xxx' 'xxx' 'xxx' 'xxx' 'xxx';
      | 'bqw' 'dml' 'tum' 'php' 'xxx' 'xxx' 'xxx' 'xxx' 'xxx' 'xxx' 'xxx' 'xxx' 'xxx' 'xxx' 'xxx' 'xxx' 'xxx' 'xxx' 'xxx' 'xxx' 'xxx' 'xxx' 'xxx' 'xxx';
      | 'txi' 'aeo' 'dmr' 'adp' 'waa' 'nhj' 'uni' 'xxx' 'xxx' 'xxx' 'xxx' 'xxx' 'xxx' 'xxx' 'xxx' 'xxx' 'xxx' 'xxx' 'xxx' 'xxx' 'xxx' 'xxx' 'xxx' 'xxx';
      | 'krd' 'gwp' 'xxx' 'xxx' 'xxx' 'xxx' 'xxx' 'xxx' 'xxx' 'xxx' 'xxx' 'xxx' 'xxx' 'xxx' 'xxx' 'xxx' 'xxx' 'xxx' 'xxx' 'xxx' 'xxx' 'xxx' 'xxx' 'xxx';
      | 'wke' 'dni' 'wxl' 'jwl' 'xxx' 'xxx' 'xxx' 'xxx' 'xxx' 'xxx' 'xxx' 'xxx' 'xxx' 'xxx' 'xxx' 'xxx' 'xxx' 'xxx' 'xxx' 'xxx' 'xxx' 'xxx' 'xxx' 'xxx';
      | 'ldf' 'uqb' 'tcu' 'hrd' 'xxx' 'xxx' 'xxx' 'xxx' 'xxx' 'xxx' 'xxx' 'xxx' 'xxx' 'xxx' 'xxx' 'xxx' 'xxx' 'xxx' 'xxx' 'xxx' 'xxx' 'xxx' 'xxx' 'xxx';
      | 'jmn' 'knq' 'xee' 'jmk' 'xxx' 'xxx' 'xxx' 'xxx' 'xxx' 'xxx' 'xxx' 'xxx' 'xxx' 'xxx' 'xxx' 'xxx' 'xxx' 'xxx' 'xxx' 'xxx' 'xxx' 'xxx' 'xxx' 'xxx';
      | 'ylm' 'fan' 'bcq' 'lts' 'xxx' 'xxx' 'xxx' 'xxx' 'xxx' 'xxx' 'xxx' 'xxx' 'xxx' 'xxx' 'xxx' 'xxx' 'xxx' 'xxx' 'xxx' 'xxx' 'xxx' 'xxx' 'xxx' 'xxx';
      | 'qpo' 'ppm' 'laq' 'qgn' 'jlg' 'xxx' 'xxx' 'xxx' 'xxx' 'xxx' 'xxx' 'xxx' 'xxx' 'xxx' 'xxx' 'xxx' 'xxx' 'xxx' 'xxx' 'xxx' 'xxx' 'xxx' 'xxx' 'xxx';
      | 'qgn' 'ucp' 'ejz' 'phn' 'cmt' 'lcp' 'uuh' 'xje' 'tqs' 'gep' 'foj' 'gdh' 'tph' 'nhf' 'fwn' 'dcr' 'wck' 'ryr' 'bvv' 'tmb' 'zrw' 'srh' 'vis' 'ggn';
      | 'tpb' 'ifs' 'laq' 'xxx' 'xxx' 'xxx' 'xxx' 'xxx' 'xxx' 'xxx' 'xxx' 'xxx' 'xxx' 'xxx' 'xxx' 'xxx' 'xxx' 'xxx' 'xxx' 'xxx' 'xxx' 'xxx' 'xxx' 'xxx';
      | 'uvl' 'hlo' 'cel' 'bxg' 'pbm' 'xxx' 'xxx' 'xxx' 'xxx' 'xxx' 'xxx' 'xxx' 'xxx' 'xxx' 'xxx' 'xxx' 'xxx' 'xxx' 'xxx' 'xxx' 'xxx' 'xxx' 'xxx' 'xxx';
      | 'iur' 'rjp' 'vnd' 'ytc' 'xxx' 'xxx' 'xxx' 'xxx' 'xxx' 'xxx' 'xxx' 'xxx' 'xxx' 'xxx' 'xxx' 'xxx' 'xxx' 'xxx' 'xxx' 'xxx' 'xxx' 'xxx' 'xxx' 'xxx';
      | 'oil' 'uut' 'lte' 'xxx' 'xxx' 'xxx' 'xxx' 'xxx' 'xxx' 'xxx' 'xxx' 'xxx' 'xxx' 'xxx' 'xxx' 'xxx' 'xxx' 'xxx' 'xxx' 'xxx' 'xxx' 'xxx' 'xxx' 'xxx';
      | 'oxm' 'ppm' 'laq' 'qgn' 'jlg' 'xxx' 'xxx' 'xxx' 'xxx' 'xxx' 'xxx' 'xxx' 'xxx' 'xxx' 'xxx' 'xxx' 'xxx' 'xxx' 'xxx' 'xxx' 'xxx' 'xxx' 'xxx' 'xxx';
      | 'grp' 'qgh' 'sid' 'xxx' 'xxx' 'xxx' 'xxx' 'xxx' 'xxx' 'xxx' 'xxx' 'xxx' 'xxx' 'xxx' 'xxx' 'xxx' 'xxx' 'xxx' 'xxx' 'xxx' 'xxx' 'xxx' 'xxx' 'xxx';
      | 'lzx' 'vns' 'csx' 'saf' 'xxx' 'xxx' 'xxx' 'xxx' 'xxx' 'xxx' 'xxx' 'xxx' 'xxx' 'xxx' 'xxx' 'xxx' 'xxx' 'xxx' 'xxx' 'xxx' 'xxx' 'xxx' 'xxx' 'xxx';
      | 'uji' 'qgn' 'jlg' 'ppm' 'laq' 'xxx' 'xxx' 'xxx' 'xxx' 'xxx' 'xxx' 'xxx' 'xxx' 'xxx' 'xxx' 'xxx' 'xxx' 'xxx' 'xxx' 'xxx' 'xxx' 'xxx' 'xxx' 'xxx';
      | 'amv' 'wks' 'uge' 'tns' 'xxx' 'xxx' 'xxx' 'xxx' 'xxx' 'xxx' 'xxx' 'xxx' 'xxx' 'xxx' 'xxx' 'xxx' 'xxx' 'xxx' 'xxx' 'xxx' 'xxx' 'xxx' 'xxx' 'xxx';
      | 'qup' 'qcj' 'xxx' 'xxx' 'xxx' 'xxx' 'xxx' 'xxx' 'xxx' 'xxx' 'xxx' 'xxx' 'xxx' 'xxx' 'xxx' 'xxx' 'xxx' 'xxx' 'xxx' 'xxx' 'xxx' 'xxx' 'xxx' 'xxx';
      | 'xmq' 'mwu' 'you' 'xxx' 'xxx' 'xxx' 'xxx' 'xxx' 'xxx' 'xxx' 'xxx' 'xxx' 'xxx' 'xxx' 'xxx' 'xxx' 'xxx' 'xxx' 'xxx' 'xxx' 'xxx' 'xxx' 'xxx' 'xxx';
      | 'fqn' 'sva' 'xxx' 'xxx' 'xxx' 'xxx' 'xxx' 'xxx' 'xxx' 'xxx' 'xxx' 'xxx' 'xxx' 'xxx' 'xxx' 'xxx' 'xxx' 'xxx' 'xxx' 'xxx' 'xxx' 'xxx' 'xxx' 'xxx';
      | 'gpu' 'sta' 'xee' 'jmk' 'txi' 'xxx' 'xxx' 'xxx' 'xxx' 'xxx' 'xxx' 'xxx' 'xxx' 'xxx' 'xxx' 'xxx' 'xxx' 'xxx' 'xxx' 'xxx' 'xxx' 'xxx' 'xxx' 'xxx';
      | 'nfj' 'mwd' 'goq' 'xxx' 'xxx' 'xxx' 'xxx' 'xxx' 'xxx' 'xxx' 'xxx' 'xxx' 'xxx' 'xxx' 'xxx' 'xxx' 'xxx' 'xxx' 'xxx' 'xxx' 'xxx' 'xxx' 'xxx' 'xxx';])
  Constant1 : Constant  Commented=on  Value=|
      | double(['fxp' 'udl' 'vii' 'hgb' 'qmy' 'xxx' 'xxx' 'xxx' 'xxx' 'xxx' 'xxx' 'xxx' 'xxx' 'xxx' 'xxx' 'xxx' 'xxx' 'xxx' 'xxx' 'xxx' 'xxx' 'xxx' 'xxx' 'xxx';
      | 'ixc' 'cje' 'lra' 'jhu' 'xxx' 'xxx' 'xxx' 'xxx' 'xxx' 'xxx' 'xxx' 'xxx' 'xxx' 'xxx' 'xxx' 'xxx' 'xxx' 'xxx' 'xxx' 'xxx' 'xxx' 'xxx' 'xxx' 'xxx';
      | 'sgn' 'apv' 'vbc' 'xxx' 'xxx' 'xxx' 'xxx' 'xxx' 'xxx' 'xxx' 'xxx' 'xxx' 'xxx' 'xxx' 'xxx' 'xxx' 'xxx' 'xxx' 'xxx' 'xxx' 'xxx' 'xxx' 'xxx' 'xxx';
      | 'wua' 'knq' 'xxx' 'xxx' 'xxx' 'xxx' 'xxx' 'xxx' 'xxx' 'xxx' 'xxx' 'xxx' 'xxx' 'xxx' 'xxx' 'xxx' 'xxx' 'xxx' 'xxx' 'xxx' 'xxx' 'xxx' 'xxx' 'xxx';
      | 'fnr' 'csd' 'awl' 'vvj' 'fyx' 'cvi' 'xhb' 'mvn' 'guw' 'wid' 'vbp' 'uvk' 'krt' 'oil' 'izj' 'zlh' 'gwv' 'xxx' 'xxx' 'xxx' 'xxx' 'xxx' 'xxx' 'xxx';
      | 'krt' 'grp' 'cml' 'vxt' 'xxx' 'xxx' 'xxx' 'xxx' 'xxx' 'xxx' 'xxx' 'xxx' 'xxx' 'xxx' 'xxx' 'xxx' 'xxx' 'xxx' 'xxx' 'xxx' 'xxx' 'xxx' 'xxx' 'xxx';
      | 'hwj' 'laq' 'jlg' 'xxx' 'xxx' 'xxx' 'xxx' 'xxx' 'xxx' 'xxx' 'xxx' 'xxx' 'xxx' 'xxx' 'xxx' 'xxx' 'xxx' 'xxx' 'xxx' 'xxx' 'xxx' 'xxx' 'xxx' 'xxx';
      | 'rus' 'out' 'xxx' 'xxx' 'xxx' 'xxx' 'xxx' 'xxx' 'xxx' 'xxx' 'xxx' 'xxx' 'xxx' 'xxx' 'xxx' 'xxx' 'xxx' 'xxx' 'xxx' 'xxx' 'xxx' 'xxx' 'xxx' 'xxx';
      | 'oag' 'wrc' 'gpp' 'xxx' 'xxx' 'xxx' 'xxx' 'xxx' 'xxx' 'xxx' 'xxx' 'xxx' 'xxx' 'xxx' 'xxx' 'xxx' 'xxx' 'xxx' 'xxx' 'xxx' 'xxx' 'xxx' 'xxx' 'xxx';
      | 'uos' 'zqg' 'aiu' 'gdx' 'xxx' 'xxx' 'xxx' 'xxx' 'xxx' 'xxx' 'xxx' 'xxx' 'xxx' 'xxx' 'xxx' 'xxx' 'xxx' 'xxx' 'xxx' 'xxx' 'xxx' 'xxx' 'xxx' 'xxx';
      | 'xpu' 'qpb' 'zqg' 'gdx' 'aiu' 'xxx' 'xxx' 'xxx' 'xxx' 'xxx' 'xxx' 'xxx' 'xxx' 'xxx' 'xxx' 'xxx' 'xxx' 'xxx' 'xxx' 'xxx' 'xxx' 'xxx' 'xxx' 'xxx';
      | 'mdb' 'fnr' 'mwu' 'ozd' 'xxx' 'xxx' 'xxx' 'xxx' 'xxx' 'xxx' 'xxx' 'xxx' 'xxx' 'xxx' 'xxx' 'xxx' 'xxx' 'xxx' 'xxx' 'xxx' 'xxx' 'xxx' 'xxx' 'xxx';
      | 'yrt' 'jlg' 'ifs' 'laq' 'xxx' 'xxx' 'xxx' 'xxx' 'xxx' 'xxx' 'xxx' 'xxx' 'xxx' 'xxx' 'xxx' 'xxx' 'xxx' 'xxx' 'xxx' 'xxx' 'xxx' 'xxx' 'xxx' 'xxx';
      | 'eao' 'txi' 'jmk' 'xee' 'sta' 'knq' 'xxx' 'xxx' 'xxx' 'xxx' 'xxx' 'xxx' 'xxx' 'xxx' 'xxx' 'xxx' 'xxx' 'xxx' 'xxx' 'xxx' 'xxx' 'xxx' 'xxx' 'xxx';
      | 'qcj' 'ivn' 'mwb' 'nrx' 'lgx' 'xxx' 'xxx' 'xxx' 'xxx' 'xxx' 'xxx' 'xxx' 'xxx' 'xxx' 'xxx' 'xxx' 'xxx' 'xxx' 'xxx' 'xxx' 'xxx' 'xxx' 'xxx' 'xxx';
      | 'wks' 'fyy' 'lyd' 'xxx' 'xxx' 'xxx' 'xxx' 'xxx' 'xxx' 'xxx' 'xxx' 'xxx' 'xxx' 'xxx' 'xxx' 'xxx' 'xxx' 'xxx' 'xxx' 'xxx' 'xxx' 'xxx' 'xxx' 'xxx';
      | 'xso' 'rqn' 'flj' 'fak' 'xxx' 'xxx' 'xxx' 'xxx' 'xxx' 'xxx' 'xxx' 'xxx' 'xxx' 'xxx' 'xxx' 'xxx' 'xxx' 'xxx' 'xxx' 'xxx' 'xxx' 'xxx' 'xxx' 'xxx';
      | 'ucp' 'wpn' 'mpy' 'xxx' 'xxx' 'xxx' 'xxx' 'xxx' 'xxx' 'xxx' 'xxx' 'xxx' 'xxx' 'xxx' 'xxx' 'xxx' 'xxx' 'xxx' 'xxx' 'xxx' 'xxx' 'xxx' 'xxx' 'xxx';
      | 'zcf' 'knq' 'sta' 'xee' 'jmk' 'xxx' 'xxx' 'xxx' 'xxx' 'xxx' 'xxx' 'xxx' 'xxx' 'xxx' 'xxx' 'xxx' 'xxx' 'xxx' 'xxx' 'xxx' 'xxx' 'xxx' 'xxx' 'xxx';
      | 'sdr' 'vfy' 'gsc' 'wfb' 'xxx' 'xxx' 'xxx' 'xxx' 'xxx' 'xxx' 'xxx' 'xxx' 'xxx' 'xxx' 'xxx' 'xxx' 'xxx' 'xxx' 'xxx' 'xxx' 'xxx' 'xxx' 'xxx' 'xxx';
      | 'ggn' 'brb' 'ylm' 'kdl' 'rnk' 'xxx' 'xxx' 'xxx' 'xxx' 'xxx' 'xxx' 'xxx' 'xxx' 'xxx' 'xxx' 'xxx' 'xxx' 'xxx' 'xxx' 'xxx' 'xxx' 'xxx' 'xxx' 'xxx';
      | 'tky' 'wcx' 'ytk' 'hbp' 'xjh' 'dne' 'xxx' 'xxx' 'xxx' 'xxx' 'xxx' 'xxx' 'xxx' 'xxx' 'xxx' 'xxx' 'xxx' 'xxx' 'xxx' 'xxx' 'xxx' 'xxx' 'xxx' 'xxx';
      | 'kzl' 'sft' 'sof' 'utn' 'xxx' 'xxx' 'xxx' 'xxx' 'xxx' 'xxx' 'xxx' 'xxx' 'xxx' 'xxx' 'xxx' 'xxx' 'xxx' 'xxx' 'xxx' 'xxx' 'xxx' 'xxx' 'xxx' 'xxx';
      | 'epc' 'uhn' 'cqf' 'xwv' 'xxx' 'xxx' 'xxx' 'xxx' 'xxx' 'xxx' 'xxx' 'xxx' 'xxx' 'xxx' 'xxx' 'xxx' 'xxx' 'xxx' 'xxx' 'xxx' 'xxx' 'xxx' 'xxx' 'xxx';
      | 'srh' 'shh' 'mei' 'xxx' 'xxx' 'xxx' 'xxx' 'xxx' 'xxx' 'xxx' 'xxx' 'xxx' 'xxx' 'xxx' 'xxx' 'xxx' 'xxx' 'xxx' 'xxx' 'xxx' 'xxx' 'xxx' 'xxx' 'xxx';
      | 'uqe' 'sft' 'xxx' 'xxx' 'xxx' 'xxx' 'xxx' 'xxx' 'xxx' 'xxx' 'xxx' 'xxx' 'xxx' 'xxx' 'xxx' 'xxx' 'xxx' 'xxx' 'xxx' 'xxx' 'xxx' 'xxx' 'xxx' 'xxx';
      | 'htw' 'hmf' 'aia' 'wsm' 'xxx' 'xxx' 'xxx' 'xxx' 'xxx' 'xxx' 'xxx' 'xxx' 'xxx' 'xxx' 'xxx' 'xxx' 'xxx' 'xxx' 'xxx' 'xxx' 'xxx' 'xxx' 'xxx' 'xxx';
      | 'wid' 'qwo' 'xxx' 'xxx' 'xxx' 'xxx' 'xxx' 'xxx' 'xxx' 'xxx' 'xxx' 'xxx' 'xxx' 'xxx' 'xxx' 'xxx' 'xxx' 'xxx' 'xxx' 'xxx' 'xxx' 'xxx' 'xxx' 'xxx';
      | 'daz' 'yvs' 'xxx' 'xxx' 'xxx' 'xxx' 'xxx' 'xxx' 'xxx' 'xxx' 'xxx' 'xxx' 'xxx' 'xxx' 'xxx' 'xxx' 'xxx' 'xxx' 'xxx' 'xxx' 'xxx' 'xxx' 'xxx' 'xxx';
      | 'bdl' 'ipm' 'kkp' 'xxx' 'xxx' 'xxx' 'xxx' 'xxx' 'xxx' 'xxx' 'xxx' 'xxx' 'xxx' 'xxx' 'xxx' 'xxx' 'xxx' 'xxx' 'xxx' 'xxx' 'xxx' 'xxx' 'xxx' 'xxx';
      | 'xay' 'mpi' 'xxx' 'xxx' 'xxx' 'xxx' 'xxx' 'xxx' 'xxx' 'xxx' 'xxx' 'xxx' 'xxx' 'xxx' 'xxx' 'xxx' 'xxx' 'xxx' 'xxx' 'xxx' 'xxx' 'xxx' 'xxx' 'xxx';
      | 'bsb' 'epc' 'jpb' 'cqs' 'ixc' 'cur' 'ril' 'ybr' 'xxx' 'xxx' 'xxx' 'xxx' 'xxx' 'xxx' 'xxx' 'xxx' 'xxx' 'xxx' 'xxx' 'xxx' 'xxx' 'xxx' 'xxx' 'xxx';
      | 'mwb' 'out' 'xxx' 'xxx' 'xxx' 'xxx' 'xxx' 'xxx' 'xxx' 'xxx' 'xxx' 'xxx' 'xxx' 'xxx' 'xxx' 'xxx' 'xxx' 'xxx' 'xxx' 'xxx' 'xxx' 'xxx' 'xxx' 'xxx';
      | 'cxr' 'yvs' 'xxx' 'xxx' 'xxx' 'xxx' 'xxx' 'xxx' 'xxx' 'xxx' 'xxx' 'xxx' 'xxx' 'xxx' 'xxx' 'xxx' 'xxx' 'xxx' 'xxx' 'xxx' 'xxx' 'xxx' 'xxx' 'xxx';
      | 'ruf' 'jax' 'uvl' 'ctm' 'xxx' 'xxx' 'xxx' 'xxx' 'xxx' 'xxx' 'xxx' 'xxx' 'xxx' 'xxx' 'xxx' 'xxx' 'xxx' 'xxx' 'xxx' 'xxx' 'xxx' 'xxx' 'xxx' 'xxx';
      | 'vtp' 'rbo' 'xxx' 'xxx' 'xxx' 'xxx' 'xxx' 'xxx' 'xxx' 'xxx' 'xxx' 'xxx' 'xxx' 'xxx' 'xxx' 'xxx' 'xxx' 'xxx' 'xxx' 'xxx' 'xxx' 'xxx' 'xxx' 'xxx';
      | 'tqs' 'kdl' 'pje' 'ylm' 'brb' 'xxx' 'xxx' 'xxx' 'xxx' 'xxx' 'xxx' 'xxx' 'xxx' 'xxx' 'xxx' 'xxx' 'xxx' 'xxx' 'xxx' 'xxx' 'xxx' 'xxx' 'xxx' 'xxx';
      | 'thb' 'out' 'xxx' 'xxx' 'xxx' 'xxx' 'xxx' 'xxx' 'xxx' 'xxx' 'xxx' 'xxx' 'xxx' 'xxx' 'xxx' 'xxx' 'xxx' 'xxx' 'xxx' 'xxx' 'xxx' 'xxx' 'xxx' 'xxx';
      | 'ljy' 'ael' 'tqw' 'xxx' 'xxx' 'xxx' 'xxx' 'xxx' 'xxx' 'xxx' 'xxx' 'xxx' 'xxx' 'xxx' 'xxx' 'xxx' 'xxx' 'xxx' 'xxx' 'xxx' 'xxx' 'xxx' 'xxx' 'xxx';
      | 'tkl' 'ssx' 'yds' 'xxx' 'xxx' 'xxx' 'xxx' 'xxx' 'xxx' 'xxx' 'xxx' 'xxx' 'xxx' 'xxx' 'xxx' 'xxx' 'xxx' 'xxx' 'xxx' 'xxx' 'xxx' 'xxx' 'xxx' 'xxx';
      | 'ozd' 'itv' 'csd' 'vvj' 'fyx' 'awl' 'xhb' 'mvn' 'guw' 'vbp' 'hzn' 'yft' 'mfv' 'izj' 'oil' 'uvk' 'cui' 'krt' 'myo' 'fqn' 'gwv' 'zlh' 'xxx' 'xxx';
      | 'uhn' 'lzx' 'dac' 'iqf' 'xxx' 'xxx' 'xxx' 'xxx' 'xxx' 'xxx' 'xxx' 'xxx' 'xxx' 'xxx' 'xxx' 'xxx' 'xxx' 'xxx' 'xxx' 'xxx' 'xxx' 'xxx' 'xxx' 'xxx';
      | 'zad' 'wvh' 'tmc' 'ece' 'xxx' 'xxx' 'xxx' 'xxx' 'xxx' 'xxx' 'xxx' 'xxx' 'xxx' 'xxx' 'xxx' 'xxx' 'xxx' 'xxx' 'xxx' 'xxx' 'xxx' 'xxx' 'xxx' 'xxx';
      | 'qlf' 'gce' 'sgn' 'fni' 'xxx' 'xxx' 'xxx' 'xxx' 'xxx' 'xxx' 'xxx' 'xxx' 'xxx' 'xxx' 'xxx' 'xxx' 'xxx' 'xxx' 'xxx' 'xxx' 'xxx' 'xxx' 'xxx' 'xxx';
      | 'kcf' 'dka' 'pvw' 'uzw' 'xxx' 'xxx' 'xxx' 'xxx' 'xxx' 'xxx' 'xxx' 'xxx' 'xxx' 'xxx' 'xxx' 'xxx' 'xxx' 'xxx' 'xxx' 'xxx' 'xxx' 'xxx' 'xxx' 'xxx';
      | 'uat' 'bda' 'mkd' 'xxx' 'xxx' 'xxx' 'xxx' 'xxx' 'xxx' 'xxx' 'xxx' 'xxx' 'xxx' 'xxx' 'xxx' 'xxx' 'xxx' 'xxx' 'xxx' 'xxx' 'xxx' 'xxx' 'xxx' 'xxx';
      | 'aai' 'gtk' 'gkf' 'cuk' 'qcj' 'xxx' 'xxx' 'xxx' 'xxx' 'xxx' 'xxx' 'xxx' 'xxx' 'xxx' 'xxx' 'xxx' 'xxx' 'xxx' 'xxx' 'xxx' 'xxx' 'xxx' 'xxx' 'xxx';
      | 'mfv' 'cml' 'xxx' 'xxx' 'xxx' 'xxx' 'xxx' 'xxx' 'xxx' 'xxx' 'xxx' 'xxx' 'xxx' 'xxx' 'xxx' 'xxx' 'xxx' 'xxx' 'xxx' 'xxx' 'xxx' 'xxx' 'xxx' 'xxx';
      | 'qlv' 'wdr' 'sbi' 'ihm' 'nww' 'jkx' 'bud' 'qxb' 'xxx' 'xxx' 'xxx' 'xxx' 'xxx' 'xxx' 'xxx' 'xxx' 'xxx' 'xxx' 'xxx' 'xxx' 'xxx' 'xxx' 'xxx' 'xxx';
      | 'paz' 'kbq' 'osk' 'xxx' 'xxx' 'xxx' 'xxx' 'xxx' 'xxx' 'xxx' 'xxx' 'xxx' 'xxx' 'xxx' 'xxx' 'xxx' 'xxx' 'xxx' 'xxx' 'xxx' 'xxx' 'xxx' 'xxx' 'xxx';
      | 'rys' 'iwh' 'xxx' 'xxx' 'xxx' 'xxx' 'xxx' 'xxx' 'xxx' 'xxx' 'xxx' 'xxx' 'xxx' 'xxx' 'xxx' 'xxx' 'xxx' 'xxx' 'xxx' 'xxx' 'xxx' 'xxx' 'xxx' 'xxx';
      | 'gdx' 'out' 'xxx' 'xxx' 'xxx' 'xxx' 'xxx' 'xxx' 'xxx' 'xxx' 'xxx' 'xxx' 'xxx' 'xxx' 'xxx' 'xxx' 'xxx' 'xxx' 'xxx' 'xxx' 'xxx' 'xxx' 'xxx' 'xxx';
      | 'hco' 'cuk' 'gkf' 'xxx' 'xxx' 'xxx' 'xxx' 'xxx' 'xxx' 'xxx' 'xxx' 'xxx' 'xxx' 'xxx' 'xxx' 'xxx' 'xxx' 'xxx' 'xxx' 'xxx' 'xxx' 'xxx' 'xxx' 'xxx';
      | 'gte' 'wks' 'fft' 'xxx' 'xxx' 'xxx' 'xxx' 'xxx' 'xxx' 'xxx' 'xxx' 'xxx' 'xxx' 'xxx' 'xxx' 'xxx' 'xxx' 'xxx' 'xxx' 'xxx' 'xxx' 'xxx' 'xxx' 'xxx';
      | 'zrw' 'iur' 'mei' 'shh' 'xxx' 'xxx' 'xxx' 'xxx' 'xxx' 'xxx' 'xxx' 'xxx' 'xxx' 'xxx' 'xxx' 'xxx' 'xxx' 'xxx' 'xxx' 'xxx' 'xxx' 'xxx' 'xxx' 'xxx';
      | 'izj' 'elj' 'wrh' 'vnz' 'uss' 'xxx' 'xxx' 'xxx' 'xxx' 'xxx' 'xxx' 'xxx' 'xxx' 'xxx' 'xxx' 'xxx' 'xxx' 'xxx' 'xxx' 'xxx' 'xxx' 'xxx' 'xxx' 'xxx';
      | 'lur' 'jpb' 'zib' 'zwl' 'uzn' 'epc' 'nta' 'cur' 'cqs' 'ybr' 'tkl' 'sle' 'xxx' 'xxx' 'xxx' 'xxx' 'xxx' 'xxx' 'xxx' 'xxx' 'xxx' 'xxx' 'xxx' 'xxx';
      | 'hgu' 'jmk' 'xee' 'xxx' 'xxx' 'xxx' 'xxx' 'xxx' 'xxx' 'xxx' 'xxx' 'xxx' 'xxx' 'xxx' 'xxx' 'xxx' 'xxx' 'xxx' 'xxx' 'xxx' 'xxx' 'xxx' 'xxx' 'xxx';
      | 'okf' 'ypu' 'gye' 'qzd' 'xxx' 'xxx' 'xxx' 'xxx' 'xxx' 'xxx' 'xxx' 'xxx' 'xxx' 'xxx' 'xxx' 'xxx' 'xxx' 'xxx' 'xxx' 'xxx' 'xxx' 'xxx' 'xxx' 'xxx';
      | 'mli' 'dir' 'mzw' 'xxx' 'xxx' 'xxx' 'xxx' 'xxx' 'xxx' 'xxx' 'xxx' 'xxx' 'xxx' 'xxx' 'xxx' 'xxx' 'xxx' 'xxx' 'xxx' 'xxx' 'xxx' 'xxx' 'xxx' 'xxx';
      | 'shh' 'rjp' 'xxx' 'xxx' 'xxx' 'xxx' 'xxx' 'xxx' 'xxx' 'xxx' 'xxx' 'xxx' 'xxx' 'xxx' 'xxx' 'xxx' 'xxx' 'xxx' 'xxx' 'xxx' 'xxx' 'xxx' 'xxx' 'xxx';
      | 'nhj' 'ael' 'tqw' 'xxx' 'xxx' 'xxx' 'xxx' 'xxx' 'xxx' 'xxx' 'xxx' 'xxx' 'xxx' 'xxx' 'xxx' 'xxx' 'xxx' 'xxx' 'xxx' 'xxx' 'xxx' 'xxx' 'xxx' 'xxx';
      | 'pbm' 'fxp' 'dfl' 'xxx' 'xxx' 'xxx' 'xxx' 'xxx' 'xxx' 'xxx' 'xxx' 'xxx' 'xxx' 'xxx' 'xxx' 'xxx' 'xxx' 'xxx' 'xxx' 'xxx' 'xxx' 'xxx' 'xxx' 'xxx';
      | 'vnz' 'che' 'xxx' 'xxx' 'xxx' 'xxx' 'xxx' 'xxx' 'xxx' 'xxx' 'xxx' 'xxx' 'xxx' 'xxx' 'xxx' 'xxx' 'xxx' 'xxx' 'xxx' 'xxx' 'xxx' 'xxx' 'xxx' 'xxx';
      | 'vim' 'bmu' 'xxx' 'xxx' 'xxx' 'xxx' 'xxx' 'xxx' 'xxx' 'xxx' 'xxx' 'xxx' 'xxx' 'xxx' 'xxx' 'xxx' 'xxx' 'xxx' 'xxx' 'xxx' 'xxx' 'xxx' 'xxx' 'xxx';
      | 'puz' 'dcl' 'ofd' 'xxx' 'xxx' 'xxx' 'xxx' 'xxx' 'xxx' 'xxx' 'xxx' 'xxx' 'xxx' 'xxx' 'xxx' 'xxx' 'xxx' 'xxx' 'xxx' 'xxx' 'xxx' 'xxx' 'xxx' 'xxx';
      | 'zrg' 'ihy' 'xxx' 'xxx' 'xxx' 'xxx' 'xxx' 'xxx' 'xxx' 'xxx' 'xxx' 'xxx' 'xxx' 'xxx' 'xxx' 'xxx' 'xxx' 'xxx' 'xxx' 'xxx' 'xxx' 'xxx' 'xxx' 'xxx';
      | 'scj' 'ysr' 'knu' 'xxx' 'xxx' 'xxx' 'xxx' 'xxx' 'xxx' 'xxx' 'xxx' 'xxx' 'xxx' 'xxx' 'xxx' 'xxx' 'xxx' 'xxx' 'xxx' 'xxx' 'xxx' 'xxx' 'xxx' 'xxx';
      | 'pjc' 'uvl' 'jax' 'bvs' 'xxx' 'xxx' 'xxx' 'xxx' 'xxx' 'xxx' 'xxx' 'xxx' 'xxx' 'xxx' 'xxx' 'xxx' 'xxx' 'xxx' 'xxx' 'xxx' 'xxx' 'xxx' 'xxx' 'xxx';
      | 'tbn' 'uat' 'lkd' 'fdg' 'xxx' 'xxx' 'xxx' 'xxx' 'xxx' 'xxx' 'xxx' 'xxx' 'xxx' 'xxx' 'xxx' 'xxx' 'xxx' 'xxx' 'xxx' 'xxx' 'xxx' 'xxx' 'xxx' 'xxx';
      | 'rcp' 'okf' 'xxx' 'xxx' 'xxx' 'xxx' 'xxx' 'xxx' 'xxx' 'xxx' 'xxx' 'xxx' 'xxx' 'xxx' 'xxx' 'xxx' 'xxx' 'xxx' 'xxx' 'xxx' 'xxx' 'xxx' 'xxx' 'xxx';
      | 'min' 'out' 'xxx' 'xxx' 'xxx' 'xxx' 'xxx' 'xxx' 'xxx' 'xxx' 'xxx' 'xxx' 'xxx' 'xxx' 'xxx' 'xxx' 'xxx' 'xxx' 'xxx' 'xxx' 'xxx' 'xxx' 'xxx' 'xxx';
      | 'poc' 'rta' 'yvs' 'rbo' 'xxx' 'xxx' 'xxx' 'xxx' 'xxx' 'xxx' 'xxx' 'xxx' 'xxx' 'xxx' 'xxx' 'xxx' 'xxx' 'xxx' 'xxx' 'xxx' 'xxx' 'xxx' 'xxx' 'xxx';
      | 'kde' 'bcz' 'xxx' 'xxx' 'xxx' 'xxx' 'xxx' 'xxx' 'xxx' 'xxx' 'xxx' 'xxx' 'xxx' 'xxx' 'xxx' 'xxx' 'xxx' 'xxx' 'xxx' 'xxx' 'xxx' 'xxx' 'xxx' 'xxx';
      | 'wct' 'bvs' 'jax' 'uvl' 'xxx' 'xxx' 'xxx' 'xxx' 'xxx' 'xxx' 'xxx' 'xxx' 'xxx' 'xxx' 'xxx' 'xxx' 'xxx' 'xxx' 'xxx' 'xxx' 'xxx' 'xxx' 'xxx' 'xxx';
      | 'wvh' 'brg' 'xxx' 'xxx' 'xxx' 'xxx' 'xxx' 'xxx' 'xxx' 'xxx' 'xxx' 'xxx' 'xxx' 'xxx' 'xxx' 'xxx' 'xxx' 'xxx' 'xxx' 'xxx' 'xxx' 'xxx' 'xxx' 'xxx';
      | 'wrh' 'frd' 'kbe' 'ihy' 'xxx' 'xxx' 'xxx' 'xxx' 'xxx' 'xxx' 'xxx' 'xxx' 'xxx' 'xxx' 'xxx' 'xxx' 'xxx' 'xxx' 'xxx' 'xxx' 'xxx' 'xxx' 'xxx' 'xxx';
      | 'fak' 'jwl' 'lzu' 'dni' 'xxx' 'xxx' 'xxx' 'xxx' 'xxx' 'xxx' 'xxx' 'xxx' 'xxx' 'xxx' 'xxx' 'xxx' 'xxx' 'xxx' 'xxx' 'xxx' 'xxx' 'xxx' 'xxx' 'xxx';
      | 'zaq' 'jlg' 'ifs' 'laq' 'ppm' 'xxx' 'xxx' 'xxx' 'xxx' 'xxx' 'xxx' 'xxx' 'xxx' 'xxx' 'xxx' 'xxx' 'xxx' 'xxx' 'xxx' 'xxx' 'xxx' 'xxx' 'xxx' 'xxx';
      | 'yun' 'kde' 'kob' 'qmz' 'uxn' 'xxx' 'xxx' 'xxx' 'xxx' 'xxx' 'xxx' 'xxx' 'xxx' 'xxx' 'xxx' 'xxx' 'xxx' 'xxx' 'xxx' 'xxx' 'xxx' 'xxx' 'xxx' 'xxx';
      | 'boa' 'yql' 'brg' 'fbt' 'sgu' 'xxx' 'xxx' 'xxx' 'xxx' 'xxx' 'xxx' 'xxx' 'xxx' 'xxx' 'xxx' 'xxx' 'xxx' 'xxx' 'xxx' 'xxx' 'xxx' 'xxx' 'xxx' 'xxx';
      | 'izk' 'czt' 'xxx' 'xxx' 'xxx' 'xxx' 'xxx' 'xxx' 'xxx' 'xxx' 'xxx' 'xxx' 'xxx' 'xxx' 'xxx' 'xxx' 'xxx' 'xxx' 'xxx' 'xxx' 'xxx' 'xxx' 'xxx' 'xxx';
      | 'xyj' 'out' 'xxx' 'xxx' 'xxx' 'xxx' 'xxx' 'xxx' 'xxx' 'xxx' 'xxx' 'xxx' 'xxx' 'xxx' 'xxx' 'xxx' 'xxx' 'xxx' 'xxx' 'xxx' 'xxx' 'xxx' 'xxx' 'xxx';
      | 'xhk' 'ril' 'cur' 'yun' 'pmu' 'nta' 'epc' 'uzn' 'zwl' 'rxn' 'sle' 'tkl' 'puz' 'ixc' 'cqs' 'nqo' 'jpb' 'zzk' 'xxx' 'xxx' 'xxx' 'xxx' 'xxx' 'xxx';
      | 'yql' 'mjy' 'cfo' 'bpj' 'vqp' 'xxx' 'xxx' 'xxx' 'xxx' 'xxx' 'xxx' 'xxx' 'xxx' 'xxx' 'xxx' 'xxx' 'xxx' 'xxx' 'xxx' 'xxx' 'xxx' 'xxx' 'xxx' 'xxx';
      | 'dcl' 'nbq' 'xxx' 'xxx' 'xxx' 'xxx' 'xxx' 'xxx' 'xxx' 'xxx' 'xxx' 'xxx' 'xxx' 'xxx' 'xxx' 'xxx' 'xxx' 'xxx' 'xxx' 'xxx' 'xxx' 'xxx' 'xxx' 'xxx';
      | 'ogv' 'utn' 'sof' 'pld' 'xxx' 'xxx' 'xxx' 'xxx' 'xxx' 'xxx' 'xxx' 'xxx' 'xxx' 'xxx' 'xxx' 'xxx' 'xxx' 'xxx' 'xxx' 'xxx' 'xxx' 'xxx' 'xxx' 'xxx';
      | 'rtp' 'gpp' 'gmb' 'eka' 'xxx' 'xxx' 'xxx' 'xxx' 'xxx' 'xxx' 'xxx' 'xxx' 'xxx' 'xxx' 'xxx' 'xxx' 'xxx' 'xxx' 'xxx' 'xxx' 'xxx' 'xxx' 'xxx' 'xxx';
      | 'nki' 'jmk' 'xee' 'knq' 'xxx' 'xxx' 'xxx' 'xxx' 'xxx' 'xxx' 'xxx' 'xxx' 'xxx' 'xxx' 'xxx' 'xxx' 'xxx' 'xxx' 'xxx' 'xxx' 'xxx' 'xxx' 'xxx' 'xxx';
      | 'agn' 'jly' 'alh' 'ola' 'zcf' 'xxx' 'xxx' 'xxx' 'xxx' 'xxx' 'xxx' 'xxx' 'xxx' 'xxx' 'xxx' 'xxx' 'xxx' 'xxx' 'xxx' 'xxx' 'xxx' 'xxx' 'xxx' 'xxx';
      | 'vrp' 'hnw' 'xxx' 'xxx' 'xxx' 'xxx' 'xxx' 'xxx' 'xxx' 'xxx' 'xxx' 'xxx' 'xxx' 'xxx' 'xxx' 'xxx' 'xxx' 'xxx' 'xxx' 'xxx' 'xxx' 'xxx' 'xxx' 'xxx';
      | 'lts' 'yql' 'fbt' 'sgu' 'xxx' 'xxx' 'xxx' 'xxx' 'xxx' 'xxx' 'xxx' 'xxx' 'xxx' 'xxx' 'xxx' 'xxx' 'xxx' 'xxx' 'xxx' 'xxx' 'xxx' 'xxx' 'xxx' 'xxx';
      | 'myo' 'rhq' 'kvi' 'xxx' 'xxx' 'xxx' 'xxx' 'xxx' 'xxx' 'xxx' 'xxx' 'xxx' 'xxx' 'xxx' 'xxx' 'xxx' 'xxx' 'xxx' 'xxx' 'xxx' 'xxx' 'xxx' 'xxx' 'xxx';
      | 'jpb' 'dcl' 'xuk' 'xxx' 'xxx' 'xxx' 'xxx' 'xxx' 'xxx' 'xxx' 'xxx' 'xxx' 'xxx' 'xxx' 'xxx' 'xxx' 'xxx' 'xxx' 'xxx' 'xxx' 'xxx' 'xxx' 'xxx' 'xxx';
      | 'dju' 'vrt' 'ozd' 'fnr' 'you' 'mwu' 'xxx' 'xxx' 'xxx' 'xxx' 'xxx' 'xxx' 'xxx' 'xxx' 'xxx' 'xxx' 'xxx' 'xxx' 'xxx' 'xxx' 'xxx' 'xxx' 'xxx' 'xxx';
      | 'hnw' 'hmf' 'xxx' 'xxx' 'xxx' 'xxx' 'xxx' 'xxx' 'xxx' 'xxx' 'xxx' 'xxx' 'xxx' 'xxx' 'xxx' 'xxx' 'xxx' 'xxx' 'xxx' 'xxx' 'xxx' 'xxx' 'xxx' 'xxx';
      | 'rhq' 'ehc' 'xxx' 'xxx' 'xxx' 'xxx' 'xxx' 'xxx' 'xxx' 'xxx' 'xxx' 'xxx' 'xxx' 'xxx' 'xxx' 'xxx' 'xxx' 'xxx' 'xxx' 'xxx' 'xxx' 'xxx' 'xxx' 'xxx';
      | 'dij' 'knq' 'sta' 'xee' 'txi' 'xxx' 'xxx' 'xxx' 'xxx' 'xxx' 'xxx' 'xxx' 'xxx' 'xxx' 'xxx' 'xxx' 'xxx' 'xxx' 'xxx' 'xxx' 'xxx' 'xxx' 'xxx' 'xxx';
      | 'awl' 'vxt' 'xxx' 'xxx' 'xxx' 'xxx' 'xxx' 'xxx' 'xxx' 'xxx' 'xxx' 'xxx' 'xxx' 'xxx' 'xxx' 'xxx' 'xxx' 'xxx' 'xxx' 'xxx' 'xxx' 'xxx' 'xxx' 'xxx';
      | 'knu' 'bsb' 'lur' 'igu' 'xxx' 'xxx' 'xxx' 'xxx' 'xxx' 'xxx' 'xxx' 'xxx' 'xxx' 'xxx' 'xxx' 'xxx' 'xxx' 'xxx' 'xxx' 'xxx' 'xxx' 'xxx' 'xxx' 'xxx';
      | 'dfo' 'pab' 'xxx' 'xxx' 'xxx' 'xxx' 'xxx' 'xxx' 'xxx' 'xxx' 'xxx' 'xxx' 'xxx' 'xxx' 'xxx' 'xxx' 'xxx' 'xxx' 'xxx' 'xxx' 'xxx' 'xxx' 'xxx' 'xxx';
      | 'ewm' 'sgn' 'fni' 'gce' 'xxx' 'xxx' 'xxx' 'xxx' 'xxx' 'xxx' 'xxx' 'xxx' 'xxx' 'xxx' 'xxx' 'xxx' 'xxx' 'xxx' 'xxx' 'xxx' 'xxx' 'xxx' 'xxx' 'xxx';
      | 'fed' 'osk' 'xxx' 'xxx' 'xxx' 'xxx' 'xxx' 'xxx' 'xxx' 'xxx' 'xxx' 'xxx' 'xxx' 'xxx' 'xxx' 'xxx' 'xxx' 'xxx' 'xxx' 'xxx' 'xxx' 'xxx' 'xxx' 'xxx';
      | 'nwy' 'ppm' 'laq' 'qgn' 'xxx' 'xxx' 'xxx' 'xxx' 'xxx' 'xxx' 'xxx' 'xxx' 'xxx' 'xxx' 'xxx' 'xxx' 'xxx' 'xxx' 'xxx' 'xxx' 'xxx' 'xxx' 'xxx' 'xxx';
      | 'wby' 'you' 'mwu' 'fnr' 'ozd' 'xxx' 'xxx' 'xxx' 'xxx' 'xxx' 'xxx' 'xxx' 'xxx' 'xxx' 'xxx' 'xxx' 'xxx' 'xxx' 'xxx' 'xxx' 'xxx' 'xxx' 'xxx' 'xxx';
      | 'dir' 'jmn' 'gpu' 'xxx' 'xxx' 'xxx' 'xxx' 'xxx' 'xxx' 'xxx' 'xxx' 'xxx' 'xxx' 'xxx' 'xxx' 'xxx' 'xxx' 'xxx' 'xxx' 'xxx' 'xxx' 'xxx' 'xxx' 'xxx';
      | 'mjy' 'wfb' 'iyi' 'vfy' 'xxx' 'xxx' 'xxx' 'xxx' 'xxx' 'xxx' 'xxx' 'xxx' 'xxx' 'xxx' 'xxx' 'xxx' 'xxx' 'xxx' 'xxx' 'xxx' 'xxx' 'xxx' 'xxx' 'xxx';
      | 'fcj' 'zkn' 'hgq' 'szd' 'xxx' 'xxx' 'xxx' 'xxx' 'xxx' 'xxx' 'xxx' 'xxx' 'xxx' 'xxx' 'xxx' 'xxx' 'xxx' 'xxx' 'xxx' 'xxx' 'xxx' 'xxx' 'xxx' 'xxx';
      | 'mzo' 'out' 'xxx' 'xxx' 'xxx' 'xxx' 'xxx' 'xxx' 'xxx' 'xxx' 'xxx' 'xxx' 'xxx' 'xxx' 'xxx' 'xxx' 'xxx' 'xxx' 'xxx' 'xxx' 'xxx' 'xxx' 'xxx' 'xxx';
      | 'lzl' 'xhk' 'xxx' 'xxx' 'xxx' 'xxx' 'xxx' 'xxx' 'xxx' 'xxx' 'xxx' 'xxx' 'xxx' 'xxx' 'xxx' 'xxx' 'xxx' 'xxx' 'xxx' 'xxx' 'xxx' 'xxx' 'xxx' 'xxx';
      | 'czt' 'xcu' 'xvu' 'xxx' 'xxx' 'xxx' 'xxx' 'xxx' 'xxx' 'xxx' 'xxx' 'xxx' 'xxx' 'xxx' 'xxx' 'xxx' 'xxx' 'xxx' 'xxx' 'xxx' 'xxx' 'xxx' 'xxx' 'xxx';
      | 'tyq' 'gsc' 'wfb' 'kjq' 'iyi' 'xxx' 'xxx' 'xxx' 'xxx' 'xxx' 'xxx' 'xxx' 'xxx' 'xxx' 'xxx' 'xxx' 'xxx' 'xxx' 'xxx' 'xxx' 'xxx' 'xxx' 'xxx' 'xxx';
      | 'tda' 'rbo' 'xxx' 'xxx' 'xxx' 'xxx' 'xxx' 'xxx' 'xxx' 'xxx' 'xxx' 'xxx' 'xxx' 'xxx' 'xxx' 'xxx' 'xxx' 'xxx' 'xxx' 'xxx' 'xxx' 'xxx' 'xxx' 'xxx';
      | 'ltv' 'srf' 'vim' 'mli' 'slg' 'xxx' 'xxx' 'xxx' 'xxx' 'xxx' 'xxx' 'xxx' 'xxx' 'xxx' 'xxx' 'xxx' 'xxx' 'xxx' 'xxx' 'xxx' 'xxx' 'xxx' 'xxx' 'xxx';
      | 'iwh' 'qpo' 'xxx' 'xxx' 'xxx' 'xxx' 'xxx' 'xxx' 'xxx' 'xxx' 'xxx' 'xxx' 'xxx' 'xxx' 'xxx' 'xxx' 'xxx' 'xxx' 'xxx' 'xxx' 'xxx' 'xxx' 'xxx' 'xxx';
      | 'hnn' 'bsb' 'fpb' 'lur' 'xxx' 'xxx' 'xxx' 'xxx' 'xxx' 'xxx' 'xxx' 'xxx' 'xxx' 'xxx' 'xxx' 'xxx' 'xxx' 'xxx' 'xxx' 'xxx' 'xxx' 'xxx' 'xxx' 'xxx';
      | 'fan' 'sgu' 'xxx' 'xxx' 'xxx' 'xxx' 'xxx' 'xxx' 'xxx' 'xxx' 'xxx' 'xxx' 'xxx' 'xxx' 'xxx' 'xxx' 'xxx' 'xxx' 'xxx' 'xxx' 'xxx' 'xxx' 'xxx' 'xxx';
      | 'vqp' 'zow' 'rqn' 'fak' 'flj' 'wke' 'xxx' 'xxx' 'xxx' 'xxx' 'xxx' 'xxx' 'xxx' 'xxx' 'xxx' 'xxx' 'xxx' 'xxx' 'xxx' 'xxx' 'xxx' 'xxx' 'xxx' 'xxx';
      | 'ltm' 'pvm' 'xmq' 'xxx' 'xxx' 'xxx' 'xxx' 'xxx' 'xxx' 'xxx' 'xxx' 'xxx' 'xxx' 'xxx' 'xxx' 'xxx' 'xxx' 'xxx' 'xxx' 'xxx' 'xxx' 'xxx' 'xxx' 'xxx';
      | 'cyc' 'dfl' 'fxp' 'xxx' 'xxx' 'xxx' 'xxx' 'xxx' 'xxx' 'xxx' 'xxx' 'xxx' 'xxx' 'xxx' 'xxx' 'xxx' 'xxx' 'xxx' 'xxx' 'xxx' 'xxx' 'xxx' 'xxx' 'xxx';
      | 'kvi' 'gwp' 'jnw' 'xxx' 'xxx' 'xxx' 'xxx' 'xxx' 'xxx' 'xxx' 'xxx' 'xxx' 'xxx' 'xxx' 'xxx' 'xxx' 'xxx' 'xxx' 'xxx' 'xxx' 'xxx' 'xxx' 'xxx' 'xxx';
      | 'srd' 'ipm' 'jrk' 'xxx' 'xxx' 'xxx' 'xxx' 'xxx' 'xxx' 'xxx' 'xxx' 'xxx' 'xxx' 'xxx' 'xxx' 'xxx' 'xxx' 'xxx' 'xxx' 'xxx' 'xxx' 'xxx' 'xxx' 'xxx';
      | 'lkv' 'fnr' 'vrt' 'xxx' 'xxx' 'xxx' 'xxx' 'xxx' 'xxx' 'xxx' 'xxx' 'xxx' 'xxx' 'xxx' 'xxx' 'xxx' 'xxx' 'xxx' 'xxx' 'xxx' 'xxx' 'xxx' 'xxx' 'xxx';
      | 'shb' 'hxf' 'thb' 'rus' 'xxx' 'xxx' 'xxx' 'xxx' 'xxx' 'xxx' 'xxx' 'xxx' 'xxx' 'xxx' 'xxx' 'xxx' 'xxx' 'xxx' 'xxx' 'xxx' 'xxx' 'xxx' 'xxx' 'xxx';
      | 'xuk' 'zxj' 'xxx' 'xxx' 'xxx' 'xxx' 'xxx' 'xxx' 'xxx' 'xxx' 'xxx' 'xxx' 'xxx' 'xxx' 'xxx' 'xxx' 'xxx' 'xxx' 'xxx' 'xxx' 'xxx' 'xxx' 'xxx' 'xxx';
      | 'ifs' 'ryr' 'gep' 'wck' 'lcp' 'fwn' 'gdh' 'foj' 'xxx' 'xxx' 'xxx' 'xxx' 'xxx' 'xxx' 'xxx' 'xxx' 'xxx' 'xxx' 'xxx' 'xxx' 'xxx' 'xxx' 'xxx' 'xxx';
      | 'ynz' 'uji' 'xxx' 'xxx' 'xxx' 'xxx' 'xxx' 'xxx' 'xxx' 'xxx' 'xxx' 'xxx' 'xxx' 'xxx' 'xxx' 'xxx' 'xxx' 'xxx' 'xxx' 'xxx' 'xxx' 'xxx' 'xxx' 'xxx';
      | 'igh' 'sta' 'jmk' 'xxx' 'xxx' 'xxx' 'xxx' 'xxx' 'xxx' 'xxx' 'xxx' 'xxx' 'xxx' 'xxx' 'xxx' 'xxx' 'xxx' 'xxx' 'xxx' 'xxx' 'xxx' 'xxx' 'xxx' 'xxx';
      | 'fyx' 'krd' 'xxx' 'xxx' 'xxx' 'xxx' 'xxx' 'xxx' 'xxx' 'xxx' 'xxx' 'xxx' 'xxx' 'xxx' 'xxx' 'xxx' 'xxx' 'xxx' 'xxx' 'xxx' 'xxx' 'xxx' 'xxx' 'xxx';
      | 'gkf' 'ivn' 'mwb' 'axi' 'xxx' 'xxx' 'xxx' 'xxx' 'xxx' 'xxx' 'xxx' 'xxx' 'xxx' 'xxx' 'xxx' 'xxx' 'xxx' 'xxx' 'xxx' 'xxx' 'xxx' 'xxx' 'xxx' 'xxx';
      | 'bcz' 'ftm' 'rdm' 'wby' 'lkv' 'xxx' 'xxx' 'xxx' 'xxx' 'xxx' 'xxx' 'xxx' 'xxx' 'xxx' 'xxx' 'xxx' 'xxx' 'xxx' 'xxx' 'xxx' 'xxx' 'xxx' 'xxx' 'xxx';
      | 'qeg' 'jlg' 'qgn' 'ifs' 'ppm' 'xxx' 'xxx' 'xxx' 'xxx' 'xxx' 'xxx' 'xxx' 'xxx' 'xxx' 'xxx' 'xxx' 'xxx' 'xxx' 'xxx' 'xxx' 'xxx' 'xxx' 'xxx' 'xxx';
      | 'goq' 'icv' 'xxx' 'xxx' 'xxx' 'xxx' 'xxx' 'xxx' 'xxx' 'xxx' 'xxx' 'xxx' 'xxx' 'xxx' 'xxx' 'xxx' 'xxx' 'xxx' 'xxx' 'xxx' 'xxx' 'xxx' 'xxx' 'xxx';
      | 'qmy' 'out' 'xxx' 'xxx' 'xxx' 'xxx' 'xxx' 'xxx' 'xxx' 'xxx' 'xxx' 'xxx' 'xxx' 'xxx' 'xxx' 'xxx' 'xxx' 'xxx' 'xxx' 'xxx' 'xxx' 'xxx' 'xxx' 'xxx';
      | 'wxl' 'igh' 'heh' 'hvs' 'xxx' 'xxx' 'xxx' 'xxx' 'xxx' 'xxx' 'xxx' 'xxx' 'xxx' 'xxx' 'xxx' 'xxx' 'xxx' 'xxx' 'xxx' 'xxx' 'xxx' 'xxx' 'xxx' 'xxx';
      | 'kbe' 'dzp' 'ybw' 'xxx' 'xxx' 'xxx' 'xxx' 'xxx' 'xxx' 'xxx' 'xxx' 'xxx' 'xxx' 'xxx' 'xxx' 'xxx' 'xxx' 'xxx' 'xxx' 'xxx' 'xxx' 'xxx' 'xxx' 'xxx';
      | 'hxf' 'out' 'xxx' 'xxx' 'xxx' 'xxx' 'xxx' 'xxx' 'xxx' 'xxx' 'xxx' 'xxx' 'xxx' 'xxx' 'xxx' 'xxx' 'xxx' 'xxx' 'xxx' 'xxx' 'xxx' 'xxx' 'xxx' 'xxx';
      | 'tqw' 'rdn' 'nac' 'xxx' 'xxx' 'xxx' 'xxx' 'xxx' 'xxx' 'xxx' 'xxx' 'xxx' 'xxx' 'xxx' 'xxx' 'xxx' 'xxx' 'xxx' 'xxx' 'xxx' 'xxx' 'xxx' 'xxx' 'xxx';
      | 'bmu' 'jmn' 'gkl' 'xfg' 'xxx' 'xxx' 'xxx' 'xxx' 'xxx' 'xxx' 'xxx' 'xxx' 'xxx' 'xxx' 'xxx' 'xxx' 'xxx' 'xxx' 'xxx' 'xxx' 'xxx' 'xxx' 'xxx' 'xxx';
      | 'cqf' 'lzx' 'xxx' 'xxx' 'xxx' 'xxx' 'xxx' 'xxx' 'xxx' 'xxx' 'xxx' 'xxx' 'xxx' 'xxx' 'xxx' 'xxx' 'xxx' 'xxx' 'xxx' 'xxx' 'xxx' 'xxx' 'xxx' 'xxx';
      | 'phn' 'rbi' 'fjm' 'xxx' 'xxx' 'xxx' 'xxx' 'xxx' 'xxx' 'xxx' 'xxx' 'xxx' 'xxx' 'xxx' 'xxx' 'xxx' 'xxx' 'xxx' 'xxx' 'xxx' 'xxx' 'xxx' 'xxx' 'xxx';
      | 'ykt' 'sgu' 'fbt' 'brg' 'xxx' 'xxx' 'xxx' 'xxx' 'xxx' 'xxx' 'xxx' 'xxx' 'xxx' 'xxx' 'xxx' 'xxx' 'xxx' 'xxx' 'xxx' 'xxx' 'xxx' 'xxx' 'xxx' 'xxx';
      | 'zqg' 'out' 'xxx' 'xxx' 'xxx' 'xxx' 'xxx' 'xxx' 'xxx' 'xxx' 'xxx' 'xxx' 'xxx' 'xxx' 'xxx' 'xxx' 'xxx' 'xxx' 'xxx' 'xxx' 'xxx' 'xxx' 'xxx' 'xxx';
      | 'ain' 'mpj' 'xxx' 'xxx' 'xxx' 'xxx' 'xxx' 'xxx' 'xxx' 'xxx' 'xxx' 'xxx' 'xxx' 'xxx' 'xxx' 'xxx' 'xxx' 'xxx' 'xxx' 'xxx' 'xxx' 'xxx' 'xxx' 'xxx';
      | 'esz' 'jmk' 'txi' 'xxx' 'xxx' 'xxx' 'xxx' 'xxx' 'xxx' 'xxx' 'xxx' 'xxx' 'xxx' 'xxx' 'xxx' 'xxx' 'xxx' 'xxx' 'xxx' 'xxx' 'xxx' 'xxx' 'xxx' 'xxx';
      | 'bpj' 'rqn' 'zow' 'flj' 'wke' 'fak' 'xxx' 'xxx' 'xxx' 'xxx' 'xxx' 'xxx' 'xxx' 'xxx' 'xxx' 'xxx' 'xxx' 'xxx' 'xxx' 'xxx' 'xxx' 'xxx' 'xxx' 'xxx';
      | 'qaj' 'gtk' 'gkf' 'cuk' 'qcj' 'xxx' 'xxx' 'xxx' 'xxx' 'xxx' 'xxx' 'xxx' 'xxx' 'xxx' 'xxx' 'xxx' 'xxx' 'xxx' 'xxx' 'xxx' 'xxx' 'xxx' 'xxx' 'xxx';
      | 'kul' 'ckh' 'xxx' 'xxx' 'xxx' 'xxx' 'xxx' 'xxx' 'xxx' 'xxx' 'xxx' 'xxx' 'xxx' 'xxx' 'xxx' 'xxx' 'xxx' 'xxx' 'xxx' 'xxx' 'xxx' 'xxx' 'xxx' 'xxx';
      | 'rss' 'dka' 'nwy' 'xxx' 'xxx' 'xxx' 'xxx' 'xxx' 'xxx' 'xxx' 'xxx' 'xxx' 'xxx' 'xxx' 'xxx' 'xxx' 'xxx' 'xxx' 'xxx' 'xxx' 'xxx' 'xxx' 'xxx' 'xxx';
      | 'gaq' 'ifs' 'laq' 'jlg' 'xxx' 'xxx' 'xxx' 'xxx' 'xxx' 'xxx' 'xxx' 'xxx' 'xxx' 'xxx' 'xxx' 'xxx' 'xxx' 'xxx' 'xxx' 'xxx' 'xxx' 'xxx' 'xxx' 'xxx';
      | 'ehc' 'hco' 'qaj' 'qup' 'xxx' 'xxx' 'xxx' 'xxx' 'xxx' 'xxx' 'xxx' 'xxx' 'xxx' 'xxx' 'xxx' 'xxx' 'xxx' 'xxx' 'xxx' 'xxx' 'xxx' 'xxx' 'xxx' 'xxx';
      | 'saf' 'mwu' 'you' 'fnr' 'vrt' 'xxx' 'xxx' 'xxx' 'xxx' 'xxx' 'xxx' 'xxx' 'xxx' 'xxx' 'xxx' 'xxx' 'xxx' 'xxx' 'xxx' 'xxx' 'xxx' 'xxx' 'xxx' 'xxx';
      | 'mub' 'bee' 'xxx' 'xxx' 'xxx' 'xxx' 'xxx' 'xxx' 'xxx' 'xxx' 'xxx' 'xxx' 'xxx' 'xxx' 'xxx' 'xxx' 'xxx' 'xxx' 'xxx' 'xxx' 'xxx' 'xxx' 'xxx' 'xxx';
      | 'tns' 'lyd' 'fyy' 'bqw' 'xxx' 'xxx' 'xxx' 'xxx' 'xxx' 'xxx' 'xxx' 'xxx' 'xxx' 'xxx' 'xxx' 'xxx' 'xxx' 'xxx' 'xxx' 'xxx' 'xxx' 'xxx' 'xxx' 'xxx';
      | 'ssx' 'utb' 'nel' 'thp' 'hhu' 'wbs' 'xxx' 'xxx' 'xxx' 'xxx' 'xxx' 'xxx' 'xxx' 'xxx' 'xxx' 'xxx' 'xxx' 'xxx' 'xxx' 'xxx' 'xxx' 'xxx' 'xxx' 'xxx';
      | 'mwd' 'qeg' 'gpo' 'xxx' 'xxx' 'xxx' 'xxx' 'xxx' 'xxx' 'xxx' 'xxx' 'xxx' 'xxx' 'xxx' 'xxx' 'xxx' 'xxx' 'xxx' 'xxx' 'xxx' 'xxx' 'xxx' 'xxx' 'xxx';
      | 'lgx' 'out' 'xxx' 'xxx' 'xxx' 'xxx' 'xxx' 'xxx' 'xxx' 'xxx' 'xxx' 'xxx' 'xxx' 'xxx' 'xxx' 'xxx' 'xxx' 'xxx' 'xxx' 'xxx' 'xxx' 'xxx' 'xxx' 'xxx';
      | 'lyr' 'ozd' 'xxx' 'xxx' 'xxx' 'xxx' 'xxx' 'xxx' 'xxx' 'xxx' 'xxx' 'xxx' 'xxx' 'xxx' 'xxx' 'xxx' 'xxx' 'xxx' 'xxx' 'xxx' 'xxx' 'xxx' 'xxx' 'xxx';
      | 'knq' 'qlf' 'tnt' 'bhv' 'aeo' 'ljy' 'dmr' 'xxx' 'xxx' 'xxx' 'xxx' 'xxx' 'xxx' 'xxx' 'xxx' 'xxx' 'xxx' 'xxx' 'xxx' 'xxx' 'xxx' 'xxx' 'xxx' 'xxx';
      | 'php' 'sgu' 'xxx' 'xxx' 'xxx' 'xxx' 'xxx' 'xxx' 'xxx' 'xxx' 'xxx' 'xxx' 'xxx' 'xxx' 'xxx' 'xxx' 'xxx' 'xxx' 'xxx' 'xxx' 'xxx' 'xxx' 'xxx' 'xxx';
      | 'qmz' 'fer' 'bcz' 'xxx' 'xxx' 'xxx' 'xxx' 'xxx' 'xxx' 'xxx' 'xxx' 'xxx' 'xxx' 'xxx' 'xxx' 'xxx' 'xxx' 'xxx' 'xxx' 'xxx' 'xxx' 'xxx' 'xxx' 'xxx';
      | 'oab' 'lup' 'xxx' 'xxx' 'xxx' 'xxx' 'xxx' 'xxx' 'xxx' 'xxx' 'xxx' 'xxx' 'xxx' 'xxx' 'xxx' 'xxx' 'xxx' 'xxx' 'xxx' 'xxx' 'xxx' 'xxx' 'xxx' 'xxx';
      | 'sof' 'ikt' 'xxx' 'xxx' 'xxx' 'xxx' 'xxx' 'xxx' 'xxx' 'xxx' 'xxx' 'xxx' 'xxx' 'xxx' 'xxx' 'xxx' 'xxx' 'xxx' 'xxx' 'xxx' 'xxx' 'xxx' 'xxx' 'xxx';
      | 'lte' 'ytk' 'hbp' 'xjh' 'dne' 'wcx' 'xxx' 'xxx' 'xxx' 'xxx' 'xxx' 'xxx' 'xxx' 'xxx' 'xxx' 'xxx' 'xxx' 'xxx' 'xxx' 'xxx' 'xxx' 'xxx' 'xxx' 'xxx';
      | 'hvs' 'xee' 'txi' 'knq' 'xxx' 'xxx' 'xxx' 'xxx' 'xxx' 'xxx' 'xxx' 'xxx' 'xxx' 'xxx' 'xxx' 'xxx' 'xxx' 'xxx' 'xxx' 'xxx' 'xxx' 'xxx' 'xxx' 'xxx';
      | 'bnw' 'yhu' 'qhx' 'xxx' 'xxx' 'xxx' 'xxx' 'xxx' 'xxx' 'xxx' 'xxx' 'xxx' 'xxx' 'xxx' 'xxx' 'xxx' 'xxx' 'xxx' 'xxx' 'xxx' 'xxx' 'xxx' 'xxx' 'xxx';
      | 'jnw' 'aai' 'hco' 'qup' 'nxs' 'xxx' 'xxx' 'xxx' 'xxx' 'xxx' 'xxx' 'xxx' 'xxx' 'xxx' 'xxx' 'xxx' 'xxx' 'xxx' 'xxx' 'xxx' 'xxx' 'xxx' 'xxx' 'xxx';
      | 'uge' 'bqw' 'fyy' 'xxx' 'xxx' 'xxx' 'xxx' 'xxx' 'xxx' 'xxx' 'xxx' 'xxx' 'xxx' 'xxx' 'xxx' 'xxx' 'xxx' 'xxx' 'xxx' 'xxx' 'xxx' 'xxx' 'xxx' 'xxx';
      | 'cml' 'sid' 'txz' 'qgh' 'xxx' 'xxx' 'xxx' 'xxx' 'xxx' 'xxx' 'xxx' 'xxx' 'xxx' 'xxx' 'xxx' 'xxx' 'xxx' 'xxx' 'xxx' 'xxx' 'xxx' 'xxx' 'xxx' 'xxx';
      | 'sle' 'uwp' 'jhu' 'lra' 'ltm' 'xxx' 'xxx' 'xxx' 'xxx' 'xxx' 'xxx' 'xxx' 'xxx' 'xxx' 'xxx' 'xxx' 'xxx' 'xxx' 'xxx' 'xxx' 'xxx' 'xxx' 'xxx' 'xxx';
      | 'uoi' 'yql' 'sgu' 'xxx' 'xxx' 'xxx' 'xxx' 'xxx' 'xxx' 'xxx' 'xxx' 'xxx' 'xxx' 'xxx' 'xxx' 'xxx' 'xxx' 'xxx' 'xxx' 'xxx' 'xxx' 'xxx' 'xxx' 'xxx';
      | 'tcu' 'eao' 'hgu' 'xxx' 'xxx' 'xxx' 'xxx' 'xxx' 'xxx' 'xxx' 'xxx' 'xxx' 'xxx' 'xxx' 'xxx' 'xxx' 'xxx' 'xxx' 'xxx' 'xxx' 'xxx' 'xxx' 'xxx' 'xxx';
      | 'aaj' 'laq' 'ppm' 'xxx' 'xxx' 'xxx' 'xxx' 'xxx' 'xxx' 'xxx' 'xxx' 'xxx' 'xxx' 'xxx' 'xxx' 'xxx' 'xxx' 'xxx' 'xxx' 'xxx' 'xxx' 'xxx' 'xxx' 'xxx';
      | 'bqy' 'you' 'xxx' 'xxx' 'xxx' 'xxx' 'xxx' 'xxx' 'xxx' 'xxx' 'xxx' 'xxx' 'xxx' 'xxx' 'xxx' 'xxx' 'xxx' 'xxx' 'xxx' 'xxx' 'xxx' 'xxx' 'xxx' 'xxx';
      | 'gye' 'qpo' 'xxx' 'xxx' 'xxx' 'xxx' 'xxx' 'xxx' 'xxx' 'xxx' 'xxx' 'xxx' 'xxx' 'xxx' 'xxx' 'xxx' 'xxx' 'xxx' 'xxx' 'xxx' 'xxx' 'xxx' 'xxx' 'xxx';
      | 'csx' 'you' 'mwu' 'fnr' 'vrt' 'xxx' 'xxx' 'xxx' 'xxx' 'xxx' 'xxx' 'xxx' 'xxx' 'xxx' 'xxx' 'xxx' 'xxx' 'xxx' 'xxx' 'xxx' 'xxx' 'xxx' 'xxx' 'xxx';
      | 'uut' 'dne' 'xjh' 'wcx' 'xxx' 'xxx' 'xxx' 'xxx' 'xxx' 'xxx' 'xxx' 'xxx' 'xxx' 'xxx' 'xxx' 'xxx' 'xxx' 'xxx' 'xxx' 'xxx' 'xxx' 'xxx' 'xxx' 'xxx';
      | 'tat' 'kul' 'jxm' 'dxd' 'shb' 'wtu' 'xxx' 'xxx' 'xxx' 'xxx' 'xxx' 'xxx' 'xxx' 'xxx' 'xxx' 'xxx' 'xxx' 'xxx' 'xxx' 'xxx' 'xxx' 'xxx' 'xxx' 'xxx';
      | 'sbi' 'yvn' 'mub' 'xxx' 'xxx' 'xxx' 'xxx' 'xxx' 'xxx' 'xxx' 'xxx' 'xxx' 'xxx' 'xxx' 'xxx' 'xxx' 'xxx' 'xxx' 'xxx' 'xxx' 'xxx' 'xxx' 'xxx' 'xxx';
      | 'uss' 'suv' 'ihy' 'kbe' 'xxx' 'xxx' 'xxx' 'xxx' 'xxx' 'xxx' 'xxx' 'xxx' 'xxx' 'xxx' 'xxx' 'xxx' 'xxx' 'xxx' 'xxx' 'xxx' 'xxx' 'xxx' 'xxx' 'xxx';
      | 'def' 'wrc' 'eka' 'gpp' 'xxx' 'xxx' 'xxx' 'xxx' 'xxx' 'xxx' 'xxx' 'xxx' 'xxx' 'xxx' 'xxx' 'xxx' 'xxx' 'xxx' 'xxx' 'xxx' 'xxx' 'xxx' 'xxx' 'xxx';
      | 'rso' 'out' 'xxx' 'xxx' 'xxx' 'xxx' 'xxx' 'xxx' 'xxx' 'xxx' 'xxx' 'xxx' 'xxx' 'xxx' 'xxx' 'xxx' 'xxx' 'xxx' 'xxx' 'xxx' 'xxx' 'xxx' 'xxx' 'xxx';
      | 'dmr' 'oab' 'kbr' 'jaa' 'xxx' 'xxx' 'xxx' 'xxx' 'xxx' 'xxx' 'xxx' 'xxx' 'xxx' 'xxx' 'xxx' 'xxx' 'xxx' 'xxx' 'xxx' 'xxx' 'xxx' 'xxx' 'xxx' 'xxx';
      | 'jhu' 'xmq' 'xxx' 'xxx' 'xxx' 'xxx' 'xxx' 'xxx' 'xxx' 'xxx' 'xxx' 'xxx' 'xxx' 'xxx' 'xxx' 'xxx' 'xxx' 'xxx' 'xxx' 'xxx' 'xxx' 'xxx' 'xxx' 'xxx';
      | 'qxb' 'mub' 'sfu' 'fhq' 'yvn' 'xxx' 'xxx' 'xxx' 'xxx' 'xxx' 'xxx' 'xxx' 'xxx' 'xxx' 'xxx' 'xxx' 'xxx' 'xxx' 'xxx' 'xxx' 'xxx' 'xxx' 'xxx' 'xxx';
      | 'nww' 'htw' 'xxx' 'xxx' 'xxx' 'xxx' 'xxx' 'xxx' 'xxx' 'xxx' 'xxx' 'xxx' 'xxx' 'xxx' 'xxx' 'xxx' 'xxx' 'xxx' 'xxx' 'xxx' 'xxx' 'xxx' 'xxx' 'xxx';
      | 'szd' 'zfx' 'xxx' 'xxx' 'xxx' 'xxx' 'xxx' 'xxx' 'xxx' 'xxx' 'xxx' 'xxx' 'xxx' 'xxx' 'xxx' 'xxx' 'xxx' 'xxx' 'xxx' 'xxx' 'xxx' 'xxx' 'xxx' 'xxx';
      | 'gpp' 'qvv' 'min' 'rso' 'iey' 'xxx' 'xxx' 'xxx' 'xxx' 'xxx' 'xxx' 'xxx' 'xxx' 'xxx' 'xxx' 'xxx' 'xxx' 'xxx' 'xxx' 'xxx' 'xxx' 'xxx' 'xxx' 'xxx';
      | 'sft' 'fzl' 'hnn' 'ikt' 'xxx' 'xxx' 'xxx' 'xxx' 'xxx' 'xxx' 'xxx' 'xxx' 'xxx' 'xxx' 'xxx' 'xxx' 'xxx' 'xxx' 'xxx' 'xxx' 'xxx' 'xxx' 'xxx' 'xxx';
      | 'fwn' 'mei' 'iur' 'xxx' 'xxx' 'xxx' 'xxx' 'xxx' 'xxx' 'xxx' 'xxx' 'xxx' 'xxx' 'xxx' 'xxx' 'xxx' 'xxx' 'xxx' 'xxx' 'xxx' 'xxx' 'xxx' 'xxx' 'xxx';
      | 'giz' 'txi' 'sta' 'jmk' 'xxx' 'xxx' 'xxx' 'xxx' 'xxx' 'xxx' 'xxx' 'xxx' 'xxx' 'xxx' 'xxx' 'xxx' 'xxx' 'xxx' 'xxx' 'xxx' 'xxx' 'xxx' 'xxx' 'xxx';
      | 'you' 'hzn' 'izj' 'oil' 'krt' 'wid' 'awl' 'vbp' 'csd' 'xxx' 'xxx' 'xxx' 'xxx' 'xxx' 'xxx' 'xxx' 'xxx' 'xxx' 'xxx' 'xxx' 'xxx' 'xxx' 'xxx' 'xxx';
      | 'yvs' 'fpb' 'lur' 'xhk' 'bsb' 'xxx' 'xxx' 'xxx' 'xxx' 'xxx' 'xxx' 'xxx' 'xxx' 'xxx' 'xxx' 'xxx' 'xxx' 'xxx' 'xxx' 'xxx' 'xxx' 'xxx' 'xxx' 'xxx';
      | 'mci' 'jrk' 'ipm' 'kkp' 'xxx' 'xxx' 'xxx' 'xxx' 'xxx' 'xxx' 'xxx' 'xxx' 'xxx' 'xxx' 'xxx' 'xxx' 'xxx' 'xxx' 'xxx' 'xxx' 'xxx' 'xxx' 'xxx' 'xxx';
      | 'nqo' 'uwp' 'jhu' 'cje' 'xxx' 'xxx' 'xxx' 'xxx' 'xxx' 'xxx' 'xxx' 'xxx' 'xxx' 'xxx' 'xxx' 'xxx' 'xxx' 'xxx' 'xxx' 'xxx' 'xxx' 'xxx' 'xxx' 'xxx';
      | 'alh' 'jmk' 'xee' 'sta' 'txi' 'xxx' 'xxx' 'xxx' 'xxx' 'xxx' 'xxx' 'xxx' 'xxx' 'xxx' 'xxx' 'xxx' 'xxx' 'xxx' 'xxx' 'xxx' 'xxx' 'xxx' 'xxx' 'xxx';
      | 'ejz' 'fjm' 'rbi' 'fim' 'xxx' 'xxx' 'xxx' 'xxx' 'xxx' 'xxx' 'xxx' 'xxx' 'xxx' 'xxx' 'xxx' 'xxx' 'xxx' 'xxx' 'xxx' 'xxx' 'xxx' 'xxx' 'xxx' 'xxx';
      | 'jnd' 'wua' 'esz' 'xxx' 'xxx' 'xxx' 'xxx' 'xxx' 'xxx' 'xxx' 'xxx' 'xxx' 'xxx' 'xxx' 'xxx' 'xxx' 'xxx' 'xxx' 'xxx' 'xxx' 'xxx' 'xxx' 'xxx' 'xxx';
      | 'igu' 'nta' 'pmu' 'yun' 'cur' 'ril' 'ybr' 'rxn' 'zwl' 'uzn' 'fnn' 'cqs' 'ixc' 'puz' 'sle' 'zzk' 'jpb' 'nqo' 'zib' 'xxx' 'xxx' 'xxx' 'xxx' 'xxx';
      | 'yft' 'tky' 'kcj' 'xxx' 'xxx' 'xxx' 'xxx' 'xxx' 'xxx' 'xxx' 'xxx' 'xxx' 'xxx' 'xxx' 'xxx' 'xxx' 'xxx' 'xxx' 'xxx' 'xxx' 'xxx' 'xxx' 'xxx' 'xxx';
      | 'vxt' 'sid' 'xxx' 'xxx' 'xxx' 'xxx' 'xxx' 'xxx' 'xxx' 'xxx' 'xxx' 'xxx' 'xxx' 'xxx' 'xxx' 'xxx' 'xxx' 'xxx' 'xxx' 'xxx' 'xxx' 'xxx' 'xxx' 'xxx';
      | 'dni' 'hvs' 'heh' 'mpi' 'xxx' 'xxx' 'xxx' 'xxx' 'xxx' 'xxx' 'xxx' 'xxx' 'xxx' 'xxx' 'xxx' 'xxx' 'xxx' 'xxx' 'xxx' 'xxx' 'xxx' 'xxx' 'xxx' 'xxx';
      | 'jwy' 'wtu' 'xxx' 'xxx' 'xxx' 'xxx' 'xxx' 'xxx' 'xxx' 'xxx' 'xxx' 'xxx' 'xxx' 'xxx' 'xxx' 'xxx' 'xxx' 'xxx' 'xxx' 'xxx' 'xxx' 'xxx' 'xxx' 'xxx';
      | 'ypu' 'yrt' 'xxx' 'xxx' 'xxx' 'xxx' 'xxx' 'xxx' 'xxx' 'xxx' 'xxx' 'xxx' 'xxx' 'xxx' 'xxx' 'xxx' 'xxx' 'xxx' 'xxx' 'xxx' 'xxx' 'xxx' 'xxx' 'xxx';
      | 'rqn' 'lzu' 'dni' 'xxx' 'xxx' 'xxx' 'xxx' 'xxx' 'xxx' 'xxx' 'xxx' 'xxx' 'xxx' 'xxx' 'xxx' 'xxx' 'xxx' 'xxx' 'xxx' 'xxx' 'xxx' 'xxx' 'xxx' 'xxx';
      | 'yfw' 'bag' 'puu' 'yba' 'xxx' 'xxx' 'xxx' 'xxx' 'xxx' 'xxx' 'xxx' 'xxx' 'xxx' 'xxx' 'xxx' 'xxx' 'xxx' 'xxx' 'xxx' 'xxx' 'xxx' 'xxx' 'xxx' 'xxx';
      | 'vgx' 'amv' 'gte' 'qwd' 'hpw' 'xxx' 'xxx' 'xxx' 'xxx' 'xxx' 'xxx' 'xxx' 'xxx' 'xxx' 'xxx' 'xxx' 'xxx' 'xxx' 'xxx' 'xxx' 'xxx' 'xxx' 'xxx' 'xxx';
      | 'hgb' 'out' 'xxx' 'xxx' 'xxx' 'xxx' 'xxx' 'xxx' 'xxx' 'xxx' 'xxx' 'xxx' 'xxx' 'xxx' 'xxx' 'xxx' 'xxx' 'xxx' 'xxx' 'xxx' 'xxx' 'xxx' 'xxx' 'xxx';
      | 'gwp' 'nxs' 'qaj' 'xxx' 'xxx' 'xxx' 'xxx' 'xxx' 'xxx' 'xxx' 'xxx' 'xxx' 'xxx' 'xxx' 'xxx' 'xxx' 'xxx' 'xxx' 'xxx' 'xxx' 'xxx' 'xxx' 'xxx' 'xxx';
      | 'obo' 'fbt' 'xxx' 'xxx' 'xxx' 'xxx' 'xxx' 'xxx' 'xxx' 'xxx' 'xxx' 'xxx' 'xxx' 'xxx' 'xxx' 'xxx' 'xxx' 'xxx' 'xxx' 'xxx' 'xxx' 'xxx' 'xxx' 'xxx';
      | 'yhu' 'xkn' 'jai' 'boa' 'xxx' 'xxx' 'xxx' 'xxx' 'xxx' 'xxx' 'xxx' 'xxx' 'xxx' 'xxx' 'xxx' 'xxx' 'xxx' 'xxx' 'xxx' 'xxx' 'xxx' 'xxx' 'xxx' 'xxx';
      | 'phi' 'bqy' 'ftm' 'xxx' 'xxx' 'xxx' 'xxx' 'xxx' 'xxx' 'xxx' 'xxx' 'xxx' 'xxx' 'xxx' 'xxx' 'xxx' 'xxx' 'xxx' 'xxx' 'xxx' 'xxx' 'xxx' 'xxx' 'xxx';
      | 'cmi' 'xyj' 'xxx' 'xxx' 'xxx' 'xxx' 'xxx' 'xxx' 'xxx' 'xxx' 'xxx' 'xxx' 'xxx' 'xxx' 'xxx' 'xxx' 'xxx' 'xxx' 'xxx' 'xxx' 'xxx' 'xxx' 'xxx' 'xxx';
      | 'mvn' 'ruf' 'btp' 'xxx' 'xxx' 'xxx' 'xxx' 'xxx' 'xxx' 'xxx' 'xxx' 'xxx' 'xxx' 'xxx' 'xxx' 'xxx' 'xxx' 'xxx' 'xxx' 'xxx' 'xxx' 'xxx' 'xxx' 'xxx';
      | 'utn' 'ikt' 'xxx' 'xxx' 'xxx' 'xxx' 'xxx' 'xxx' 'xxx' 'xxx' 'xxx' 'xxx' 'xxx' 'xxx' 'xxx' 'xxx' 'xxx' 'xxx' 'xxx' 'xxx' 'xxx' 'xxx' 'xxx' 'xxx';
      | 'mkd' 'zcf' 'giz' 'alh' 'xxx' 'xxx' 'xxx' 'xxx' 'xxx' 'xxx' 'xxx' 'xxx' 'xxx' 'xxx' 'xxx' 'xxx' 'xxx' 'xxx' 'xxx' 'xxx' 'xxx' 'xxx' 'xxx' 'xxx';
      | 'eff' 'zow' 'rqn' 'wke' 'flj' 'xxx' 'xxx' 'xxx' 'xxx' 'xxx' 'xxx' 'xxx' 'xxx' 'xxx' 'xxx' 'xxx' 'xxx' 'xxx' 'xxx' 'xxx' 'xxx' 'xxx' 'xxx' 'xxx';
      | 'dml' 'yql' 'brg' 'sgu' 'fbt' 'xxx' 'xxx' 'xxx' 'xxx' 'xxx' 'xxx' 'xxx' 'xxx' 'xxx' 'xxx' 'xxx' 'xxx' 'xxx' 'xxx' 'xxx' 'xxx' 'xxx' 'xxx' 'xxx';
      | 'ivn' 'out' 'xxx' 'xxx' 'xxx' 'xxx' 'xxx' 'xxx' 'xxx' 'xxx' 'xxx' 'xxx' 'xxx' 'xxx' 'xxx' 'xxx' 'xxx' 'xxx' 'xxx' 'xxx' 'xxx' 'xxx' 'xxx' 'xxx';
      | 'fft' 'fyy' 'lyd' 'xxx' 'xxx' 'xxx' 'xxx' 'xxx' 'xxx' 'xxx' 'xxx' 'xxx' 'xxx' 'xxx' 'xxx' 'xxx' 'xxx' 'xxx' 'xxx' 'xxx' 'xxx' 'xxx' 'xxx' 'xxx';
      | 'vbp' 'vnz' 'xxx' 'xxx' 'xxx' 'xxx' 'xxx' 'xxx' 'xxx' 'xxx' 'xxx' 'xxx' 'xxx' 'xxx' 'xxx' 'xxx' 'xxx' 'xxx' 'xxx' 'xxx' 'xxx' 'xxx' 'xxx' 'xxx';
      | 'cuk' 'ivn' 'lgx' 'axi' 'nrx' 'xxx' 'xxx' 'xxx' 'xxx' 'xxx' 'xxx' 'xxx' 'xxx' 'xxx' 'xxx' 'xxx' 'xxx' 'xxx' 'xxx' 'xxx' 'xxx' 'xxx' 'xxx' 'xxx';
      | 'brb' 'lts' 'bcq' 'xsx' 'fan' 'xxx' 'xxx' 'xxx' 'xxx' 'xxx' 'xxx' 'xxx' 'xxx' 'xxx' 'xxx' 'xxx' 'xxx' 'xxx' 'xxx' 'xxx' 'xxx' 'xxx' 'xxx' 'xxx';
      | 'ckh' 'out' 'xxx' 'xxx' 'xxx' 'xxx' 'xxx' 'xxx' 'xxx' 'xxx' 'xxx' 'xxx' 'xxx' 'xxx' 'xxx' 'xxx' 'xxx' 'xxx' 'xxx' 'xxx' 'xxx' 'xxx' 'xxx' 'xxx';
      | 'cui' 'zrg' 'elj' 'wrh' 'vnz' 'uss' 'xxx' 'xxx' 'xxx' 'xxx' 'xxx' 'xxx' 'xxx' 'xxx' 'xxx' 'xxx' 'xxx' 'xxx' 'xxx' 'xxx' 'xxx' 'xxx' 'xxx' 'xxx';
      | 'ybw' 'pxr' 'xxx' 'xxx' 'xxx' 'xxx' 'xxx' 'xxx' 'xxx' 'xxx' 'xxx' 'xxx' 'xxx' 'xxx' 'xxx' 'xxx' 'xxx' 'xxx' 'xxx' 'xxx' 'xxx' 'xxx' 'xxx' 'xxx';
      | 'sfu' 'bee' 'ynz' 'xxx' 'xxx' 'xxx' 'xxx' 'xxx' 'xxx' 'xxx' 'xxx' 'xxx' 'xxx' 'xxx' 'xxx' 'xxx' 'xxx' 'xxx' 'xxx' 'xxx' 'xxx' 'xxx' 'xxx' 'xxx';
      | 'aov' 'gyl' 'xyj' 'xxx' 'xxx' 'xxx' 'xxx' 'xxx' 'xxx' 'xxx' 'xxx' 'xxx' 'xxx' 'xxx' 'xxx' 'xxx' 'xxx' 'xxx' 'xxx' 'xxx' 'xxx' 'xxx' 'xxx' 'xxx';
      | 'yxq' 'jsh' 'smb' 'qhx' 'xxx' 'xxx' 'xxx' 'xxx' 'xxx' 'xxx' 'xxx' 'xxx' 'xxx' 'xxx' 'xxx' 'xxx' 'xxx' 'xxx' 'xxx' 'xxx' 'xxx' 'xxx' 'xxx' 'xxx';
      | 'hgq' 'xvu' 'xxx' 'xxx' 'xxx' 'xxx' 'xxx' 'xxx' 'xxx' 'xxx' 'xxx' 'xxx' 'xxx' 'xxx' 'xxx' 'xxx' 'xxx' 'xxx' 'xxx' 'xxx' 'xxx' 'xxx' 'xxx' 'xxx';
      | 'yba' 'pab' 'xbk' 'bvq' 'xxx' 'xxx' 'xxx' 'xxx' 'xxx' 'xxx' 'xxx' 'xxx' 'xxx' 'xxx' 'xxx' 'xxx' 'xxx' 'xxx' 'xxx' 'xxx' 'xxx' 'xxx' 'xxx' 'xxx';
      | 'ser' 'mzo' 'vii' 'hgb' 'qmy' 'xxx' 'xxx' 'xxx' 'xxx' 'xxx' 'xxx' 'xxx' 'xxx' 'xxx' 'xxx' 'xxx' 'xxx' 'xxx' 'xxx' 'xxx' 'xxx' 'xxx' 'xxx' 'xxx';
      | 'xfg' 'txi' 'xee' 'xxx' 'xxx' 'xxx' 'xxx' 'xxx' 'xxx' 'xxx' 'xxx' 'xxx' 'xxx' 'xxx' 'xxx' 'xxx' 'xxx' 'xxx' 'xxx' 'xxx' 'xxx' 'xxx' 'xxx' 'xxx';
      | 'iey' 'out' 'xxx' 'xxx' 'xxx' 'xxx' 'xxx' 'xxx' 'xxx' 'xxx' 'xxx' 'xxx' 'xxx' 'xxx' 'xxx' 'xxx' 'xxx' 'xxx' 'xxx' 'xxx' 'xxx' 'xxx' 'xxx' 'xxx';
      | 'vhi' 'jaa' 'kbr' 'evt' 'ndc' 'xxx' 'xxx' 'xxx' 'xxx' 'xxx' 'xxx' 'xxx' 'xxx' 'xxx' 'xxx' 'xxx' 'xxx' 'xxx' 'xxx' 'xxx' 'xxx' 'xxx' 'xxx' 'xxx';
      | 'kcj' 'hbp' 'xxx' 'xxx' 'xxx' 'xxx' 'xxx' 'xxx' 'xxx' 'xxx' 'xxx' 'xxx' 'xxx' 'xxx' 'xxx' 'xxx' 'xxx' 'xxx' 'xxx' 'xxx' 'xxx' 'xxx' 'xxx' 'xxx';
      | 'qmf' 'zfx' 'xxx' 'xxx' 'xxx' 'xxx' 'xxx' 'xxx' 'xxx' 'xxx' 'xxx' 'xxx' 'xxx' 'xxx' 'xxx' 'xxx' 'xxx' 'xxx' 'xxx' 'xxx' 'xxx' 'xxx' 'xxx' 'xxx';
      | 'tum' 'sgu' 'brg' 'yql' 'xxx' 'xxx' 'xxx' 'xxx' 'xxx' 'xxx' 'xxx' 'xxx' 'xxx' 'xxx' 'xxx' 'xxx' 'xxx' 'xxx' 'xxx' 'xxx' 'xxx' 'xxx' 'xxx' 'xxx';
      | 'sva' 'her' 'yfw' 'anr' 'xxx' 'xxx' 'xxx' 'xxx' 'xxx' 'xxx' 'xxx' 'xxx' 'xxx' 'xxx' 'xxx' 'xxx' 'xxx' 'xxx' 'xxx' 'xxx' 'xxx' 'xxx' 'xxx' 'xxx';
      | 'ctm' 'cyc' 'xxx' 'xxx' 'xxx' 'xxx' 'xxx' 'xxx' 'xxx' 'xxx' 'xxx' 'xxx' 'xxx' 'xxx' 'xxx' 'xxx' 'xxx' 'xxx' 'xxx' 'xxx' 'xxx' 'xxx' 'xxx' 'xxx';
      | 'sta' 'ewm' 'izk' 'bhv' 'tnt' 'vhi' 'hkq' 'ljy' 'waa' 'aeo' 'ofz' 'xhd' 'fcj' 'gwo' 'qlf' 'nhj' 'xxx' 'xxx' 'xxx' 'xxx' 'xxx' 'xxx' 'xxx' 'xxx';
      | 'jai' 'fbt' 'sgu' 'xxx' 'xxx' 'xxx' 'xxx' 'xxx' 'xxx' 'xxx' 'xxx' 'xxx' 'xxx' 'xxx' 'xxx' 'xxx' 'xxx' 'xxx' 'xxx' 'xxx' 'xxx' 'xxx' 'xxx' 'xxx';
      | 'iyj' 'dka' 'kez' 'nwy' 'xxx' 'xxx' 'xxx' 'xxx' 'xxx' 'xxx' 'xxx' 'xxx' 'xxx' 'xxx' 'xxx' 'xxx' 'xxx' 'xxx' 'xxx' 'xxx' 'xxx' 'xxx' 'xxx' 'xxx';
      | 'ofd' 'tlb' 'xxx' 'xxx' 'xxx' 'xxx' 'xxx' 'xxx' 'xxx' 'xxx' 'xxx' 'xxx' 'xxx' 'xxx' 'xxx' 'xxx' 'xxx' 'xxx' 'xxx' 'xxx' 'xxx' 'xxx' 'xxx' 'xxx';
      | 'qff' 'rcp' 'osk' 'xxx' 'xxx' 'xxx' 'xxx' 'xxx' 'xxx' 'xxx' 'xxx' 'xxx' 'xxx' 'xxx' 'xxx' 'xxx' 'xxx' 'xxx' 'xxx' 'xxx' 'xxx' 'xxx' 'xxx' 'xxx';
      | 'wbs' 'fnr' 'you' 'mwu' 'vrt' 'ozd' 'xxx' 'xxx' 'xxx' 'xxx' 'xxx' 'xxx' 'xxx' 'xxx' 'xxx' 'xxx' 'xxx' 'xxx' 'xxx' 'xxx' 'xxx' 'xxx' 'xxx' 'xxx';
      | 'ulj' 'hrd' 'tcu' 'uqb' 'xxx' 'xxx' 'xxx' 'xxx' 'xxx' 'xxx' 'xxx' 'xxx' 'xxx' 'xxx' 'xxx' 'xxx' 'xxx' 'xxx' 'xxx' 'xxx' 'xxx' 'xxx' 'xxx' 'xxx';
      | 'uvk' 'vxt' 'grp' 'qgy' 'xxx' 'xxx' 'xxx' 'xxx' 'xxx' 'xxx' 'xxx' 'xxx' 'xxx' 'xxx' 'xxx' 'xxx' 'xxx' 'xxx' 'xxx' 'xxx' 'xxx' 'xxx' 'xxx' 'xxx';
      | 'txz' 'irm' 'jwy' 'fmr' 'xxx' 'xxx' 'xxx' 'xxx' 'xxx' 'xxx' 'xxx' 'xxx' 'xxx' 'xxx' 'xxx' 'xxx' 'xxx' 'xxx' 'xxx' 'xxx' 'xxx' 'xxx' 'xxx' 'xxx';
      | 'yco' 'out' 'xxx' 'xxx' 'xxx' 'xxx' 'xxx' 'xxx' 'xxx' 'xxx' 'xxx' 'xxx' 'xxx' 'xxx' 'xxx' 'xxx' 'xxx' 'xxx' 'xxx' 'xxx' 'xxx' 'xxx' 'xxx' 'xxx';
      | 'hlo' 'fxp' 'ser' 'xxx' 'xxx' 'xxx' 'xxx' 'xxx' 'xxx' 'xxx' 'xxx' 'xxx' 'xxx' 'xxx' 'xxx' 'xxx' 'xxx' 'xxx' 'xxx' 'xxx' 'xxx' 'xxx' 'xxx' 'xxx';
      | 'gsc' 'ldf' 'yqe' 'ulj' 'xxx' 'xxx' 'xxx' 'xxx' 'xxx' 'xxx' 'xxx' 'xxx' 'xxx' 'xxx' 'xxx' 'xxx' 'xxx' 'xxx' 'xxx' 'xxx' 'xxx' 'xxx' 'xxx' 'xxx';
